simulink model "finalmodel1"  (R2024b)
(part 6 of 9)

Industries GmbH Sunmodule Plus SW 220 mono black | SolarWorld Industries GmbH Sunmodule Plus SW 220 poly | SolarWorld Industries GmbH Sunmodule Plus SW 225 mono | SolarWorld Industries GmbH Sunmodule Plus SW 225 mono black | SolarWorld Industries GmbH Sunmodule Plus SW 225 poly | SolarWorld Industries GmbH Sunmodule Plus SW 230 mono | SolarWorld Industries GmbH Sunmodule Plus SW 230 mono black | SolarWorld Industries GmbH Sunmodule Plus SW 230 poly | SolarWorld Industries GmbH Sunmodule Plus SW 235 mono | SolarWorld Industries GmbH Sunmodule Plus SW 235 mono black | SolarWorld Industries GmbH Sunmodule Plus SW 235 poly | SolarWorld Industries GmbH Sunmodule Plus SW 240 mono | SolarWorld Industries GmbH Sunmodule Plus SW 240 mono black | SolarWorld Industries GmbH Sunmodule Plus SW 240 poly | SolarWorld Industries GmbH Sunmodule Plus SW 245 mono | SolarWorld Industries GmbH Sunmodule Plus SW 245 mono black | SolarWorld Industries GmbH Sunmodule Plus SW 245 poly | SolarWorld Industries GmbH Sunmodule Plus SW 250 mono | SolarWorld Industries GmbH Sunmodule Plus SW 250 mono black | SolarWorld Industries GmbH Sunmodule Plus SW 250 poly | SolarWorld Industries GmbH Sunmodule Plus SW 255 mono | SolarWorld Industries GmbH Sunmodule Plus SW 255 mono black | SolarWorld Industries GmbH Sunmodule Plus SW 255 poly | SolarWorld Industries GmbH Sunmodule Protect SW 255 mono | SolarWorld Industries GmbH Sunmodule Protect SW 255 mono black | SolarWorld Industries GmbH Sunmodule Bisun SW 260 duo | SolarWorld Industries GmbH Sunmodule Plus SW 260 mono | SolarWorld Industries GmbH Sunmodule Plus SW 260 mono black | SolarWorld Industries GmbH Sunmodule Plus SW 260 poly | SolarWorld Industries GmbH Sunmodule Protect SW 260 mono | SolarWorld Industries GmbH Sunmodule Protect SW 260 mono black | SolarWorld Industries GmbH Sunmodule Bisun SW 265 duo | SolarWorld Industries GmbH Sunmodule Bisun SW 265 duo black | SolarWorld Industries GmbH Sunmodule Plus SW 265 mono | SolarWorld Industries GmbH Sunmodule Plus SW 265 mono black | SolarWorld Industries GmbH Sunmodule Plus SW 265 poly | SolarWorld Industries GmbH Sunmodule Protect SW 265 mono | SolarWorld Industries GmbH sunmodule Protect SW 265 mono black | SolarWorld Industries GmbH Sunmodule Plus SW 270 mono | SolarWorld Industries GmbH Sunmodule Protect SW 270 mono black | SolarWorld Industries GmbH Sunmodule Plus SW 275 mono | SolarWorld Industries GmbH Sunmodule Protect SW 275 mono | SolarWorld Industries GmbH Sunmodule Protect SW 275 mono black | SolarWorld Industries GmbH Sunmodule Protect SW 285 mono | SolarWorld Industries GmbH Sunmodule SW 305 XL mono | SolarWorld Industries GmbH Sunmodule SW 310 XL mono | SolarWorld Industries GmbH Sunmodule SW 315 XL mono | Solarzentrum Allgau Wiosun A-170P | Solarzentrum Allgau Wiosun PVT 170 | Solarzentrum Allgau Wiosun A-175P | Solarzentrum Allgau Wiosun PVT 175 | Solarzentrum Allgau Wiosun A-180P | Solarzentrum Allgau Wiosun PVT 180 | Solarzentrum Allgau Wiosun A-185P | Solarzentrum Allgau Wiosun PVT 185 | Solarzentrum Allgau Wiosun A-190P | Solarzentrum Allgau Wiosun PVT 190 | Soleeva Energy S1AC-7M330 | Soleeva Energy S1AC-7M335 | Soleeva Energy S1AC-7M340 | Soleeva Energy S1AC-7M345 | Solon Solon Blue 220/01 215 | Solon Solon Blue 220 | Solon Solon Blue 220/01 220 | Solon Solon Black 225 | Solon Solon Black 230/01 225 | Solon Solon Black 230/15 225 | Solon Solon Blue 220/01 225 | Solon Solon Blue 225 | Solon Solon Corvus 225 | Solon Solon Black 230 | Solon Solon Black 230/01 230 | Solon Solon Black 230/15 230 | Solon Solon Blue 220/01 230 | Solon Solon Blue 230 | Solon Solon Corvus 230 | Solon Solon Black 230/01 235 | Solon Solon Black 230/15 235 | Solon Solon Black 235 | Solon Solon Blue 220/01 235 | Solon Solon Blue 235 | Solon Solon Corvus 235 | Solon Solon Black 230/01 240 | Solon Solon Black 230/15 240 | Solon Solon Black 240 | Solon Solon Blue 220/01 240 | Solon Solon Blue 240 | Solon Solon Corvus 240 | Solon Solon Black 245 | Solon Solon Blue 270/09 250 | Solon Solon Blue 270/09 255 | Solon Solon Blue 270/09 260 | Solon Solon Black 280/09 265 | Solon Solon Blue 270/09 265 | Solon Solon Blue XT 265 | Solon Solon Black 280/09 270 | Solon Solon Blue 270/09 270 | Solon Solon Blue XT 270 | Solon Solon Black 280/09 275 | Solon Solon Black XT 275 | Solon Solon Blue 270/09 275 | Solon Solon Blue XT 275 | Solon Solon Black 280/09 280 | Solon Solon Black XT 280 | Solon Solon Blue 270/09 280 | Solon Solon Blue XT 280 | Solon SOLquick Black XT 280 | Solon SOLquick Blue XT 280 | Solon SOLquick Blue XT-H 280 | Solon Solon Black 280/09 285 | Solon Solon Black XT 285 | Solon Solon Blue 270/09 285 | Solon Solon Blue XT 285 | Solon SOLquick Black XT 285 | Solon SOLquick Blue XT 285 | Solon Solon Black 280/09 290 | Solon Solon Black XT 290 | Solon Solon Blue 270/09 290 | Solon SOLquick Black XT 290 | Solon Solon Black 280/09 295 | Solon Solon Black XT 295 | Solon SOLquick Black XT 295 | Solon Solon Black 280/09 300 | Solon SOLquick Black XT 300 | Soltecture Linion 85 F | Soltecture Linion 85 L | Soltecture Linion 85 R | Soltecture Linion 90 F | Soltecture Linion 90 L | Soltecture Linion 95 F | Soltecture Linion 95 L | Soltecture Linion 100 F | Soltecture Linion 100 L | SOLTON Power SPI-175M | SOLTON Power SPI-180M | SOLTON Power SPI-185M | SOLTON Power SPI-215P | SOLTON Power SPI-220P | SOLTON Power SPI-225M | SOLTON Power SPI-225P | SOLTON Power SPI-230M | SOLTON Power SPI-230P | SOLTON Power SPI-60-235M | SOLTON Power SPI-60-235P | SOLTON Power SPI-60-240M | SOLTON Power SPI-60-240P | SOLTON Power SPI-60-245M | SOLTON Power SPI-60-245P | SOLTON Power SPI-60-250M | SOLTON Power SPI-60-250P | SOLTON Power SPI-260M | SOLTON Power SPI-260P | SOLTON Power SPI-265M | SOLTON Power SPI-270M | SOLTON Power SPI-270P | SOLTON Power SPI-275M | SOLTON Power SPI-280M | SOLTON Power SPI-280P | SOLTON Power SPI-285M | SOLTON Power SPI-285P | SOLTON Power SPI-290M | SOLTON Power SPI-290P | SOLTON Power SPI-295M | SOLTON Power SPI-295P | SOLTON Power SPI-300M | SOLTON Power SPI-300P | Solvation Manufacturing P6Y-230 | Solvation Manufacturing P6Y-235 | Solvation Manufacturing P6Y-240 | Solvation Manufacturing SM240-5M | Solvation Manufacturing SM240M-B | Solvation Manufacturing P6Y-245 | Solvation Manufacturing SM245-5M | Solvation Manufacturing SM245M-B | Solvation Manufacturing SM245M-Bv | Solvation Manufacturing SM245S-B | Solvation Manufacturing M9X-250 | Solvation Manufacturing P6Y-250 | Solvation Manufacturing SM250-5M | Solvation Manufacturing SM250M-B | Solvation Manufacturing SM250M-Bv | Solvation Manufacturing SM250S-B | Solvation Manufacturing M9X-255 | Solvation Manufacturing SM255-5M | Solvation Manufacturing SM255M-B | Solvation Manufacturing SM255M-Bv | Solvation Manufacturing SM255S-B | Solvation Manufacturing M9X-260 | Solvation Manufacturing SM260-5M | Solvation Manufacturing SM260M-Bv | Solvation Manufacturing M9X-265 | Solvation Manufacturing SM265M-Bv | Solvation Manufacturing P7Y-270 | Solvation Manufacturing SM270M-A | Solvation Manufacturing P7Y-275 | Solvation Manufacturing SM275M-A | Solvation Manufacturing P7Y-280 | Solvation Manufacturing SM280M-A | Solvation Manufacturing P7Y-285 | Solvation Manufacturing SM285M-A | Solvation Manufacturing SM285M-Av | Solvation Manufacturing P7Y-290 | Solvation Manufacturing SM290M-A | Solvation Manufacturing SM290M-Av | Solvation Manufacturing SM295M-A | Solvation Manufacturing SM295M-Av | Solvation Manufacturing SM300M-A | Solvation Manufacturing SM300M-Av | Solvation Manufacturing SM305M-A | Solvation Manufacturing SM305M-Av | Solvation Manufacturing SM310M-Av | Solvation Manufacturing SM315M-Av | Sonali Energees SS 270 | Sonali Energees SS 280 | Sonali Energees SS 290 | Sonali Energees SS 300 | Sonali Energees SS 310 | Sonali Energees SS 315 | Sonali Energees SS 320 | Sonali Energees USA SS 1200 P | Sonali Energees USA SS 1250 P | Sonali Energees USA SS 1300 P | Sonali Energees USA SS 1400 P | Sonali Energees USA SS1750-170W | Sonali Energees USA SS 1750 P | Sonali Energees USA SS1750-175W | Sonali Energees USA SS 1800 P | Sonali Energees USA SS1750-180W | Sonali Energees USA SS 1900 P | Sonali Energees USA SS 2000 P | Sonali Energees USA SS 2100 P | Sonali Energees USA SS2100-210W | Sonali Energees USA SS2100-215W | Sonali Energees USA SS 2200 P | Sonali Energees USA SS2100-220W | Sonali Energees USA SS 2300 P | Sonali Energees USA SS2300-230W | Sonali Energees USA SS2300-235W | Sonali Energees USA SS 2400 P | Sonali Energees USA SS2300-240W | Sonali Energees USA SS2500-250W | Sonali Energees USA SS2800-275W | Sonali Energees USA SS2800-280W | Sonali Energees USA SS2800-285W | Sonnetek SNK-165PSD | Sonnetek SNK-170PSD | Sonnetek SNK-175PSD | Sonnetek SNK-180PSD | Sonnetek SNK-250PSP | Sonnetek SNK-260PSP | Sonnetek SNK-270PSP | Sopray Energy SR-150 | Sopray Energy SR-160 | Sopray Energy SR-165 | Sopray Energy SR-170 | Sopray Energy SR-175 | Sopray Energy SR-180 | Sopray Energy SR156P-200 | Sopray Energy SR156P-210 | Sopray Energy SR156P-220 | Sopray Energy SR156P-230 | Sova Power SOLARSOVA 200P | Sova Power SOLARSOVA 205P | Sova Power SOLARSOVA 210P | Sova Power SOLARSOVA 215P | Sova Power SOLARSOVA 220P | Sova Power SOLARSOVA 235P | Sova Power SOLARSOVA 240P | Sova Power SOLARSOVA 245P | Sova Power SOLARSOVA 250P | Sova Power SOLARSOVA 255P | Sova Power SOLARSOVA 260P | Sovello SV-T-190-yyy | Sovello SV-X-190-yyy | Sovello SV-T-195-yyy | Sovello SV-X-195-yyy | Sovello SV-T-200-yyy | Sovello SV-X-200-yyy | Sovello SV-X-205-yyy | Sovello SV-X-210-yyy | SRS Energy SPT16 | Star Harvest Solar SHS260-5M | Stion SN-110 | Stion STN-110 | Stion SN-115 | Stion STN-115 | Stion SN-120 | Stion STL-120A | Stion STN-120 | Stion STO-120A | Stion SN-125 | Stion STL-125 | Stion STL-125A | Stion STN-125 | Stion STO-125 | Stion STO-125A | Stion SN-130 | Stion STL-130 | Stion STL-130A | Stion STN-130 | Stion STO-130 | Stion STO-130A | Stion SN-135 | Stion STL-135 | Stion STL-135A | Stion STN-135 | Stion STO-135 | Stion STO-135A | Stion SN-140 | Stion STL-140 | Stion STL-140A | Stion STN-140 | Stion STO-140 | Stion STO-140A | Stion SN-145 | Stion STL-145 | Stion STL-145A | Stion STN-145 | Stion STO-145 | Stion STO-145A | Stion SN-150 | Stion STL-150 | Stion STL-150A | Stion STN-150 | Stion STO-150 | Stion STO-150A | Stion STL-155A | Stion STO-155A | Stion STL-160A | Stion STO-160A | STX Solar STX-240MT2 | STX Solar STX-245MT2 | STX Solar STX-250MT2 | STX Solar STX-255MT2 | STX Solar STX-260MT2 | STX Solar STX-290MT2 | STX Solar STX-295MT2 | STX Solar STX-300MT2 | STX Solar STX-305MT2 | Sun Earth Solar Power TDB125x125-36-P 80W | Sun Earth Solar Power TDB125x125-36-P 85W | Sun Earth Solar Power TPB125x125-36-P 85W | Sun Earth Solar Power TDB125x125-36-P 90W | Sun Earth Solar Power TPB125x125-36-P 90W | Sun Earth Solar Power TDB125x125-36-P 95W | Sun Earth Solar Power TPB125x125-36-P 95W | Sun Earth Solar Power TDB156x156-36-P 125W | Sun Earth Solar Power TPB156x156-36-P 125W | Sun Earth Solar Power TDB156x156-36-P 130W | Sun Earth Solar Power TPB156x156-36-P 130W | Sun Earth Solar Power TDB156x156-36-P 135W | Sun Earth Solar Power TPB156x156-36-P 135W | Sun Earth Solar Power TDB156x156-36-P 140W | Sun Earth Solar Power TPB156x156-36-P 140W | Sun Earth Solar Power TDB156x156-36-P 145W | Sun Earth Solar Power TPB156x156-36-P 145W | Sun Earth Solar Power TDB125x125-72-P 150W | Sun Earth Solar Power TPB125x125-72-P 150W | Sun Earth Solar Power TDB125x125-72-P 155W | Sun Earth Solar Power TPB125x125-72-P 155W | Sun Earth Solar Power TDB125x125-72-P 160W | Sun Earth Solar Power TPB125x125-72-P 160W | Sun Earth Solar Power TDB125x125-72-P 165W | Sun Earth Solar Power TPB125x125-72-P 165W | Sun Earth Solar Power TDB125x125-72-P 170W | Sun Earth Solar Power TPB125x125-72-P 170W | Sun Earth Solar Power TDB125x125-72-P 175W | Sun Earth Solar Power TPB125x125-72-P 175W | Sun Earth Solar Power TDB125x125-72-P 180W | Sun Earth Solar Power TPB125x125-72-P 180W | Sun Earth Solar Power TPB156x156-54-P 180W | Sun Earth Solar Power TDB125x125-72-P 185W | Sun Earth Solar Power TPB125x125-72-P 185W | Sun Earth Solar Power TPB156x156-54-P 185W | Sun Earth Solar Power TDB125x125-72-P 190W | Sun Earth Solar Power TPB125x125-72-P 190W | Sun Earth Solar Power TPB156x156-54-P 190W | Sun Earth Solar Power TPB156x156-54-P 195W | Sun Earth Solar Power TPB125x125-96-P 200W | Sun Earth Solar Power TPB156x156-54-P 200W | Sun Earth Solar Power TPB156x156-60-P 200W | Sun Earth Solar Power TPB156x156-54-P 205W | Sun Earth Solar Power TPB156x156-60-P 205W | Sun Earth Solar Power TPB125x125-96-P 210W | Sun Earth Solar Power TPB156x156-54-P 210W | Sun Earth Solar Power TPB156x156-60-P 210W | Sun Earth Solar Power TDB156x156-60-P 215W | Sun Earth Solar Power TPB156x156-54-P 215W | Sun Earth Solar Power TPB156x156-60-P 215W | Sun Earth Solar Power TDB156x156-60-P 220W | Sun Earth Solar Power TPB125x125-96-P 220W | Sun Earth Solar Power TPB156x156-54-P 220W | Sun Earth Solar Power TPB156x156-60-P 220W | Sun Earth Solar Power TDB156x156-60-P 225W | Sun Earth Solar Power TPB156x156-60-P 225W | Sun Earth Solar Power TDB156x156-60-P 230W | Sun Earth Solar Power TPB125x125-96-P 230W | Sun Earth Solar Power TPB156x156-60-P 230W | Sun Earth Solar Power TPB156x156-72-P 230W | Sun Earth Solar Power TDB156x156-60-P 235W | Sun Earth Solar Power TPB156x156-60-P 235W | Sun Earth Solar Power TDB156x156-60-P 240W | Sun Earth Solar Power TPB125x125-96-P 240W | Sun Earth Solar Power TPB156x156-60-P 240W | Sun Earth Solar Power TPB156x156-72-P 240W | Sun Earth Solar Power TDB156x156-60-P 245W | Sun Earth Solar Power TPB156x156-60-P 245W | Sun Earth Solar Power TPB156x156-72-P 250W | Sun Earth Solar Power TPB156x156-72-P 255W | Sun Earth Solar Power TPB156x156-72-P 260W | Sun Earth Solar Power TPB156x156-72-P 270W | Sun Earth Solar Power TDB156x156-72-P 280W | Sun Earth Solar Power TPB156x156-72-P 280W | Sun Earth Solar Power TDB156x156-72-P 285W | Sun Earth Solar Power TPB156x156-72-P 285W | Sun Earth Solar Power TDB156x156-72-P 290W | Sun Earth Solar Power TPB156x156-72-P 290W | Sun Earth Solar Power TDB156x156-72-P 295W | Sun Earth Solar Power TPB156x156-72-P 295W | Sun Energy Engineering SE14-50 | Sun Energy Engineering SE14-52 | SUN M ENERGY SDN BHD ES200PCFW | SUN M ENERGY SDN BHD SME-P648200 | SUN M ENERGY SDN BHD SME-P648200B | SUN M ENERGY SDN BHD ES205PCFW | SUN M ENERGY SDN BHD SME-P648205 | SUN M ENERGY SDN BHD SME-P648205B | SUN M ENERGY SDN BHD ES210PCFW | SUN M ENERGY SDN BHD SME-P648210 | SUN M ENERGY SDN BHD SME-P648210B | SUN M ENERGY SDN BHD ES215PCFW | SUN M ENERGY SDN BHD SME-P648215 | SUN M ENERGY SDN BHD SME-P648215B | SUN M ENERGY SDN BHD ES250PAFW | SUN M ENERGY SDN BHD SME-P660250 | SUN M ENERGY SDN BHD SME-P660250B | SUN M ENERGY SDN BHD ES255PAFW | SUN M ENERGY SDN BHD SME-P660255 | SUN M ENERGY SDN BHD SME-P660255B | SUN M ENERGY SDN BHD ES260PAFW | SUN M ENERGY SDN BHD SME-P660260 | SUN M ENERGY SDN BHD SME-P660260B | SUN M ENERGY SDN BHD ES265PAFW | SUN M ENERGY SDN BHD SME-P660265 | SUN M ENERGY SDN BHD SME-P660265B | SUN M ENERGY SDN BHD ES300PBFW | SUN M ENERGY SDN BHD SME-P672300 | SUN M ENERGY SDN BHD SME-P672300B | SUN M ENERGY SDN BHD ES305PBFW | SUN M ENERGY SDN BHD SME-P672305 | SUN M ENERGY SDN BHD SME-P672305B | SUN M ENERGY SDN BHD ES310PBFW | SUN M ENERGY SDN BHD SME-P672310 | SUN M ENERGY SDN BHD SME-P672310B | SUN M ENERGY SDN BHD ES315PBFW | SUN M ENERGY SDN BHD SME-P672315 | SUN M ENERGY SDN BHD SME-P672315B | SUN M ENERGY SDN BHD ES320PBFW | SUN M ENERGY SDN BHD SME-P672320 | SUN M ENERGY SDN BHD SME-P672320B | Sun Well Solar WD-A-CC-087A | Sun Well Solar WD-A-CC-087B | Sun Well Solar WD-A-CC-087C | Sun World Solar Energy Technology (Luoyang) SWM230P156 | Sun World Solar Energy Technology (Luoyang) SWM235M156 | Sun World Solar Energy Technology (Luoyang) SWM235P156 | Sun World Solar Energy Technology (Luoyang) SWM240M156 | Sun World Solar Energy Technology (Luoyang) SWM240P156 | Sun World Solar Energy Technology (Luoyang) SWM245M156 | Sun World Solar Energy Technology (Luoyang) SWM245P156 | Sun World Solar Energy Technology (Luoyang) SWM250M156 | Sun World Solar Energy Technology (Luoyang) SWM250P156 | Sun World Solar Energy Technology (Luoyang) SWM255M156 | Sun World Solar Energy Technology (Luoyang) SWM280P156 | Sun World Solar Energy Technology (Luoyang) SWM285M156 | Sun World Solar Energy Technology (Luoyang) SWM285P156 | Sun World Solar Energy Technology (Luoyang) SWM290M156 | Sun World Solar Energy Technology (Luoyang) SWM290P156 | Sun World Solar Energy Technology (Luoyang) SWM295M156 | Sun World Solar Energy Technology (Luoyang) SWM295P156 | Sun World Solar Energy Technology (Luoyang) SWM300M156 | Sun World Solar Energy Technology (Luoyang) SWM300P156 | Sunarray SUNARRAY-M6B2409-130 | Sunarray SUNARRAY-M6B2409-135 | Sunarray SUNARRAY-S6B2409-135 | Sunarray SUNARRAY-M6B2409-140 | Sunarray SUNARRAY-S6B2409-140 | Sunarray SUNARRAY-S6B2409-145 | Sunarray SUNARRAY-M6B2608-175 | Sunarray SUNARRAY-M6B2608-180 | Sunarray SUNARRAY-S6B2608-180 | Sunarray SUNARRAY-M6B2608-185 | Sunarray SUNARRAY-S6B2608-185 | Sunarray SUNARRAY-M6B2609-190 | Sunarray SUNARRAY-S6B2608-190 | Sunarray SUNARRAY-M6B2609-195 | Sunarray SUNARRAY-S6B2609-195 | Sunarray SUNARRAY-M6B2609-200 | Sunarray SUNARRAY-S6B2609-200 | Sunarray SUNARRAY-M6B2609-205 | Sunarray SUNARRAY-S6B2609-205 | Sunarray SUNARRAY-M6B2609-210 | Sunarray SUNARRAY-S6B2609-210 | Sunarray SUNARRAY-M6B2609-215 | Sunarray SUNARRAY-S6B2609-215 | Sunarray SUNARRAY-M6B2609-220 | Sunarray SUNARRAY-S6B2609-220 | Sunarray SUNARRAY-M6B2609-225 | Sunarray SUNARRAY-S6B2609-225 | Sunarray SUNARRAY-M6B2609-230 | Sunarray SUNARRAY-S6B2609-230 | Sunarray SUNARRAY-M6B2610-235 | Sunarray SUNARRAY-S6B2609-235 | Sunarray SUNARRAY-M6B2610-240 | Sunarray SUNARRAY-S6B2609-240 | Sunarray SUNARRAY-M6B3612-270T | Sunarray SUNARRAY-M6B2612-275 | Sunarray SUNARRAY-M6B3612-275T | Sunarray SUNARRAY-M6B2612-280 | Sunarray SUNARRAY-M6B3612-280T | Sunarray SUNARRAY-M6B2612-285 | Sunarray SUNARRAY-M6B3612-285T | Sunarray SUNARRAY-S6B3612-285T | Sunarray SUNARRAY-M6B2612-290 | Sunarray SUNARRAY-M6B3612-290T | Sunarray SUNARRAY-S6B3612-290T | Sunarray SUNARRAY-M6B2612-295 | Sunarray SUNARRAY-S6B3612-295T | Sunarray SUNARRAY-S6B3612-300T | Sunarray SUNARRAY-S6B3612-305T | SunEdison SE-F245KzC-2y | SunEdison SE-F250KzC-2y | SunEdison MEMC-F255KzC-2y | SunEdison SE-F255CzC-3y | SunEdison SE-F255CzC-4y | SunEdison SE-F255CzD-3y | SunEdison SE-F255CzD-4y | SunEdison SE-F255FzC-3y | SunEdison SE-F255FzC-4y | SunEdison SE-F255FzD-3y | SunEdison SE-F255FzD-4y | SunEdison SE-F255GzC-3y | SunEdison SE-F255GzC-4y | SunEdison SE-F255GzD-3y | SunEdison SE-F255GzD-4y | SunEdison SE-F255KzC-2y | SunEdison SE-F255KzC-3y | SunEdison SE-F255KzC-4y | SunEdison SE-F255KzD-3y | SunEdison SE-F255KzD-4y | SunEdison MEMC-F260KzC-2y | SunEdison SE-F260CzC-3y | SunEdison SE-F260CzC-4y | SunEdison SE-F260CzD-3y | SunEdison SE-F260CzD-4y | SunEdison SE-F260FzC-3y | SunEdison SE-F260FzC-4y | SunEdison SE-F260FzD-3y | SunEdison SE-F260FzD-4y | SunEdison SE-F260GzC-3y | SunEdison SE-F260GzC-4y | SunEdison SE-F260GzD-3y | SunEdison SE-F260GzD-4y | SunEdison SE-F260KzC-2y | SunEdison SE-F260KzC-3y | SunEdison SE-F260KzC-4y | SunEdison SE-F260KzD-3y | SunEdison SE-F260KzD-4y | SunEdison MEMC-F265KzC-2y | SunEdison SE-F265CzC-3y | SunEdison SE-F265CzC-4y | SunEdison SE-F265CzD-3y | SunEdison SE-F265CzD-4y | SunEdison SE-F265FzC-3y | SunEdison SE-F265FzC-4y | SunEdison SE-F265FzD-3y | SunEdison SE-F265FzD-4y | SunEdison SE-F265GzC-3y | SunEdison SE-F265GzC-4y | SunEdison SE-F265GzD-3y | SunEdison SE-F265GzD-4y | SunEdison SE-F265KzC-2y | SunEdison SE-F265KzC-3y | SunEdison SE-F265KzC-4y | SunEdison SE-F265KzD-3y | SunEdison SE-F265KzD-4y | SunEdison SE-R265GzC-3y | SunEdison SE-R265GzC-4y | SunEdison MEMC-F270KzC-2y | SunEdison SE-F270CzC-3y | SunEdison SE-F270CzC-4y | SunEdison SE-F270CzD-3y | SunEdison SE-F270CzD-4y | SunEdison SE-F270FzC-3y | SunEdison SE-F270FzC-4y | SunEdison SE-F270FzD-3y | SunEdison SE-F270FzD-4y | SunEdison SE-F270GzC-4y | SunEdison SE-F270GzD-3y | SunEdison SE-F270GzD-4y | SunEdison SE-F270KzC-2y | SunEdison SE-F270KzC-3y | SunEdison SE-F270KzC-4y | SunEdison SE-F270KzD-3y | SunEdison SE-F270KzD-4y | SunEdison SE-H270EzC-3y | SunEdison SE-R270CzC-3y | SunEdison SE-R270GzC-3y | SunEdison SE-R270GzC-4y | SunEdison SE-R270KzC-3y | SunEdison SE-F275CzC-3y | SunEdison SE-F275CzC-4y | SunEdison SE-F275CzD-3y | SunEdison SE-F275CzD-4y | SunEdison SE-F275FzC-3y | SunEdison SE-F275FzC-4y | SunEdison SE-F275FzD-3y | SunEdison SE-F275FzD-4y | SunEdison SE-F275GzC-4y | SunEdison SE-F275GzD-3y | SunEdison SE-F275GzD-4y | SunEdison SE-F275KzC-4y | SunEdison SE-F275KzD-3y | SunEdison SE-F275KzD-4y | SunEdison SE-H275EzC-3y | SunEdison SE-R275CzC-3y | SunEdison SE-R275FzC-3y | SunEdison SE-R275FzC-4y | SunEdison SE-R275GzC-3y | SunEdison SE-R275GzC-4y | SunEdison SE-R275KzC-3y | SunEdison SE-F280CzC-3y | SunEdison SE-F280CzC-4y | SunEdison SE-F280CzD-3y | SunEdison SE-F280CzD-4y | SunEdison SE-F280FzC-4y | SunEdison SE-F280FzD-3y | SunEdison SE-F280FzD-4y | SunEdison SE-F280GzC-4y | SunEdison SE-F280GzD-3y | SunEdison SE-F280GzD-4y | SunEdison SE-F280KzC-4y | SunEdison SE-F280KzD-3y | SunEdison SE-F280KzD-4y | SunEdison SE-H280EzC-3y | SunEdison SE-R280CzC-3y | SunEdison SE-R280FzC-3y | SunEdison SE-R280FzC-4y | SunEdison SE-R280GzC-3y | SunEdison SE-R280GzC-4y | SunEdison SE-R280KzC-3y | SunEdison SE-H285EzC-3y | SunEdison SE-R285CzC-3y | SunEdison SE-R285FzC-3y | SunEdison SE-R285FzC-4y | SunEdison SE-R285GzC-3y | SunEdison SE-R285GzC-4y | SunEdison SE-H290EzC-3y | SunEdison SE-R290CzC-3y | SunEdison SE-R290FzC-3y | SunEdison SE-R290FzC-4y | SunEdison SE-R295FzC-3y | SunEdison SE-R295FzC-4y | SunEdison SE-F305BzC-4y | SunEdison SE-F305BzD-3y | SunEdison SE-F305BzD-4y | SunEdison SE-F305EzC-3y | SunEdison SE-F305EzC-4y | SunEdison SE-F305EzD-3y | SunEdison SE-F305EzD-4y | SunEdison SE-Z305-4 | SunEdison SE-F310BzC-3y | SunEdison SE-F310BzC-4y | SunEdison SE-F310BzD-3y | SunEdison SE-F310BzD-4y | SunEdison SE-F310EzC-3y | SunEdison SE-F310EzC-4y | SunEdison SE-F310EzD-3y | SunEdison SE-F310EzD-4y | SunEdison SE-Z310-4 | SunEdison SE-D315BzC-3y | SunEdison SE-F315BzC-3y | SunEdison SE-F315BzC-4y | SunEdison SE-F315BzD-3y | SunEdison SE-F315BzD-4y | SunEdison SE-F315EzC-3y | SunEdison SE-F315EzC-4y | SunEdison SE-F315EzD-3y | SunEdison SE-F315EzD-4y | SunEdison SE-Z315-4 | SunEdison SE-D320BzC-3y | SunEdison SE-F320BzC-3y | SunEdison SE-F320BzC-4y | SunEdison SE-F320BzD-3y | SunEdison SE-F320BzD-4y | SunEdison SE-F320EzC-3y | SunEdison SE-F320EzC-4y | SunEdison SE-F320EzD-3y | SunEdison SE-F320EzD-4y | SunEdison SE-Z320-4 | SunEdison SE-D325BzC-3y | SunEdison SE-F325BzC-3y | SunEdison SE-F325BzC-4y | SunEdison SE-F325BzD-3y | SunEdison SE-F325BzD-4y | SunEdison SE-F325EzC-3y | SunEdison SE-F325EzC-4y | SunEdison SE-F325EzD-3y | SunEdison SE-F325EzD-4y | SunEdison SE-R325BzC-3y | SunEdison SE-Z325-4 | SunEdison SE-D330BzC-3y | SunEdison SE-F330BzC-3y | SunEdison SE-F330BzC-4y | SunEdison SE-F330BzD-3y | SunEdison SE-F330BzD-4y | SunEdison SE-F330EzC-3y | SunEdison SE-F330EzC-4y | SunEdison SE-F330EzD-3y | SunEdison SE-F330EzD-4y | SunEdison SE-H330EzC-3y | SunEdison SE-R330BzC-3y | SunEdison SE-R330BzC-4y | SunEdison SE-R330EzC-3y | SunEdison SE-R330EzC-4y | SunEdison SE-Z330-4 | SunEdison SE-D335BzC-3y | SunEdison SE-F335BzC-3y | SunEdison SE-F335BzC-4y | SunEdison SE-F335BzD-3y | SunEdison SE-F335BzD-4y | SunEdison SE-F335EzC-3y | SunEdison SE-F335EzC-4y | SunEdison SE-F335EzD-3y | SunEdison SE-F335EzD-4y | SunEdison SE-H335-4 | SunEdison SE-H335EzC-3y | SunEdison SE-R335BzC-3y | SunEdison SE-R335BzC-4y | SunEdison SE-R335EzC-3y | SunEdison SE-R335EzC-4y | SunEdison SE-H340-4 | SunEdison SE-H340EzC-3y | SunEdison SE-R340BzC-3y | SunEdison SE-R340BzC-4y | SunEdison SE-R340EzC-3y | SunEdison SE-R340EzC-4y | SunEdison SE-H345-4 | SunEdison SE-H345EzC-3y | SunEdison SE-R345BzC-3y | SunEdison SE-R345BzC-4y | SunEdison SE-R345EzC-3y | SunEdison SE-R345EzC-4y | SunEdison SE-H350-4 | SunEdison SE-H350EzC-3y | SunEdison SE-R350BzC-3y | SunEdison SE-R350BzC-4y | SunEdison SE-R350EzC-3y | SunEdison SE-R350EzC-4y | SunEdison SE-H355-4 | SunEdison SE-H355EzC-3y | SunEdison SE-R355BzC-4y | SunEdison SE-R355EzC-3y | SunEdison SE-R355EzC-4y | SunEdison SE-H360-4 | SunEdison SE-R360BzC-4y | SunEdison SE-R360EzC-3y | SunEdison SE-R360EzC-4y | SunEdison SE-H365-4 | SunEdison SE-Z370-4 | SunEdison SE-Z375-4 | SunEdison SE-Z380-4 | SunEdison SE-Z385-4 | SunEdison SE-Z390-4 | SunEdison SE-Z395-4 | SUNGEN International SG-HN90-GG | SUNGEN International SG-HN95-GG | SUNGEN International SG-HN100-GG | SUNGEN International SG-HN105-GG | SUNGEN International SG-HN110-GG | SUNGEN International SGM-165D | SUNGEN International SGM-170D | SUNGEN International SGM-175D | SUNGEN International SGM-180D | SUNGEN International SGM-185D | SUNGEN International SGM-190D | SUNGEN International SGM-195D | SUNGEN International SGM-200D | SUNGEN International SGM-200P | SUNGEN International SGM-205D | SUNGEN International SGM-205P | SUNGEN International SGM-210D | SUNGEN International SGM-210P | SUNGEN International SGM-215D | SUNGEN International SGM-215P | SUNGEN International SGM-220D | SUNGEN International SGM-220P | SUNGEN International SGM-225D | SUNGEN International SGM-225P | SUNGEN International SGM-230D | SUNGEN International SGM-230P | SUNGEN International SGM-235D | SUNGEN International SGM-235P | SUNGEN International SGM-240D | SUNGEN International SGM-240P | SUNGEN International SGM-245D | SUNGEN International SGM-245P | SUNGEN International SGM-250D | SUNGEN International SGM-250P | SUNGEN International SGM-255D | SUNGEN International SGM-255P | SUNGEN International SGM-260D | SUNGEN International SGM-260P | SUNGEN International SGM-265P | SUNGEN International SGM-270P | SUNGEN International SGM-275P | SUNGEN International SGM-280P | SUNGEN International SGM-285P | Suniva ART230-60-3-100 | Suniva ART235-60-3-100 | Suniva ART235-60-3-101 | Suniva ART235-60-3-1B0 | Suniva MVP235-60-5-401 | Suniva MVT235-60-5-100 | Suniva MVX235-60-5-100 | Suniva MVX235-60-5-701 | Suniva OPT235-60-4-100 | Suniva OPT235-60-4-1B0 | Suniva ART240-60-3-100 | Suniva ART240-60-3-101 | Suniva ART240-60-3-1B0 | Suniva MVT240-60-5-100 | Suniva MVX240-60-5-100 | Suniva MVX240-60-5-701 | Suniva MVX240-60-5-7B1 | Suniva MVX240-60-5-801 | Suniva MVX240-60-5-8B1 | Suniva OPT240-60-4-100 | Suniva OPT240-60-4-1B0 | Suniva ART245-60-3-100 | Suniva ART245-60-3-101 | Suniva ART245-60-3-1B0 | Suniva MVT245-60-5-100 | Suniva MVX245-60-5-100 | Suniva MVX245-60-5-701 | Suniva MVX245-60-5-7B1 | Suniva MVX245-60-5-801 | Suniva MVX245-60-5-8B1 | Suniva OPT245-60-4-100 | Suniva OPT245-60-4-1B0 | Suniva ART250-60-3-100 | Suniva ART250-60-3-101 | Suniva ART250-60-3-1B0 | Suniva MVT250-60-5-100 | Suniva MVX250-60-5-100 | Suniva MVX250-60-5-701 | Suniva MVX250-60-5-7B1 | Suniva MVX250-60-5-801 | Suniva MVX250-60-5-8B1 | Suniva OPT250-60-4-100 | Suniva OPT250-60-4-1B0 | Suniva ART255-60-3-100 | Suniva ART255-60-3-1B0 | Suniva MVT255-60-5-100 | Suniva MVX255-60-5-100 | Suniva MVX255-60-5-701 | Suniva MVX255-60-5-7B1 | Suniva MVX255-60-5-801 | Suniva MVX255-60-5-8B1 | Suniva OPT255-60-4-100 | Suniva OPT255-60-4-1B0 | Suniva MVT260-60-5-100 | Suniva MVX260-60-5-100 | Suniva MVX260-60-5-701 | Suniva MVX260-60-5-7B1 | Suniva MVX260-60-5-800 | Suniva MVX260-60-5-801 | Suniva MVX260-60-5-8B1 | Suniva OPT260-60-4-100 | Suniva OPT260-60-4-1B0 | Suniva ART265-60-4-8B0 | Suniva MVT265-60-5-100 | Suniva MVX265-60-5-100 | Suniva MVX265-60-5-800 | Suniva OPT265-60-4-100 | Suniva OPT265-60-4-1B0 | Suniva ART270-60-4-8B0 | Suniva MVX270-60-5-800 | Suniva OPT270-60-4-100 | Suniva OPT270-60-4-1B0 | Suniva ART275-60-4-800 | Suniva ART275-60-4-8B0 | Suniva OPT275-60-4-100 | Suniva OPT275-60-4-1B0 | Suniva OPT275-60-4-800 | Suniva OPT275-60-4-8B0 | Suniva ART280-60-4-800 | Suniva ART280-60-4-8B0 | Suniva MVT280-72-5-100 | Suniva MVX280-72-5-100 | Suniva OPT280-60-4-100 | Suniva OPT280-60-4-1B0 | Suniva OPT280-60-4-800 | Suniva OPT280-60-4-8B0 | Suniva ART285-60-4-800 | Suniva ART285-60-4-8B0 | Suniva MVT285-72-5-100 | Suniva MVX285-72-5-100 | Suniva MVX285-72-5-701 | Suniva MVX285-72-5-801 | Suniva OPT285-60-4-100 | Suniva OPT285-60-4-1B0 | Suniva OPT285-60-4-800 | Suniva OPT285-60-4-8B0 | Suniva ART290-60-4-800 | Suniva ART290-60-4-8B0 | Suniva MVT290-72-5-100 | Suniva MVX290-72-5-100 | Suniva MVX290-72-5-701 | Suniva MVX290-72-5-801 | Suniva OPT290-60-4-100 | Suniva OPT290-60-4-1B0 | Suniva OPT290-60-4-800 | Suniva OPT290-60-4-8B0 | Suniva OPT290-72-4-100 | Suniva MVT295-72-5-100 | Suniva MVX295-72-5-100 | Suniva MVX295-72-5-701 | Suniva MVX295-72-5-801 | Suniva OPT295-60-4-100 | Suniva OPT295-60-4-1B0 | Suniva OPT295-72-4-100 | Suniva ART300-72-4-100 | Suniva MVT300-72-5-100 | Suniva MVX300-72-5-100 | Suniva MVX300-72-5-701 | Suniva MVX300-72-5-801 | Suniva OPT300-60-4-100 | Suniva OPT300-60-4-1B0 | Suniva OPT300-72-4-100 | Suniva ART305-72-4-100 | Suniva MVT305-72-5-100 | Suniva MVX305-72-5-100 | Suniva MVX305-72-5-701 | Suniva MVX305-72-5-801 | Suniva OPT305-72-4-100 | Suniva ART310-72-4-100 | Suniva MVT310-72-5-100 | Suniva MVX310-72-5-100 | Suniva MVX310-72-5-800 | Suniva MVX310-72-5-801 | Suniva OPT310-72-4-100 | Suniva ART315-72-4-100 | Suniva MVX315-72-5-800 | Suniva OPT315-72-4-100 | Suniva ART320-72-4-100 | Suniva MVX320-72-5-800 | Suniva OPT320-72-4-100 | Suniva ART325-72-4-100 | Suniva MVX325-72-5-800 | Suniva OPT325-72-4-100 | Suniva ART330-72-4-100 | Suniva MVX330-72-5-800 | Suniva OPT330-72-4-100 | Suniva ART335-72-4-100 | Suniva OPT335-72-4-100 | Suniva ART340-72-4-100 | Suniva OPT340-72-4-100 | Sunlan Solar SLM225P | Sunlan Solar SLM230P | Sunlan Solar SLM235P | Sunlan Solar SLM245P | Sunlan Solar SLM270P | Sunlan Solar SLM275P | Sunlan Solar SLM280P | Sunny International Power SPM-180PB203 | Sunny International Power SPM-180SB105 | Sunny International Power SPM-190PB203 | Sunny International Power SPM-190SB105 | Sunny International Power SPM-200PB203 | Sunny International Power SPM-200PB204 | Sunny International Power SPM-200SB105 | Sunny International Power SPM-210PB203 | Sunny International Power SPM-210PB204 | Sunny International Power SPM-220PB204 | Sunny International Power SPM-230PB204 | Sunny International Power SPM-230PB206 | Sunny International Power SPM-240PB204 | Sunny International Power SPM-240PB205 | Sunny International Power SPM-240PB206 | Sunny International Power SPM-250PB205 | Sunny International Power SPM-250PB206 | Sunny International Power SPM-260PB205 | Sunny International Power SPM-260PB206 | Sunny International Power SPM-270PB205 | Sunny International Power SPM-270PB206 | Sunny International Power SPM-280PB205 | Sunny International Power SPM-290PB205 | Sunperfect Solar CRM60S125M-24 | Sunperfect Solar CRM60S125S | Sunperfect Solar CRM85S125M-36 | Sunperfect Solar CRM85S125S | Sunperfect Solar CRM115S125M-48 | Sunperfect Solar CRM115S125S | Sunperfect Solar CRM145S125M-60 | Sunperfect Solar CRM145S125S | Sunperfect Solar CRM175S125M-72 | Sunperfect Solar CRM175S125S | Sunperfect Solar CRM180S125M-72 | Sunperfect Solar CRM185S125M-72 | Sunperfect Solar CRM185S156P-54 | Sunperfect Solar CRM190S125M-72 | Sunperfect Solar CRM190S156P-54 | Sunperfect Solar CRM195S125M-72 | Sunperfect Solar CRM195S125M-80 | Sunperfect Solar CRM195S125S | Sunperfect Solar CRM195S156P-54 | Sunperfect Solar CRM200S156P-54 | Sunperfect Solar CRM200S156P-60 | Sunperfect Solar CRM205S125M-80 | Sunperfect Solar CRM205S156P-54 | Sunperfect Solar CRM205S156P-60 | Sunperfect Solar CRM210S125M-80 | Sunperfect Solar CRM210S156P-54 | Sunperfect Solar CRM210S156P-60 | Sunperfect Solar CRM215S125M-80 | Sunperfect Solar CRM215S156P-54 | Sunperfect Solar CRM215S156P-60 | Sunperfect Solar CRM220S156P-54 | Sunperfect Solar CRM220S156P-60 | Sunperfect Solar CRM225S156P-54 | Sunperfect Solar CRM225S156P-60 | Sunperfect Solar CRM230S156P-54 | Sunperfect Solar CRM230S156P-60 | Sunperfect Solar CRM235S125M-96 | Sunperfect Solar CRM235S125S | Sunperfect Solar CRM235S156P-60 | Sunperfect Solar CRM240S125M-96 | Sunperfect Solar CRM240S156P-60 | Sunperfect Solar CRM240S156P-72 | Sunperfect Solar CRM245S125M-96 | Sunperfect Solar CRM245S156P-60 | Sunperfect Solar CRM245S156P-72 | Sunperfect Solar CRM250S125M-96 | Sunperfect Solar CRM250S156P-60 | Sunperfect Solar CRM250S156P-72 | Sunperfect Solar CRM255S125M-96 | Sunperfect Solar CRM255S156P-60 | Sunperfect Solar CRM255S156P-72 | Sunperfect Solar CRM260S125M-96 | Sunperfect Solar CRM260S156P-60 | Sunperfect Solar CRM260S156P-72 | Sunperfect Solar CRM265S125M-96 | Sunperfect Solar CRM265S156P-72 | Sunperfect Solar CRM270S156P-72 | Sunperfect Solar CRM275S156P-72 | Sunperfect Solar CRM280S156P-72 | Sunperfect Solar CRM285S156P-72 | Sunperfect Solar CRM290S156P-72 | Sunperfect Solar CRM295S156P-72 | Sunperfect Solar CRM300S156P-72 | SunPower PL-PLT-63L-BLK-U | SunPower SPR-76R-BLK-U | SunPower SPR-76RE-BLK-U | SunPower SPR-200-BLK-U | SunPower SPR-200-WHT-U | SunPower SPR-205-BLK-U | SunPower SPR-208-WHT-U | SunPower SPR-210-BLK-U | SunPower SPR-210-WHT-U | SunPower PL-SUNP-SPR-215 | SunPower SPR-215-WHT-U | SunPower SPR-217-WHT-U | SunPower SER-220P | SunPower SPR-220-BLK-U | SunPower SPR-220-WHT-U | SunPower SPR-225-BLK-U | SunPower SPR-225E-BLK-D | SunPower SPR-225E-BLK-U-ACPV | SunPower SPR-225E-WHT-D | SunPower SPR-225NE-BLK-D | SunPower SER-228P | SunPower SPR-230E-WHT-D | SunPower SPR-230NE-BLK-D | SunPower SPR-230NE-BLK-U-ACPV | SunPower SPR-230-WHT-U | SunPower SER-235P | SunPower SPR-235NE-WHT-D | SunPower SPR-E18-235 | SunPower SPR-E19-235 | SunPower T5-SER-235P | SunPower SPR-238E-WHT-D | SunPower SPR-240E-WHT-D | SunPower SPR-240E-WHT-U-ACPV | SunPower SPR-E19-240 | SunPower SPR-X19-240-BLK | SunPower SPR-X19-240-BLK-B-AC | SunPower SPR-245NE-WHT-D | SunPower SPR-245NE-WHT-U-240 ACPV | SunPower SPR-245NE-WHT-U-ACPV | SunPower SPR-E19-245 | SunPower SPR-E20-245 | SunPower SPR-E20-245-A-AC | SunPower SPR-E20-245-B-AC | SunPower SPR-X20-245 | SunPower SPR-250NX-BLK-D | SunPower SPR-X20-250-BLK | SunPower SPR-X20-250-BLK-A-AC | SunPower SPR-X20-250-BLK-B-AC | SunPower SPR-X20-250-BLK-LAM | SunPower SPR-X20-255 | SunPower SPR-X21-255 | SunPower PL-SUNP-SPR-290 | SunPower SPR-290-WHT-U | SunPower T5-SPR-290 | SunPower SPR-295E-WHT-D | SunPower SPR-295E-WHT-U | SunPower SPR-E18-295-COM | SunPower SPR-300E-WHT-D | SunPower SPR-300NE-WHT-D | SunPower SPR-E18-300-COM | SunPower PL-SUNP-SPR-305 | SunPower SPR-305E-WHT-D | SunPower SPR-305E-WHT-U | SunPower SPR-305NE-WHT-D | SunPower SPR-305-WHT-U | SunPower SPR-E18-305-COM | SunPower T5-SPR-305 | SunPower T5-SPR-305E | SunPower PL-SUNP-SPR-308E | SunPower SPR-308E-WHT-D | SunPower SPR-308NE-WHT-D | SunPower T5-SPR-308E | SunPower PL-SUNP-SPR-310 | SunPower SPR-310E-WHT-D | SunPower SPR-310E-WHT-U | SunPower SPR-310-WHT-U | SunPower SPR-E19-310-COM | SunPower T5-SPR-310 | SunPower PL-SUNP-SPR-315E | SunPower SPR-315E-WHT-D | SunPower SPR-315E-WHT-U | SunPower SPR-315NE-WHT-D | SunPower SPR-E19-315 | SunPower SPR-E19-315-COM | SunPower T5-SPR-315 | SunPower T5-SPR-315E | SunPower PL-SUNP-SPR-318E | SunPower SPR-318E-WHT-D | SunPower T5-SPR-318E | SunPower SPR-320E-WHT-D | SunPower SPR-320NE-WHT-D | SunPower SPR-E19-320 | SunPower SPR-E19-320-C-AC | SunPower SPR-E19-320-COM | SunPower SPR-E19-320-D-AC | SunPower T5-SPR-320E | SunPower SPR-P17-325-COM | SunPower SPR-327NE-WHT-D | SunPower SPR-E20-327 | SunPower SPR-E20-327-C-AC | SunPower SPR-E20-327-COM | SunPower SPR-E20-327-COM-LAM | SunPower SPR-E20-327-COM-T5 | SunPower SPR-E20-327-D-AC | SunPower SPR-X20-327 | SunPower SPR-X20-327-BLK | SunPower SPR-X20-327-BLK-C-AC | SunPower SPR-X20-327-BLK-D-AC | SunPower SPR-X20-327-C-AC | SunPower SPR-X20-327-COM | SunPower SPR-X20-327-D-AC | SunPower T5-SPR-327 | SunPower SPR-P17-330-COM | SunPower SPR-335NX-BLK-D | SunPower SPR-P17-335-COM | SunPower SPR-X21-335 | Sunpower SPR-X21-335-BLK | SunPower SPR-X21-335-BLK-C-AC | SunPower SPR-X21-335-BLK-D-AC | SunPower SPR-X21-335-C-AC | Sunpower SPR-X21-335-COM | SunPower SPR-X21-335-D-AC | SunPower SPR-X22-335-BLK | SunPower SPR-P17-340-COM | SunPower SPR-X22-340-BLK | SunPower SPR-343J-WHT-D | SunPower SPR-343NJ-WHT-D | SunPower SPR-343NX-BLK-D | SunPower SPR-343NX-WHT-D | SunPower SPR-P17-345-COM | SunPower SPR-X21-345 | SunPower SPR-X21-345-C-AC | SunPower SPR-X21-345-COM | SunPower SPR-X21-345-D-AC | SunPower SPR-X22-345-BLK | SunPower SPV-P17-345-COM | SunPower SPR-P17-350-COM | SunPower SPR-X21-350-BLK | SunPower SPR-P17-355-COM | SunPower SPR-X22-359 | SunPower SPR-X22-360 | SunPower SPR-X22-360-C-AC | SunPower SPR-X22-360-COM | SunPower SPR-X22-360-D-AC | SunPower SPR-X22-370 | SunPower SPR-X22-370-COM | SunPower SPR-X22-370-D-AC | SunPower SPR-390E-WHT-D | SunPower SPR-400E-WHT-D | SunPower SPR-410NE-WHT-D | SunPower SPR-E19-410-COM | SunPower SPR-415E-WHT-D | Sunpower SPR-E19-415-COM | SunPower SPR-E19-420-COM | Sunpower SPR-425E-WHT-D | SunPower SPR-435NE-WHT-D | SunPower SPR-E20-435-COM | SunPower SPR-440NE-WHT-D | SunPower SPR-E20-440-COM | SunPower SPR-445J-WHT-D | SunPower SPR-445NJ-WHT-D | SunPower SPR-445NX-WHT-D | SunPower SPR-X20-445-COM | Sunpower SPR-X20-450-COM | Sunpower SPR-X21-460-COM | Sunpower SPR-X22-460 | SunPower SPR-X22-460-COM | Sunpower SPR-X21-470-COM | SunPower SPR-X22-470-COM | SunPower SPR-X22-475-COM | Sunpower SPR-X22-480-COM | Sunpreme Inc. SNPM-GX-220 | Sunpreme Inc. SNPM-GX-225 | Sunpreme Inc. SNPM-GX-230 | Sunpreme Inc. SNPM-GX-235 | Sunpreme Inc. SNPM-GX-240 | Sunpreme Inc. SNPM-GX-72-245 | Sunpreme Inc. SNPM-GX-72-250 | Sunpreme Inc. SNPM-GX-72-255 | Sunpreme Inc. SNPM-GxB-270 | Sunpreme Inc. SNPM-GxB-280 | Sunpreme Inc. SNPM-GX-285 | Sunpreme Inc. SNPM-GX-290 | Sunpreme Inc. SNPM-GxB-290 | Sunpreme Inc. SNPM-GxB-290 SM | Sunpreme Inc. SNPM-GxB-SL-290 | Sunpreme Inc. SNPM-GX-295 | Sunpreme Inc. SNPM-GX-300 | Sunpreme Inc. SNPM-GxB-300y | Sunpreme Inc. SNPM-GxB-SL-300 | Sunpreme Inc. SNPM-GX-305 | Sunpreme Inc. SNPM-GX-310 | Sunpreme Inc. SNPM-GxB-310y | Sunpreme Inc. SNPM-GxB-310y SM | Sunpreme Inc. SNPM-GxB-SL-310 | Sunpreme Inc. SNPM-GX-315 | Sunpreme Inc. SNPM-GX-330 | Sunpreme Inc. SNPM-GxB-330 | Sunpreme Inc. SNPM-GX-340 | Sunpreme Inc. SNPM-GxB-340 | Sunpreme Inc. SNPM-GX-350 | Sunpreme Inc. SNPM-GxB-350 | Sunpreme Inc. SNPM-GxB-360 | Sunpreme Inc. SNPM-GxB-370-4BB | Sunpreme Inc. SNPM-GxB-380-4BB | Sunpreme Inc. SNPM-HxB-390 | Sunpreme Inc. SNPM-HxB-395 | Sunpreme Inc. SNPM-HxB-400 | Sunpreme Inc. SNPM-HxB-405 | Sunpreme Inc. SNPM-HxB-410 | Sunpreme Inc. SNPM-HxB-415 | Sunpreme Inc. SNPM-HxB-420 | Sunpreme Inc. SNPM-GxB-490 | Sunpreme Inc. SNPM-GxB-500 | Sunpreme Inc. SNPM-GxB-510 | Sunrise Solartech SR-M572185 | Sunrise Solartech SR-M648185 | Sunrise Solartech SR-M572190 | Sunrise Solartech SR-M648190 | Sunrise Solartech SR-M572195 | Sunrise Solartech SR-M648195 | Sunrise Solartech SR-M572200 | Sunrise Solartech SR-M648200 | Sunrise Solartech SR-M572205 | Sunrise Solartech SR-M648205 | Sunrise Solartech SR-M654210 | Sunrise Solartech SR-M654215 | Sunrise Solartech SR-M654220 | Sunrise Solartech SR-P660220 | Sunrise Solartech SR-M654225 | Sunrise Solartech SR-P660225 | Sunrise Solartech SR-M654230 | Sunrise Solartech SR-P660230 | Sunrise Solartech SR-M660235 | Sunrise Solartech SR-P660235 | Sunrise Solartech SR-M660240 | Sunrise Solartech SR-P660240 | Sunrise Solartech SR-M660245 | Sunrise Solartech SR-M660250 | Sunrise Solartech SR-M660255 | Sunrise Solartech SR-M660260 | Sunrise Solartech SR-P672275 | Sunrise Solartech SR-M672280 | Sunrise Solartech SR-P672280 | Sunrise Solartech SR-M672285 | Sunrise Solartech SR-P672285 | Sunrise Solartech SR-M672290 | Sunrise Solartech SR-P672290 | Sunrise Solartech SR-M672295 | Sunrise Solartech SR-P672295 | Sunrise Solartech SR-M672300 | Sunrise Solartech SR-M672305 | Sunrise Solartech SR-M672310 | Sunspark Technology SMX-245P | Sunspark Technology SMX-250P | Sunspark Technology SMX-255P | Sunspark Technology SMX-260P | Sunspark Technology SMX-265P | Sunspark Technology SST-275M | Sunspark Technology SST-280M | Sunspark Technology SST-285M | Sunspark Technology SST-290M | Sunspark Technology SST-295M | Sunspark Technology SST-300M | Suntech Power STP050D-5/ZCB | Suntech Power STP050D-5/ZCF | Suntech Power STP050D-5/ZCG | Suntech Power STP120D-12/VEC | Suntech Power STP130D-12/VEC | Suntech Power STP135D-12/VEC | Suntech Power STP160S-24/Ab-1 Black | Suntech Power STP165S-24/Ab-1 Black | Suntech Power STP170S-24/Ab-1 | Suntech Power STP170S-24/Ab-1 Black | Suntech Power STP170S-24/Ad+ | Suntech Power STP170S-24/Adb+ | Suntech Power MSZ175B-F | Suntech Power MSZ175J-F | Suntech Power STP175S-24/Ab-1 | Suntech Power STP175S-24/Ab-1 Black | Suntech Power STP175S-24/Ad+ | Suntech Power STP175S-24/Adb+ | Suntech Power MSZ180B-F | Suntech Power MSZ180J-F | Suntech Power STP180S-24/Ab-1 | Suntech Power STP180S-24/Ab-1 Black | Suntech Power STP180S-24/Ad+ | Suntech Power STP180S-24/Adb+ | Suntech Power STP185S-24/Ab-1 | Suntech Power STP185S-24/Ad+ | Suntech Power STP185S-24/Adb | Suntech Power STP185S-24/Adb+ | Suntech Power PLUTO190-Ada | Suntech Power PLUTO190-Adb | Suntech Power PLUTO190-Ade | Suntech Power PLUTO190-Adf | Suntech Power STP190-18/UB-1 | Suntech Power STP190S-24/Ad | Suntech Power STP190S-24/Ad+ | Suntech Power STP190S-24/Adb | Suntech Power STP190S-24/Adb+ | Suntech Power PLUTO195-Ada | Suntech Power PLUTO195-Adb | Suntech Power PLUTO195-Ade | Suntech Power PLUTO195-Adf | Suntech Power STP195S-24/Ad | Suntech Power STP195S-24/Ad+ | Suntech Power STP195S-24/Adb | Suntech Power STP195S-24/Adb+ | Suntech Power PLUTO200-Ada | Suntech Power PLUTO200-Adb | Suntech Power PLUTO200-Ade | Suntech Power PLUTO200-Adf | Suntech Power STP200-18/UB-1 | Suntech Power STP200-18/Ud | Suntech Power PLUTO205-Ada | Suntech Power PLUTO205-Adb | Suntech Power PLUTO205-Ade | Suntech Power PLUTO205-Adf | Suntech Power STP205-18/Ud | Suntech Power PLUTO210-Ada | Suntech Power PLUTO210-Adb | Suntech Power PLUTO210-Ade | Suntech Power PLUTO210-Adf | Suntech Power PLUTO210-Udm | Suntech Power STP210-18/UB-1 | Suntech Power STP210-18/Ud | Suntech Power STP210-20/Wd | Suntech Power STP210-20/Wde | Suntech Power PLUTO215-Udm | Suntech Power STP215-18/Ud | Suntech Power STP215-20/Wd | Suntech Power STP215-20/Wde | Suntech Power PLUTO220-Udm | Suntech Power STP220-18/Ud | Suntech Power STP220-20/Wd | Suntech Power STP220-20/Wde | Suntech Power STP220-20/Wdl | Suntech Power PLUTO225-Udm | Suntech Power STP225-18/Ud | Suntech Power STP225-20/Wd | Suntech Power STP225-20/Wde | Suntech Power STP225-20/Wdl | Suntech Power PLUTO230-Udm | Suntech Power PLUTO230-Wdb | Suntech Power PLUTO230-Wde | Suntech Power PLUTO230-Wdm | Suntech Power STP230-20/Wd | Suntech Power STP230-20/Wde | Suntech Power STP230-20/Wdl | Suntech Power STP230S-20/Wd | Suntech Power STP230S-20/Wdb | Suntech Power STP230S-20/Wde | Suntech Power PLUTO235-Wdb | Suntech Power PLUTO235-Wde | Suntech Power PLUTO235-Wdm | Suntech Power STP235-20/Wd | Suntech Power STP235-20/Wde | Suntech Power STP235-20/Wdl | Suntech Power STP235S-20/Wd | Suntech Power STP235S-20/Wdb | Suntech Power STP235S-20/Wde | Suntech Power PLUTO240-Wdb | Suntech Power PLUTO240-Wde | Suntech Power PLUTO240-Wdm | Suntech Power STP240-20/Wd | Suntech Power STP240-20/Wdb | Suntech Power STP240-20/Wde | Suntech Power STP240-20/Wdl | Suntech Power STP240S-20/Wd | Suntech Power STP240S-20/Wdb | Suntech Power STP240S-20/Wde | Suntech Power PLUTO245-Wdb | Suntech Power PLUTO245-Wde | Suntech Power PLUTO245-Wdm | Suntech Power STP245-20/Wd | Suntech Power STP245-20/Wdb | Suntech Power STP245-20/Wde | Suntech Power STP245S-20/Wd | Suntech Power STP245S-20/Wdb | Suntech Power STP245S-20/Wde | Suntech Power PLUTO250-Wdb | Suntech Power PLUTO250-Wde | Suntech Power PLUTO250-Wdm | Suntech Power STP250-20/Wd | Suntech Power STP250-20/Wdb | Suntech Power STP250-20/Wde | Suntech Power STP250-20/Wem | Suntech Power STP250D-24/VEC | Suntech Power STP250S-20/Wd | Suntech Power STP250S-20/Wdb | Suntech Power STP250S-20/Wde | Suntech Power STP255-20/Wd | Suntech Power STP255-20/Wdb | Suntech Power STP255-20/Wde | Suntech Power STP255-20/Wem | Suntech Power STP255S-20/Wdb | Suntech Power STP255S-20/Wde | Suntech Power STP260-20/Wd | Suntech Power STP260-20/Wdb | Suntech Power STP260-20/Wde | Suntech Power STP260-20/Wem | Suntech Power STP260-24/Vb-1 | Suntech Power STP260-24/Vd | Suntech Power STP260-24/Ve | Suntech Power STP260D-24/VEC | Suntech Power STP260S-20/Wdb | Suntech Power STP260S-20/Wde | Suntech Power STP260-VRM-1 | Suntech Power STP265-20/Wd | Suntech Power STP265-20/Wde | Suntech Power STP265-20/Wem | Suntech Power STP265S-20/Web | Suntech Power STP270-20/Wem | Suntech Power STP270-24/Vb-1 | Suntech Power STP270-24/Vd | Suntech Power STP270-24/Vdx | Suntech Power STP270-24/Ve | Suntech Power STP270D-24/VEC | Suntech Power STP270S-20/Web | Suntech Power STP270-VRM-1 | Suntech Power STP275-24/Vd | Suntech Power STP275-24/Vdx | Suntech Power STP275-24/Ve | Suntech Power STP275S-20/Web | Suntech Power STP275S-20/Wem | Suntech Power STP275S-20/Wew | Suntech Power STP275-VRM-1 | Suntech Power STP275-VRM-1.5 | Suntech Power PLUTO280-Vdm | Suntech Power PLUTO280-Vdx | Suntech Power STP280-24/Vb-1 | Suntech Power STP280-24/Vd | Suntech Power STP280-24/Vdx | Suntech Power STP280-24/Ve | Suntech Power STP280S-20/Web | Suntech Power STP280S-20/Wem | Suntech Power STP280S-20/Wew | Suntech Power STP280-VRM-1 | Suntech Power STP280-VRM-1.5 | Suntech Power PLUTO285-Vdm | Suntech Power PLUTO285-Vdx | Suntech Power STP285-24/Vd | Suntech Power STP285-24/Vdx | Suntech Power STP285-24/Ve | Suntech Power STP285-24/Ver | Suntech Power STP285S-20/Web | Suntech Power STP285S-20/Wem | Suntech Power STP285S-20/Wew | Suntech Power STP285-VRM-1 | Suntech Power STP285-VRM-1.5 | Suntech Power PLUTO290-Vdm | Suntech Power PLUTO290-Vdx | Suntech Power STP290-24/Vd | Suntech Power STP290-24/Vdx | Suntech Power STP290-24/Ve | Suntech Power STP290-24/Ver | Suntech Power STP290S-20/Web | Suntech Power STP290S-20/Wem | Suntech Power STP290S-20/Wew | Suntech Power STP290-VRM-1 | Suntech Power STP290-VRM-1.5 | Suntech Power PLUTO295-Vdm | Suntech Power PLUTO295-Vdx | Suntech Power STP295-24/Vd | Suntech Power STP295-24/Vdx | Suntech Power STP295-24/Ve | Suntech Power STP295-24/Ver | Suntech Power STP295-VRM-1 | Suntech Power STP295-VRM-1.5 | Suntech Power PLUTO300-Vdm | Suntech Power PLUTO300-Vdx | Suntech Power STP300-24/Vd | Suntech Power STP300-24/Vdx | Suntech Power STP300-24/Ve | Suntech Power STP300-24/Ver | Suntech Power STP300-VRM-1 | Suntech Power STP300-VRM-1.5 | Suntech Power PLUTO305-Vdm | Suntech Power PLUTO305-Vdx | Suntech Power STP305-24/Vd | Suntech Power STP305-24/Vdx | Suntech Power STP305-24/Ve | Suntech Power STP305-24/Vem | Suntech Power STP305-24/Ver | Suntech Power STP305-VRM-1 | Suntech Power STP305-VRM-1.5 | Suntech Power PLUTO310-Vdm | Suntech Power PLUTO310-Vdx | Suntech Power STP310-24/Vd | Suntech Power STP310-24/Vdx | Suntech Power STP310-24/Ve | Suntech Power STP310-24/Vem | Suntech Power STP310-24/Ver | Suntech Power STP310-VRM-1 | Suntech Power STP310-VRM-1.5 | Suntech Power STP315-24/Vd | Suntech Power STP315-24/Vdx | Suntech Power STP315-24/Ve | Suntech Power STP315-24/Vem | Suntech Power STP315-24/Ver | Suntech Power STP320-24/Vd | Suntech Power STP320-24/Vdx | Suntech Power STP320-24/Ve | Suntech Power STP320-24/Vem | Suntech Power STP325-24/Vem | Suntech Power STP330-24/Vem | SunTegra STS-110M-B4U | Suntop Solar Energy TOP-S-125M6A | Suntop Solar Energy TOP-S-130M6A | Suntop Solar Energy TOP-S-135M6A | Suntop Solar Energy TOP-S-135S6A | Suntop Solar Energy TOP-S-140M6A | Suntop Solar Energy TOP-S-140S6A | Suntop Solar Energy TOP-S-145S6A | Suntop Solar Energy TOP-S-170M6A | Suntop Solar Energy TOP-S-175M6A | Suntop Solar Energy TOP-S-180M6A | Suntop Solar Energy TOP-S-185M6A | Suntop Solar Energy TOP-S-185S6A | Suntop Solar Energy TOP-S-190M6A | Suntop Solar Energy TOP-S-190S6A | Suntop Solar Energy TOP-S-195M6A | Suntop Solar Energy TOP-S-195S6A | Suntop Solar Energy TOP-S-200M6A | Suntop Solar Energy TOP-S-205M6A | Suntop Solar Energy TOP-S-210M6A | Suntop Solar Energy TOP-H-215M6A | Suntop Solar Energy TOP-S-215M6A | Suntop Solar Energy TOP-H-220M6A | Suntop Solar Energy TOP-H-220S6A | Suntop Solar Energy TOP-S-220M6A | Suntop Solar Energy TOP-S-220S6A | Suntop Solar Energy TOP-H-225M6A | Suntop Solar Energy TOP-H-225S6A | Suntop Solar Energy TOP-S-225M6A | Suntop Solar Energy TOP-S-225S6A | Suntop Solar Energy TOP-H-230M6A | Suntop Solar Energy TOP-H-230S6A | Suntop Solar Energy TOP-S-230M6A | Suntop Solar Energy TOP-S-230S6A | Suntop Solar Energy TOP-H-235M6A | Suntop Solar Energy TOP-H-235S6A | Suntop Solar Energy TOP-S-235M6A | Suntop Solar Energy TOP-S-235S6A | Suntop Solar Energy TOP-H-240S6A | Suntop Solar Energy TOP-S-240S6A | SunWize Technologies SW170 | SunWize Technologies SW175 | SunWize Technologies SW180 | Supreme Solar SS-165M | Supreme Solar SS-170M | Supreme Solar SS-175M | Supreme Solar SS-180M | Supreme Solar SS-200P | Supreme Solar SS-210P | Supreme Solar SS-220P | Supreme Solar SS-230P | Supreme Solar SS-250P | Supreme Solar SS-260P | Supreme Solar SS-270P | Supreme Solar SS-280P | Suzhou Shenglong PV-Tech SLSM-175D | Suzhou Shenglong PV-Tech SLSM-180D | Suzhou Shenglong PV-Tech SLSM-185D | Suzhou Shenglong PV-Tech SLSM-220P | Suzhou Shenglong PV-Tech SLSM-225P | Suzhou Shenglong PV-Tech SLSM-230P | SweModule 220 x | SweModule 225 x | SweModule 230 x | SweModule 235 x | SweModule 240 x | SweModule 245 x | SweModule 250 x | SweModule 255 x | SweModule 260 x | SweModule 265 x | Symphony Energy SE-M215Gy | Symphony Energy SE-M216Gy | Symphony Energy SE-M217Gy | Symphony Energy SE-M218Gy | Symphony Energy SE-M219Gy | Symphony Energy SE-M220Gy | Symphony Energy SE-M221Gy | Symphony Energy SE-M222Gy | Symphony Energy SE-M223Gy | Symphony Energy SE-M224Gy | Symphony Energy OS-M225NA | Symphony Energy SE-M225Gy | Symphony Energy SE-M225NA | Symphony Energy OS-M226NA | Symphony Energy SE-M226Gy | Symphony Energy SE-M226NA | Symphony Energy OS-M227NA | Symphony Energy SE-M227Gy | Symphony Energy SE-M227NA | Symphony Energy OS-M228NA | Symphony Energy OS-S228TA | Symphony Energy SE-M228Gy | Symphony Energy SE-M228NA | Symphony Energy SE-S228TA | Symphony Energy OS-M229NA | Symphony Energy OS-S229TA | Symphony Energy SE-M229Gy | Symphony Energy SE-M229NA | Symphony Energy SE-S229TA | Symphony Energy OS-M230NA | Symphony Energy OS-M230NA3 | Symphony Energy OS-S230TA | Symphony Energy SE-M230Gy | Symphony Energy SE-M230NA | Symphony Energy SE-M230NA3 | Symphony Energy SE-S230TA | Symphony Energy OS-M231NA | Symphony Energy OS-M231NA3 | Symphony Energy OS-S231TA | Symphony Energy SE-M231Gy | Symphony Energy SE-M231NA | Symphony Energy SE-M231NA3 | Symphony Energy SE-S231TA | Symphony Energy OS-M232NA | Symphony Energy OS-M232NA3 | Symphony Energy OS-S232TA | Symphony Energy SE-M232Gy | Symphony Energy SE-M232NA | Symphony Energy SE-M232NA3 | Symphony Energy SE-S232TA | Symphony Energy OS-M233NA | Symphony Energy OS-M233NA3 | Symphony Energy OS-S233TA | Symphony Energy SE-M233Gy | Symphony Energy SE-M233NA | Symphony Energy SE-M233NA3 | Symphony Energy SE-S233TA | Symphony Energy OS-M234NA | Symphony Energy OS-M234NA3 | Symphony Energy OS-S234TA | Symphony Energy SE-M234Gy | Symphony Energy SE-M234NA | Symphony Energy SE-M234NA3 | Symphony Energy SE-S234TA | Symphony Energy OS-M235NA | Symphony Energy OS-M235NA3 | Symphony Energy OS-S235NA3 | Symphony Energy OS-S235TA | Symphony Energy SE-M235Gy | Symphony Energy SE-M235NA | Symphony Energy SE-M235NA3 | Symphony Energy SE-S235NA3 | Symphony Energy SE-S235TA | Symphony Energy OS-M236NA | Symphony Energy OS-M236NA3 | Symphony Energy OS-P236NA3 | Symphony Energy OS-S236NA3 | Symphony Energy OS-S236TA | Symphony Energy SE-M236NA | Symphony Energy SE-M236NA3 | Symphony Energy SE-P236NA3 | Symphony Energy SE-S236NA3 | Symphony Energy SE-S236TA | Symphony Energy OS-M237NA | Symphony Energy OS-M237NA3 | Symphony Energy OS-P237NA3 | Symphony Energy OS-S237NA3 | Symphony Energy OS-S237TA | Symphony Energy SE-M237NA | Symphony Energy SE-M237NA3 | Symphony Energy SE-P237NA3 | Symphony Energy SE-S237NA3 | Symphony Energy SE-S237TA | Symphony Energy OS-M238NA | Symphony Energy OS-M238NA3 | Symphony Energy OS-P238NA3 | Symphony Energy OS-S238NA3 | Symphony Energy OS-S238TA | Symphony Energy SE-M238NA | Symphony Energy SE-M238NA3 | Symphony Energy SE-P238NA3 | Symphony Energy SE-S238NA3 | Symphony Energy SE-S238TA | Symphony Energy OS-M239NA | Symphony Energy OS-M239NA3 | Symphony Energy OS-P239NA3 | Symphony Energy OS-S239NA3 | Symphony Energy OS-S239TA | Symphony Energy SE-M239NA | Symphony Energy SE-M239NA3 | Symphony Energy SE-P239NA3 | Symphony Energy SE-S239NA3 | Symphony Energy SE-S239TA | Symphony Energy OS-M240NA | Symphony Energy OS-M240NA3 | Symphony Energy OS-P240NA3 | Symphony Energy OS-S240NA3 | Symphony Energy OS-S240TA | Symphony Energy SE-M240NA | Symphony Energy SE-M240NA3 | Symphony Energy SE-P240NA3 | Symphony Energy SE-S240NA3 | Symphony Energy SE-S240TA | Symphony Energy OS-M241NA | Symphony Energy OS-M241NA3 | Symphony Energy OS-P241NA3 | Symphony Energy OS-S241NA3 | Symphony Energy OS-S241TA | Symphony Energy SE-M241NA | Symphony Energy SE-M241NA3 | Symphony Energy SE-P241NA3 | Symphony Energy SE-S241NA3 | Symphony Energy SE-S241TA | Symphony Energy OS-M242NA | Symphony Energy OS-M242NA3 | Symphony Energy OS-P242NA3 | Symphony Energy OS-S242NA3 | Symphony Energy OS-S242TA | Symphony Energy SE-M242NA | Symphony Energy SE-M242NA3 | Symphony Energy SE-P242NA3 | Symphony Energy SE-S242NA3 | Symphony Energy SE-S242TA | Symphony Energy OS-M243NA | Symphony Energy OS-M243NA3 | Symphony Energy OS-P243NA3 | Symphony Energy OS-S243NA3 | Symphony Energy OS-S243TA | Symphony Energy SE-M243NA | Symphony Energy SE-M243NA3 | Symphony Energy SE-P243NA3 | Symphony Energy SE-S243NA3 | Symphony Energy SE-S243TA | Symphony Energy OS-M244NA | Symphony Energy OS-M244NA3 | Symphony Energy OS-P244NA3 | Symphony Energy OS-S244NA3 | Symphony Energy OS-S244TA | Symphony Energy SE-M244NA | Symphony Energy SE-M244NA3 | Symphony Energy SE-P244NA3 | Symphony Energy SE-S244NA3 | Symphony Energy SE-S244TA | Symphony Energy OS-M245NA | Symphony Energy OS-M245NA3 | Symphony Energy OS-P245NA3 | Symphony Energy OS-S245NA3 | Symphony Energy OS-S245TA | Symphony Energy SE-M245NA | Symphony Energy SE-M245NA3 | Symphony Energy SE-P245NA3 | Symphony Energy SE-S245NA3 | Symphony Energy SE-S245TA | Symphony Energy OS-M246NA3 | Symphony Energy OS-P246NA3 | Symphony Energy OS-S246NA3 | Symphony Energy OS-S246TA | Symphony Energy SE-M246NA3 | Symphony Energy SE-P246NA3 | Symphony Energy SE-S246NA3 | Symphony Energy SE-S246TA | Symphony Energy OS-M247NA3 | Symphony Energy OS-P247NA3 | Symphony Energy OS-S247NA3 | Symphony Energy OS-S247TA | Symphony Energy SE-M247NA3 | Symphony Energy SE-P247NA3 | Symphony Energy SE-S247NA3 | Symphony Energy SE-S247TA | Symphony Energy OS-M248NA3 | Symphony Energy OS-P248NA3 | Symphony Energy OS-S248NA3 | Symphony Energy OS-S248TA | Symphony Energy SE-M248NA3 | Symphony Energy SE-P248NA3 | Symphony Energy SE-S248NA3 | Symphony Energy SE-S248TA | Symphony Energy OS-M249NA3 | Symphony Energy OS-P249NA3 | Symphony Energy OS-S249NA3 | Symphony Energy OS-S249TA | Symphony Energy SE-M249NA3 | Symphony Energy SE-P249NA3 | Symphony Energy SE-S249NA3 | Symphony Energy SE-S249TA | Symphony Energy OS-M250NA3 | Symphony Energy OS-P250NA3 | Symphony Energy OS-S250NA3 | Symphony Energy OS-S250TA | Symphony Energy SE-M250NA3 | Symphony Energy SE-P250NA3 | Symphony Energy SE-S250NA3 | Symphony Energy SE-S250TA | Symphony Energy OS-P251NA3 | Symphony Energy OS-S251NA3 | Symphony Energy SE-P251NA3 | Symphony Energy SE-S251NA3 | Symphony Energy OS-P252NA3 | Symphony Energy OS-S252NA3 | Symphony Energy SE-P252NA3 | Symphony Energy SE-S252NA3 | Symphony Energy OS-P253NA3 | Symphony Energy OS-S253NA3 | Symphony Energy SE-P253NA3 | Symphony Energy SE-S253NA3 | Symphony Energy OS-P254NA3 | Symphony Energy OS-S254NA3 | Symphony Energy SE-P254NA3 | Symphony Energy SE-S254NA3 | Symphony Energy OS-P255NA3 | Symphony Energy OS-S255NA3 | Symphony Energy SE-P255NA3 | Symphony Energy SE-S255NA3 | Symphony Energy OS-P256NA3 | Symphony Energy SE-P256NA3 | Symphony Energy OS-P257NA3 | Symphony Energy SE-P257NA3 | Symphony Energy OS-P258NA3 | Symphony Energy SE-P258NA3 | Symphony Energy OS-P259NA3 | Symphony Energy SE-P259NA3 | Symphony Energy OS-P260NA3 | Symphony Energy SE-P260NA3 | T & Solar TSS3-228 | T & Solar TSS3-230 | T & Solar TSS3-233 | T & Solar TSS3-235 | T & Solar TSS3-238 | T & Solar TSS3-240 | T & Solar TSS3-243 | T & Solar TSS3-245 | T & Solar TSS3-248 | T & Solar TSS3-250 | Tainergy Tech TKSE-13001 | Tainergy Tech TKSE-13501 | Tainergy Tech TKSE-14001 | Tainergy Tech TKSD-15001 | Tainergy Tech TKSD-15501 | Tainergy Tech TKSD-16001 | Tainergy Tech TKSD-16501 | Tainergy Tech TKSC-17001 | Tainergy Tech TKSC-17501 | Tainergy Tech TKSC-18001 | Tainergy Tech TKSC-18501 | Tainergy Tech TKSC-19001 | Tainergy Tech TKSB-20001 | Tainergy Tech TKSB-20501 | Tainergy Tech TKSB-21001 | Tainergy Tech TKSB-21501 | Tainergy Tech TKSA-22001 | Tainergy Tech TKSB-22001 | Tainergy Tech TKSA-22501 | Tainergy Tech TKSA-23001 | Tainergy Tech TKSA-23501 | Tainergy Tech TKSA-24001 | Tainergy Tech TKSA-24501 | Tainergy Tech TKSA-25001 | Tainergy Tech TKSG-25001 | Tainergy Tech TKSA-25501 | Tainergy Tech TKSG-25501 | Tainergy Tech TKSA-26001 | Tainergy Tech TKSG-26001 | Tainergy Tech TKSG-26501 | Tainergy Tech TKSG-27001 | Tainergy Tech TKSG-27501 | Tainergy Tech TKSG-28001 | Tainergy Tech TKSG-28501 | Tainergy Tech TKSG-29001 | Tainergy Tech TKSG-29501 | Tainergy Tech TKSG-30001 | Tainergy Tech TKSG-30501 | Tainergy Tech TKSG-31001 | Tainergy Tech TKSG-31501 | Taiwan Semiconductor Manufacturing TS-230P4-AD | Taiwan Semiconductor Manufacturing TS-235P4-AD | Taiwan Semiconductor Manufacturing TS-240P4-AD | Taiwan Semiconductor Manufacturing TS-245P4-AD | Taiwan Semiconductor Manufacturing TS-250P4-AD | Talesun Solar TP572M-175 | Talesun Solar TP572M-180 | Talesun Solar TP572M-185 | Talesun Solar TP572M-190 | Talesun Solar TP572M-195 | Talesun Solar TP572M-200 | Talesun Solar TP660M-220 | Talesun Solar TP660P-220 | Talesun Solar TP660M-225 | Talesun Solar TP660P-225 | Talesun Solar TP660M-230 | Talesun Solar TP660P-230 | Talesun Solar TP660M-235 | Talesun Solar TP660P-235 | Talesun Solar TP660M-240 | Talesun Solar TP660M-240B | Talesun Solar TP660P-240 | Talesun Solar TP660P-240B | Talesun Solar TP660M-245 | Talesun Solar TP660M-245B | Talesun Solar TP660P-245 | Talesun Solar TP660P-245B | Talesun Solar TAC208/240 | Talesun Solar TP660AM225 | Talesun Solar TP660AM240 | Talesun Solar TP660M-250 | Talesun Solar TP660M-250B | Talesun Solar TP660P-250 | Talesun Solar TP660P-250B | Talesun Solar TP660M-255 | Talesun Solar TP660M-255B | Talesun Solar TP660P-255 | Talesun Solar TP660P-255B | Talesun Solar TP660M-260 | Talesun Solar TP660M-260B | Talesun Solar TP660P-260 | Talesun Solar TP660M-265 | Talesun Solar TP660P(H)-265 | Talesun Solar TP660P-265 | Talesun Solar TP660M-270 | Talesun Solar TP660P(H)-270 | Talesun Solar TP660P-270 | Talesun Solar TP660M(H)-275 | Talesun Solar TP660M-275 | Talesun Solar TP660P(H)-275 | Talesun Solar TP660P-275 | Talesun Solar TP660M(H)-280 | Talesun Solar TP660M-280 | Talesun Solar TP660P(H)-280 | Talesun Solar TP660P-280 | Talesun Solar TP672P-280 | Talesun Solar TP660M(H)-285 | Talesun Solar TP660M-285 | Talesun Solar TP660P(H)-285 | Talesun Solar TP660P-285 | Talesun Solar TP672M-285 | Talesun Solar TP672M-285B | Talesun Solar TP672P-285 | Talesun Solar TP672P-285B | Talesun Solar TP660M(H)-290 | Talesun Solar TP660M-290 | Talesun Solar TP672M-290 | Talesun Solar TP672M-290B | Talesun Solar TP672P-290 | Talesun Solar TP672P-290B | Talesun Solar TP660M(H)-295 | Talesun Solar TP660M-295 | Talesun Solar TP672M-295 | Talesun Solar TP672M-295B | Talesun Solar TP672P-295 | Talesun Solar TP672P-295B | Talesun Solar TP660M(H)-300 | Talesun Solar TP660M-300 | Talesun Solar TP672M-300 | Talesun Solar TP672M-300B | Talesun Solar TP672P-300 | Talesun Solar TP672P-300B | Talesun Solar TP672M-305 | Talesun Solar TP672M-305B | Talesun Solar TP672P-305 | Talesun Solar TP672M-310 | Talesun Solar TP672M-310B | Talesun Solar TP672P-310 | Talesun Solar TP672M-315 | Talesun Solar TP672P(H)-315 | Talesun Solar TP672P-315 | Talesun Solar TP672M-320 | Talesun Solar TP672P(H)-320 | Talesun Solar TP672P-320 | Talesun Solar TP672M(H)-325 | Talesun Solar TP672M-325 | Talesun Solar TP672P(H)-325 | Talesun Solar TP672P-325 | Talesun Solar TP672M(H)-330 | Talesun Solar TP672M-330 | Talesun Solar TP672P(H)-330 | Talesun Solar TP672P-330 | Talesun Solar TP672M(H)-335 | Talesun Solar TP672M-335 | Talesun Solar TP672P(H)-335 | Talesun Solar TP672P-335 | Talesun Solar TP672M(H)-340 | Talesun Solar TP672M-340 | Talesun Solar TP672P(H)-340 | Talesun Solar TP672P-340 | Talesun Solar TP672M(H)-345 | Talesun Solar TP672M-345 | Talesun Solar TP672P(H)-345 | Talesun Solar TP672P-345 | Talesun Solar TP672M(H)-350 | Talesun Solar TP672M-350 | Talesun Solar TP672M(H)-355 | Talesun Solar TP672M-355 | Talesun Solar TP672M(H)-360 | Talesun Solar TP672M-360 | Tata Power Solar Systems TP140SBZ | Tata Power Solar Systems TP145SBZ | Tata Power Solar Systems TP150SBZ | Tata Power Solar Systems TP235MBZ | Tata Power Solar Systems TP240MBZ | Tata Power Solar Systems TP245MBZ | Tata Power Solar Systems TP250MBZ | Tata Power Solar Systems TP255MBZ | Tata Power Solar Systems TP265LBZ | Tata Power Solar Systems TP270LBZ | Tata Power Solar Systems TP275LBZ | Tata Power Solar Systems TP280LBZ | Tata Power Solar Systems TP285LBZ | Tata Power Solar Systems TP290LBZ | Tata Power Solar Systems TP295LBZ | Tata Power Solar Systems TP300LBZ | Tata Power Solar Systems TP305LBZ | Tata Power Solar Systems TP310LBZ | TBEA Xinjiang SunOasis TBEA4180T | TBEA Xinjiang SunOasis TBEA4185T | TBEA Xinjiang SunOasis TBEA4190T | TBEA Xinjiang SunOasis TBEA3220T | TBEA Xinjiang SunOasis TBEA3225T | TBEA Xinjiang SunOasis TBEA3230T | TBEA Xinjiang SunOasis TBEA3235T | TBEA Xinjiang SunOasis TBEA3240T | TDG Holding T170M725 | TDG Holding T175M725 | TDG Holding T180M725 | TDG Holding T185M725 | TDG Holding T190M725 | TDG Holding T195M725 | TDG Holding T200M725 | TDG Holding T210P606 | TDG Holding T215P606 | TDG Holding T220M606 | TDG Holding T220M965 | TDG Holding T220P606 | TDG Holding T225M606 | TDG Holding T225M965 | TDG Holding T225P606 | TDG Holding T230M606 | TDG Holding T230M965 | TDG Holding T230P606 | TDG Holding T235M606 | TDG Holding T235M965 | TDG Holding T235P606 | TDG Holding T240M606 | TDG Holding T240M965 | TDG Holding T240P606 | TDG Holding T245M606 | TDG Holding T245M965 | TDG Holding T245P606 | TDG Holding T250M606 | TDG Holding T250M965 | TDG Holding T250P606 | TDG Holding T250P726 | TDG Holding T255M606 | TDG Holding T255M726 | TDG Holding T255M965 | TDG Holding T255P726 | TDG Holding T260M726 | TDG Holding T260M965 | TDG Holding T260P726 | TDG Holding T265M726 | TDG Holding T265P726 | TDG Holding T270M726 | TDG Holding T270P726 | TDG Holding T275M726 | TDG Holding T275P726 | TDG Holding T280M726 | TDG Holding T280P726 | TDG Holding T285M726 | TDG Holding T285P726 | TDG Holding T290M726 | TDG Holding T290P726 | TDG Holding T295M726 | TDG Holding T295P726 | TDG Holding T300M726 | TDG Holding T305M726 | Tesla Inc. SR24S3-2 | Tesla Inc. SR24T3-2 | Tesla Inc. SR25S3 | Tesla Inc. SR25T3 | Thaisun Green Energy TSG-180M | Thaisun Green Energy TSG-185M | Thaisun Green Energy TSG-190M | Thaisun Green Energy TSG54-200P | Thaisun Green Energy TSG54-210M | Thaisun Green Energy TSG54-210P | Thaisun Green Energy TSG54-220M | Thaisun Green Energy TSG54-220P | Thaisun Green Energy TSG60-220P | Thaisun Green Energy TSG54-230M | Thaisun Green Energy TSG60-230M | Thaisun Green Energy TSG60-230P | Thaisun Green Energy TSG60-240M | Thaisun Green Energy TSG60-240P | Thaisun Green Energy TSG60-245P | Thaisun Green Energy TSG60-250M | Thaisun Green Energy TSG60-250P | Thaisun Green Energy TSG60-255M | Thaisun Green Energy TSG60-255P | Thaisun Green Energy TSG60-260M | Thaisun Green Energy TSG60-260P | Thaisun Green Energy TSG60-265M | Thaisun Green Energy TSG60-265P | Thaisun Green Energy TSG60-270M | Thaisun Green Energy TSG72-270P | Thaisun Green Energy TSG60-275M | Thaisun Green Energy TSG72-280M | Thaisun Green Energy TSG72-280P | Thaisun Green Energy TSG72-290M | Thaisun Green Energy TSG72-290P | Thaisun Green Energy TSG72-295P | Thaisun Green Energy TSG72-300M | Thaisun Green Energy TSG72-300P | Thaisun Green Energy TSG72-305M | Thaisun Green Energy TSG72-305P | Thaisun Green Energy TSG72-310M | Thaisun Green Energy TSG72-310P | Thaisun Green Energy TSG72-315M | Thaisun Green Energy TSG72-315P | Thaisun Green Energy TSG72-320M | Thaisun Green Energy TSG72-320P | Thaisun Green Energy TSG72-325M | Thaisun Green Energy TSG72-330M | Thaisun Green Energy TSG72-335M | Tianwei EcoSolargy TWES-(155)72M | Tianwei EcoSolargy TWES-(160)72M | Tianwei EcoSolargy TWES-(165)72M | Tianwei EcoSolargy TWES-(170)72M | Tianwei EcoSolargy TWES-(175)72M | Tianwei EcoSolargy TWES-(180)72M | Tianwei EcoSolargy TWES-(200)60P | Tianwei EcoSolargy TWES-(205)60P | Tianwei EcoSolargy TWES-(210)60P | Tianwei EcoSolargy TWES-(215)60P | Tianwei EcoSolargy TWES-(220)60P | Tianwei EcoSolargy TWES-(225)60P | Tianwei EcoSolargy TWES-(230)60P | Tianwei EcoSolargy TWES-(235)60P | Tianwei New Energy (Chengdu) PV Module TW155(35)D | Tianwei New Energy (Chengdu) PV Module TW160(35)D | Tianwei New Energy (Chengdu) PV Module TW165(35)D | Tianwei New Energy (Chengdu) PV Module TW170(35)D | Tianwei New Energy (Chengdu) PV Module TW175(35)D | Tianwei New Energy (Chengdu) PV Module TW180(28)P | Tianwei New Energy (Chengdu) PV Module TW180(35)D | Tianwei New Energy (Chengdu) PV Module TW185(28)P | Tianwei New Energy (Chengdu) PV Module TW185(35)D | Tianwei New Energy (Chengdu) PV Module TW190(28)P | Tianwei New Energy (Chengdu) PV Module TW195(28)P | Tianwei New Energy (Chengdu) PV Module TW200(28)P | Tianwei New Energy (Chengdu) PV Module TW205(28)P | Tianwei New Energy (Chengdu) PV Module TW210(28)P | Tianwei New Energy (Chengdu) PV Module TW215(28)P | Tianwei New Energy (Chengdu) PV Module TW220(28)P | Tianwei New Energy (Chengdu) PV Module TW225(28)P | Tianwei New Energy (Chengdu) PV Module TW230(28)P | Tianwei New Energy (Chengdu) PV Module TW235(28)P | Tianwei New Energy (Yangzhou) TW240P660 | Tianwei New Energy (Yangzhou) TW240P660(1000) | Tianwei New Energy (Yangzhou) TW245P660 | Tianwei New Energy (Yangzhou) TW245P660(1000) | Tianwei New Energy (Yangzhou) TW250M660 | Tianwei New Energy (Yangzhou) TW250M660(1000) | Tianwei New Energy (Yangzhou) TW250P660 | Tianwei New Energy (Yangzhou) TW250P660(1000) | Tianwei New Energy (Yangzhou) TW255M660 | Tianwei New Energy (Yangzhou) TW255M660(1000) | Tianwei New Energy (Yangzhou) TW255P660 | Tianwei New Energy (Yangzhou) TW255P660(1000) | Tianwei New Energy (Yangzhou) TW260M660 | Tianwei New Energy (Yangzhou) TW260M660(1000) | Tianwei New Energy (Yangzhou) TW260P660 | Tianwei New Energy (Yangzhou) TW260P660(1000) | Tianwei New Energy (Yangzhou) TW265M660 | Tianwei New Energy (Yangzhou) TW265M660(1000) | Tianwei New Energy (Yangzhou) TW270M660 | Tianwei New Energy (Yangzhou) TW270M660(1000) | Tianwei New Energy (Yangzhou) TW285P672 | Tianwei New Energy (Yangzhou) TW285P672(1000) | Tianwei New Energy (Yangzhou) TW290M672 | Tianwei New Energy (Yangzhou) TW290M672(1000) | Tianwei New Energy (Yangzhou) TW290P672 | Tianwei New Energy (Yangzhou) TW290P672(1000) | Tianwei New Energy (Yangzhou) TW295M672 | Tianwei New Energy (Yangzhou) TW295M672(1000) | Tianwei New Energy (Yangzhou) TW295P672 | Tianwei New Energy (Yangzhou) TW295P672(1000) | Tianwei New Energy (Yangzhou) TW300M672 | Tianwei New Energy (Yangzhou) TW300M672(1000) | Tianwei New Energy (Yangzhou) TW300P672 | Tianwei New Energy (Yangzhou) TW300P672(1000) | Tianwei New Energy (Yangzhou) TW305M672 | Tianwei New Energy (Yangzhou) TW305M672(1000) | Tianwei New Energy (Yangzhou) TW305P672 | Tianwei New Energy (Yangzhou) TW305P672(1000) | Tianwei New Energy (Yangzhou) TW310M672 | Tianwei New Energy (Yangzhou) TW310M672(1000) | Tianwei New Energy (Yangzhou) TW310P672 | Tianwei New Energy (Yangzhou) TW310P672(1000) | Tianwei New Energy (Yangzhou) TW315M672 | Tianwei New Energy (Yangzhou) TW315M672(1000) | Tianwei New Energy (Yangzhou) TW320M672 | Tianwei New Energy (Yangzhou) TW320M672(1000) | Tianwei New Energy Holdings TW210P60-FA2 | Tianwei New Energy Holdings TW215P60-FA2 | Tianwei New Energy Holdings TW220P60-FA2 | Tianwei New Energy Holdings TW225P60-FA2 | Tianwei New Energy Holdings TW230P60-FA2 | Tianwei New Energy Holdings TW235P60-FA2 | Tianwei New Energy Holdings TW240P60-FA2 | Titan Energy Systems Titan S6-60 | Titan Energy Systems Titan S6-60-2-235 | Titan Energy Systems Titan S6-60-2-240 | Titan Energy Systems Titan S6-60-2-245 | Tongwei Solar (Hefei) TW240P-60 | Tongwei Solar (Hefei) TW245P-60 | Tongwei Solar (Hefei) TW250P-60 | Tongwei Solar (Hefei) TW255P-60 | Tongwei Solar (Hefei) TW260P-60 | Tongwei Solar (Hefei) TW285P-72 | Tongwei Solar (Hefei) TW290P-72 | Tongwei Solar (Hefei) TW295P-72 | Tongwei Solar (Hefei) TW300P-72 | Tongwei Solar (Hefei) TW305P-72 | Tongwei Solar (Hefei) TW310P-72 | Top Solar TSC-200W-E | Topsun TS-M228NA1 | Topsun TS-M229NA1 | Topsun TS-M230NA1 | Topsun TS-M231NA1 | Topsun TS-M232NA1 | Topsun TS-M233NA1 | Topsun TS-M234NA1 | Topsun TS-M235NA1 | Topsun TS-M236NA1 | Topsun TS-M237NA1 | Topsun TS-M238NA1 | Topsun TS-S238SA1K | Topsun TS-S238TA1 | Topsun TS-M239NA1 | Topsun TS-S239SA1K | Topsun TS-S239TA1 | Topsun TS-M240NA1 | Topsun TS-S240SA1K | Topsun TS-S240TA1 | Topsun TS-M241NA1 | Topsun TS-S241SA1K | Topsun TS-S241TA1 | Topsun TS-M242NA1 | Topsun TS-S242SA1K | Topsun TS-S242TA1 | Topsun TS-M243NA1 | Topsun TS-S243SA1K | Topsun TS-S243TA1 | Topsun TS-M244NA1 | Topsun TS-S244SA1K | Topsun TS-S244TA1 | Topsun TS-M245NA1 | Topsun TS-S245SA1K | Topsun TS-S245TA1 | Topsun TS-M246NA1 | Topsun TS-S246SA1K | Topsun TS-S246TA1 | Topsun TS-M247NA1 | Topsun TS-S247SA1K | Topsun TS-S247TA1 | Topsun TS-M248NA1 | Topsun TS-S248SA1K | Topsun TS-S248TA1 | Topsun TS-M249NA1 | Topsun TS-S249SA1K | Topsun TS-S249TA1 | Topsun TS-M250NA1 | Topsun TS-S250SA1 | Topsun TS-S250SA1K | Topsun TS-S250TA1 | Topsun TS-M251NA1 | Topsun TS-S251SA1K | Topsun TS-S251TA1 | Topsun TS-M252NA1 | Topsun TS-S252SA1K | Topsun TS-S252TA1 | Topsun TS-S253SA1K | Topsun TS-S253TA1 | Topsun TS-S254SA1K | Topsun TS-S254TA1 | Topsun TS-S255SA1 | Topsun TS-S255SA1K | Topsun TS-S255TA1 | Topsun TS-S256SA1K | Topsun TS-S256TA1 | Topsun TS-S257SA1K | Topsun TS-S257TA1 | Topsun TS-S258SA1K | Topsun TS-S258TA1 | Topsun TS-S259SA1K | Topsun TS-S259TA1 | Topsun TS-S260SA1 | Topsun TS-S260SA1K | Topsun TS-S260TA1 | Topsun TS-S261SA1K | Topsun TS-S261TA1 | Topsun TS-S262SA1K | Topsun TS-S262TA1 | Topsun TS-S286SA1K | Topsun TS-S287SA1K | Topsun TS-S288SA1K | Topsun TS-S289SA1K | Topsun TS-S290SA1K | Topsun TS-S291SA1K | Topsun TS-S292SA1K | Topsun TS-S293SA1K | Topsun TS-S294SA1K | Topsun TS-S295SA1K | Topsun TS-S296SA1K | Topsun TS-S297SA1K | Topsun TS-S298SA1K | Topsun TS-S299SA1K | Topsun TS-S300SA1 | Topsun TS-S300SA1K | Topsun TS-S301SA1K | Topsun TS-S302SA1K | Topsun TS-S303SA1K | Topsun TS-S304SA1K | Topsun TS-S305SA1 | Topsun TS-S305SA1K | Topsun TS-S306SA1K | Topsun TS-S307SA1K | Topsun TS-S308SA1K | Topsun TS-S309SA1K | Topsun TS-S310SA1 | Topsun TS-S310SA1K | Topsun TS-S311SA1K | Topsun TS-S312SA1K | Topsun TS-S313SA1K | Topsun TS-S314SA1K | Topsun TS-S356TA1 | Topsun TS-S357TA1 | Topsun TS-S358TA1 | Topsun TS-S359TA1 | Topsun TS-S360TA1 | Topsun TS-M361NA1 | Topsun TS-S361TA1 | Topsun TS-M362NA1 | Topsun TS-S362TA1 | Topsun TS-M363NA1 | Topsun TS-S363TA1 | Topsun TS-M364NA1 | Topsun TS-S364TA1 | Topsun TS-M365NA1 | Topsun TS-S365TA1 | Topsun TS-M366NA1 | Topsun TS-S366TA1 | Topsun TS-M367NA1 | Topsun TS-S367TA1 | Topsun TS-M368NA1 | Topsun TS-S368TA1 | Topsun TS-M369NA1 | Topsun TS-S369TA1 | Topsun TS-M370NA1 | Topsun TS-S370 | Topsun TS-S370TA1 | Topsun TS-M371NA1 | Topsun TS-S371 | Topsun TS-S371TA1 | Topsun TS-M372NA1 | Topsun TS-S372 | Topsun TS-S372TA1 | Topsun TS-M373NA1 | Topsun TS-S373 | Topsun TS-S373TA1 | Topsun TS-M374NA1 | Topsun TS-S374 | Topsun TS-S374TA1 | Topsun TS-M375NA1 | Topsun TS-S375 | Topsun TS-S375TA1 | Topsun TS-M376NA1 | Topsun TS-S376 | Topsun TS-S376TA1 | Topsun TS-M377NA1 | Topsun TS-S377 | Topsun TS-S377TA1 | Topsun TS-M378NA1 | Topsun TS-S378 | Topsun TS-S378TA1 | Topsun TS-M379NA1 | Topsun TS-S379 | Topsun TS-S379TA1 | Topsun TS-M380NA1 | Topsun TS-S380 | Topsun TS-S380SA1 | Topsun TS-S380TA1 | Topsun TS-S380VA1 | Topsun TS-M381JA1 | Topsun TS-M381NA1 | Topsun TS-S381 | Topsun TS-S381SA1 | Topsun TS-S381SA1K | Topsun TS-S381TA1 | Topsun TS-S381VA1 | Topsun TS-M382JA1 | Topsun TS-M382NA1 | Topsun TS-S382 | Topsun TS-S382SA1 | Topsun TS-S382SA1K | Topsun TS-S382TA1 | Topsun TS-S382VA1 | Topsun TS-M383JA1 | Topsun TS-M383NA1 | Topsun TS-S383 | Topsun TS-S383SA1 | Topsun TS-S383SA1K | Topsun TS-S383TA1 | Topsun TS-S383VA1 | Topsun TS-M384JA1 | Topsun TS-M384NA1 | Topsun TS-S384 | Topsun TS-S384SA1 | Topsun TS-S384SA1K | Topsun TS-S384TA1 | Topsun TS-S384VA1 | Topsun TS-M385JA1 | Topsun TS-M385NA1 | Topsun TS-S385 | Topsun TS-S385SA1 | Topsun TS-S385SA1K | Topsun TS-S385TA1 | Topsun TS-S385VA1 | Topsun TS-M386JA1 | Topsun TS-M386NA1 | Topsun TS-S386 | Topsun TS-S386SA1 | Topsun TS-S386SA1K | Topsun TS-S386TA1 | Topsun TS-S386VA1 | Topsun TS-M387JA1 | Topsun TS-M387NA1 | Topsun TS-S387 | Topsun TS-S387SA1 | Topsun TS-S387SA1K | Topsun TS-S387TA1 | Topsun TS-S387VA1 | Topsun TS-M388JA1 | Topsun TS-M388NA1 | Topsun TS-S388 | Topsun TS-S388SA1 | Topsun TS-S388SA1K | Topsun TS-S388TA1 | Topsun TS-S388VA1 | Topsun TS-M389JA1 | Topsun TS-M389NA1 | Topsun TS-S389 | Topsun TS-S389SA1 | Topsun TS-S389SA1K | Topsun TS-S389TA1 | Topsun TS-S389VA1 | Topsun TS-M390JA1 | Topsun TS-M390NA1 | Topsun TS-S390 | Topsun TS-S390SA1 | Topsun TS-S390SA1K | Topsun TS-S390TA1 | Topsun TS-S390VA1 | Topsun TS-M391JA1 | Topsun TS-M391NA1 | Topsun TS-S391 | Topsun TS-S391SA1 | Topsun TS-S391SA1K | Topsun TS-S391TA1 | Topsun TS-S391VA1 | Topsun TS-M392JA1 | Topsun TS-M392NA1 | Topsun TS-S392 | Topsun TS-S392SA1 | Topsun TS-S392SA1K | Topsun TS-S392TA1 | Topsun TS-S392VA1 | Topsun TS-M393JA1 | Topsun TS-M393NA1 | Topsun TS-S393 | Topsun TS-S393SA1 | Topsun TS-S393SA1K | Topsun TS-S393TA1 | Topsun TS-S393VA1 | Topsun TS-M394JA1 | Topsun TS-M394NA1 | Topsun TS-S394 | Topsun TS-S394SA1 | Topsun TS-S394SA1K | Topsun TS-S394TA1 | Topsun TS-S394VA1 | Topsun TS-M395JA1 | Topsun TS-M395NA1 | Topsun TS-S395 | Topsun TS-S395SA1 | Topsun TS-S395SA1K | Topsun TS-S395TA1 | Topsun TS-S395VA1 | Topsun TS-M396JA1 | Topsun TS-M396NA1 | Topsun TS-S396 | Topsun TS-S396SA1 | Topsun TS-S396SA1K | Topsun TS-S396TA1 | Topsun TS-S396VA1 | Topsun TS-M397JA1 | Topsun TS-M397NA1 | Topsun TS-S397 | Topsun TS-S397SA1 | Topsun TS-S397SA1K | Topsun TS-S397TA1 | Topsun TS-S397VA1 | Topsun TS-M398JA1 | Topsun TS-M398NA1 | Topsun TS-S398 | Topsun TS-S398SA1 | Topsun TS-S398SA1K | Topsun TS-S398TA1 | Topsun TS-S398VA1 | Topsun TS-M399JA1 | Topsun TS-M399NA1 | Topsun TS-S399 | Topsun TS-S399SA1 | Topsun TS-S399SA1K | Topsun TS-S399TA1 | Topsun TS-S399VA1 | Topsun TS-M400JA1 | Topsun TS-S400 | Topsun TS-S400SA1 | Topsun TS-S400SA1K | Topsun TS-S400TA1 | Topsun TS-S400VA1 | Topsun TS-M401JA1 | Topsun TS-S401 | Topsun TS-S401SA1 | Topsun TS-S401SA1K | Topsun TS-S401TA1 | Topsun TS-S401VA1 | Topsun TS-M402JA1 | Topsun TS-S402 | Topsun TS-S402SA1 | Topsun TS-S402SA1K | Topsun TS-S402TA1 | Topsun TS-S402VA1 | Topsun TS-M403JA1 | Topsun TS-S403 | Topsun TS-S403SA1 | Topsun TS-S403SA1K | Topsun TS-S403TA1 | Topsun TS-S403VA1 | Topsun TS-M404JA1 | Topsun TS-S404 | Topsun TS-S404SA1 | Topsun TS-S404SA1K | Topsun TS-S404TA1 | Topsun TS-S404VA1 | Topsun TS-M405JA1 | Topsun TS-S405 | Topsun TS-S405SA1 | Topsun TS-S405SA1K | Topsun TS-S405TA1 | Topsun TS-S405VA1 | Topsun TS-M406JA1 | Topsun TS-S406 | Topsun TS-S406SA1 | Topsun TS-S406SA1K | Topsun TS-S406TA1 | Topsun TS-S406VA1 | Topsun TS-M407JA1 | Topsun TS-S407 | Topsun TS-S407SA1 | Topsun TS-S407SA1K | Topsun TS-S407TA1 | Topsun TS-S407VA1 | Topsun TS-M408JA1 | Topsun TS-S408 | Topsun TS-S408SA1 | Topsun TS-S408SA1K | Topsun TS-S408TA1 | Topsun TS-S408VA1 | Topsun TS-M409JA1 | Topsun TS-S409 | Topsun TS-S409SA1 | Topsun TS-S409SA1K | Topsun TS-S409TA1 | Topsun TS-S409VA1 | Topsun TS-M410JA1 | Topsun TS-S410 | Topsun TS-S410SA1 | Topsun TS-S410SA1K | Topsun TS-S410TA1 | Topsun TS-S410VA1 | Topsun TS-M411JA1 | Topsun TS-S411SA1 | Topsun TS-S411SA1K | Topsun TS-S411TA1 | Topsun TS-S411VA1 | Topsun TS-M412JA1 | Topsun TS-S412SA1 | Topsun TS-S412SA1K | Topsun TS-S412TA1 | Topsun TS-S412VA1 | Topsun TS-M413JA1 | Topsun TS-S413SA1 | Topsun TS-S413SA1K | Topsun TS-S413TA1 | Topsun TS-S413VA1 | Topsun TS-M414JA1 | Topsun TS-S414SA1 | Topsun TS-S414SA1K | Topsun TS-S414TA1 | Topsun TS-S414VA1 | Topsun TS-M415JA1 | Topsun TS-S415SA1 | Topsun TS-S415SA1K | Topsun TS-S415TA1 | Topsun TS-S415VA1 | Topsun TS-M416JA1 | Topsun TS-S416SA1 | Topsun TS-S416SA1K | Topsun TS-S416TA1 | Topsun TS-S416VA1 | Topsun TS-M417JA1 | Topsun TS-S417SA1 | Topsun TS-S417SA1K | Topsun TS-S417TA1 | Topsun TS-S417VA1 | Topsun TS-M418JA1 | Topsun TS-S418SA1 | Topsun TS-S418SA1K | Topsun TS-S418TA1 | Topsun TS-S418VA1 | Topsun TS-M419JA1 | Topsun TS-S419SA1 | Topsun TS-S419SA1K | Topsun TS-S419TA1 | Topsun TS-M420JA1 | Topsun TS-S420SA1 | Topsun TS-S420TA1 | Trina Solar TSM-160PEG40.07 | Trina Solar TSM-165DA01 | Trina Solar TSM-165PEG40.07 | Trina Solar TSM-170D | Trina Solar TSM-170DA01 | Trina Solar TSM-170DA03 | Trina Solar TSM-170PA03 | Trina Solar TSM-170PEG40.07 | Trina Solar TSM-175D | Trina Solar TSM-175DA01 | Trina Solar TSM-175DA03 | Trina Solar TSM-175PA03 | Trina Solar TSM-175PEG40.07 | Trina Solar TSM-180D | Trina Solar TSM-180DA01 | Trina Solar TSM-180DA03 | Trina Solar TSM-180PA03 | Trina Solar TSM-185DA01 | Trina Solar TSM-185DA01A | Trina Solar TSM-185DA01A.05 | Trina Solar TSM-185DA01A.08 | Trina Solar TSM-185DA03 | Trina Solar TSM-185PA03 | Trina Solar TSM-190DA01A | Trina Solar TSM-190DA01A.05 | Trina Solar TSM-190DA01A.08 | Trina Solar TSM-190DA03 | Trina Solar TSM-190PA03 | Trina Solar TSM-195DA01A | Trina Solar TSM-195DA01A.05 | Trina Solar TSM-195DA01A.08 | Trina Solar TSM-200DA01A | Trina Solar TSM-200DA01A.05 | Trina Solar TSM-200DA01A.08 | Trina Solar TSM-205DA01A | Trina Solar TSM-205DA01A.05 | Trina Solar TSM-205DA01A.08 | Trina Solar TSM-220DA05 | Trina Solar TSM-220PA05 | Trina Solar TSM-220PA05.05 | Trina Solar TSM-220PA05.08 | Trina Solar TSM-220PA05.10 | Trina Solar TSM-220PA05.15 | Trina Solar TSM-220PA05.18 | Trina Solar TSM-220PA05.20 | Trina Solar TSM-220PA05.28 | Trina Solar TSM-220PA05.30 | Trina Solar TSM-220PA05.38 | Trina Solar TSM-220PA05.xy2 | Trina Solar TSM-220PD05 | Trina Solar TSM-220PD05.08 | Trina Solar TSM-220PD05.10 | Trina Solar TSM-220PD05.18 | Trina Solar TSM-220PD05.xy2 | Trina Solar TSM-225PA05 | Trina Solar TSM-225PA05.05 | Trina Solar TSM-225PA05.08 | Trina Solar TSM-225PA05.10 | Trina Solar TSM-225PA05.15 | Trina Solar TSM-225PA05.18 | Trina Solar TSM-225PA05.20 | Trina Solar TSM-225PA05.28 | Trina Solar TSM-225PA05.30 | Trina Solar TSM-225PA05.38 | Trina Solar TSM-225PA05.xy2 | Trina Solar TSM-225PD05 | Trina Solar TSM-225PD05.08 | Trina Solar TSM-225PD05.10 | Trina Solar TSM-225PD05.18 | Trina Solar TSM-225PD05.xy2 | Trina Solar TSM-230DA05 | Trina Solar TSM-230PA05 | Trina Solar TSM-230PA05.05 | Trina Solar TSM-230PA05.08 | Trina Solar TSM-230PA05.10 | Trina Solar TSM-230PA05.15 | Trina Solar TSM-230PA05.18 | Trina Solar TSM-230PA05.20 | Trina Solar TSM-230PA05.28 | Trina Solar TSM-230PA05.30 | Trina Solar TSM-230PA05.38 | Trina Solar TSM-230PA05.xy2 | Trina Solar TSM-230PD05 | Trina Solar TSM-230PD05.08 | Trina Solar TSM-230PD05.10 | Trina Solar TSM-230PD05.18 | Trina Solar TSM-230PD05.xy2 | Trina Solar TSM-235PA05 | Trina Solar TSM-235PA05.05 | Trina Solar TSM-235PA05.08 | Trina Solar TSM-235PA05.10 | Trina Solar TSM-235PA05.15 | Trina Solar TSM-235PA05.18 | Trina Solar TSM-235PA05.20 | Trina Solar TSM-235PA05.28 | Trina Solar TSM-235PA05.30 | Trina Solar TSM-235PA05.38 | Trina Solar TSM-235PA05.xy2 | Trina Solar TSM-235PD05 | Trina Solar TSM-235PD05.08 | Trina Solar TSM-235PD05.10 | Trina Solar TSM-235PD05.18 | Trina Solar TSM-235PD05.xy2 | Trina Solar TSM-240DA05 | Trina Solar TSM-240PA05 | Trina Solar TSM-240PA05.05 | Trina Solar TSM-240PA05.08 | Trina Solar TSM-240PA05.10 | Trina Solar TSM-240PA05.15 | Trina Solar TSM-240PA05.18 | Trina Solar TSM-240PA05.20 | Trina Solar TSM-240PA05.28 | Trina Solar TSM-240PA05.30 | Trina Solar TSM-240PA05.38 | Trina Solar TSM-240PA05.xy2 | Trina Solar TSM-240PD05 | Trina Solar TSM-240PD05.08 | Trina Solar TSM-240PD05.10 | Trina Solar TSM-240PD05.18 | Trina Solar TSM-240PD05.xy2 | Trina Solar TSM-240PxG5 | Trina Solar TSM-240PxG5.50 | Trina Solar TSM-245PA05 | Trina Solar TSM-245PA05.05 | Trina Solar TSM-245PA05.08 | Trina Solar TSM-245PA05.10 | Trina Solar TSM-245PA05.15 | Trina Solar TSM-245PA05.18 | Trina Solar TSM-245PA05.20 | Trina Solar TSM-245PA05.28 | Trina Solar TSM-245PA05.30 | Trina Solar TSM-245PA05.38 | Trina Solar TSM-245PA05.xy2 | Trina Solar TSM-245PD05 | Trina Solar TSM-245PD05.001 | Trina Solar TSM-245PD05.002 | Trina Solar TSM-245PD05.00C | Trina Solar TSM-245PD05.00M | Trina Solar TSM-245PD05.00S | Trina Solar TSM-245PD05.051 | Trina Solar TSM-245PD05.052 | Trina Solar TSM-245PD05.05M | Trina Solar TSM-245PD05.05S | Trina Solar TSM-245PD05.08 | Trina Solar TSM-245PD05.081 | Trina Solar TSM-245PD05.082 | Trina Solar TSM-245PD05.08C | Trina Solar TSM-245PD05.08D | Trina Solar TSM-245PD05.08M | Trina Solar TSM-245PD05.08S | Trina Solar TSM-245PD05.10 | Trina Solar TSM-245PD05.18 | Trina Solar TSM-245PD05.xy2 | Trina Solar TSM-245PxG5 | Trina Solar TSM-245PxG5.50 | Trina Solar TSM-250PA05 | Trina Solar TSM-250PA05.05 | Trina Solar TSM-250PA05.08 | Trina Solar TSM-250PA05.10 | Trina Solar TSM-250PA05.15 | Trina Solar TSM-250PA05.18 | Trina Solar TSM-250PA05.20 | Trina Solar TSM-250PA05.28 | Trina Solar TSM-250PA05.30 | Trina Solar TSM-250PA05.38 | Trina Solar TSM-250PA05.xy2 | Trina Solar TSM-250PA05A | Trina Solar TSM-250PA05A.08 | Trina Solar TSM-250PA05A.10 | Trina Solar TSM-250PA05A.18 | Trina Solar TSM-250PD05 | Trina Solar TSM-250PD05.001 | Trina Solar TSM-250PD05.002 | Trina Solar TSM-250PD05.00C | Trina Solar TSM-250PD05.00M | Trina Solar TSM-250PD05.00S | Trina Solar TSM-250PD05.00U | Trina Solar TSM-250PD05.05 | Trina Solar TSM-250PD05.051 | Trina Solar TSM-250PD05.052 | Trina Solar TSM-250PD05.05M | Trina Solar TSM-250PD05.05S | Trina Solar TSM-250PD05.05U | Trina Solar TSM-250PD05.08 | Trina Solar TSM-250PD05.081 | Trina Solar TSM-250PD05.082 | Trina Solar TSM-250PD05.08C | Trina Solar TSM-250PD05.08D | Trina Solar TSM-250PD05.08M | Trina Solar TSM-250PD05.08S | Trina Solar TSM-250PD05.08U | Trina Solar TSM-250PD05.10 | Trina Solar TSM-250PD05.18 | Trina Solar TSM-250PD05.xy2 | Trina Solar TSM-250PDG5 | Trina Solar TSM-250PE05A | Trina Solar TSM-250PE05A.08 | Trina Solar TSM-250PEG5 | Trina Solar TSM-250PEG5.07 | Trina Solar TSM-250PxG5 | Trina Solar TSM-250PxG5.50 | Trina Solar TSM-255PA05 | Trina Solar TSM-255PA05.05 | Trina Solar TSM-255PA05.08 | Trina Solar TSM-255PA05.10 | Trina Solar TSM-255PA05.18 | Trina Solar TSM-255PA05.20 | Trina Solar TSM-255PA05.28 | Trina Solar TSM-255PA05.30 | Trina Solar TSM-255PA05.38 | Trina Solar TSM-255PA05.xy2 | Trina Solar TSM-255PA05A | Trina Solar TSM-255PA05A.08 | Trina Solar TSM-255PA05A.10 | Trina Solar TSM-255PA05A.18 | Trina Solar TSM-255PD05 | Trina Solar TSM-255PD05.001 | Trina Solar TSM-255PD05.002 | Trina Solar TSM-255PD05.00C | Trina Solar TSM-255PD05.00M | Trina Solar TSM-255PD05.00S | Trina Solar TSM-255PD05.05 | Trina Solar TSM-255PD05.051 | Trina Solar TSM-255PD05.052 | Trina Solar TSM-255PD05.05M | Trina Solar TSM-255PD05.05S | Trina Solar TSM-255PD05.08 | Trina Solar TSM-255PD05.081 | Trina Solar TSM-255PD05.082 | Trina Solar TSM-255PD05.08C | Trina Solar TSM-255PD05.08D | Trina Solar TSM-255PD05.08M | Trina Solar TSM-255PD05.08S | Trina Solar TSM-255PD05.10 | Trina Solar TSM-255PD05.18 | Trina Solar TSM-255PD05.xy2 | Trina Solar TSM-255PDG5 | Trina Solar TSM-255PE05A | Trina Solar TSM-255PE05A.08 | Trina Solar TSM-255PEG5 | Trina Solar TSM-255PEG5.07 | Trina Solar TSM-255PxG5 | Trina Solar TSM-255PxG5.50 | Trina Solar TSM-260PA05 | Trina Solar TSM-260PA05.05 | Trina Solar TSM-260PA05.08 | Trina Solar TSM-260PA05.10 | Trina Solar TSM-260PA05.18 | Trina Solar TSM-260PA05.20 | Trina Solar TSM-260PA05.28 | Trina Solar TSM-260PA05.30 | Trina Solar TSM-260PA05.38 | Trina Solar TSM-260PA05.xy2 | Trina Solar TSM-260PA05A | Trina Solar TSM-260PA05A.08 | Trina Solar TSM-260PA05A.10 | Trina Solar TSM-260PA05A.18 | Trina Solar TSM-260PD05 | Trina Solar TSM-260PD05.001 | Trina Solar TSM-260PD05.002 | Trina Solar TSM-260PD05.00C | Trina Solar TSM-260PD05.00M | Trina Solar TSM-260PD05.00S | Trina Solar TSM-260PD05.05 | Trina Solar TSM-260PD05.051 | Trina Solar TSM-260PD05.052 | Trina Solar TSM-260PD05.05M | Trina Solar TSM-260PD05.05S | Trina Solar TSM-260PD05.08 | Trina Solar TSM-260PD05.081 | Trina Solar TSM-260PD05.082 | Trina Solar TSM-260PD05.08C | Trina Solar TSM-260PD05.08D | Trina Solar TSM-260PD05.08M | Trina Solar TSM-260PD05.08S | Trina Solar TSM-260PD05.10 | Trina Solar TSM-260PD05.18 | Trina Solar TSM-260PD05.18D | Trina Solar TSM-260PD05.xy2 | Trina Solar TSM-260PDG5 | Trina Solar TSM-260PE05A | Trina Solar TSM-260PE05A.08 | Trina Solar TSM-260PEG5 | Trina Solar TSM-260PEG5.07 | Trina Solar TSM-260PEG5.40 | Trina Solar TSM-260PEG5.47 | Trina Solar TSM-260PxG5 | Trina Solar TSM-260PxG5.50 | Trina Solar TSM-265PA05.05 | Trina Solar TSM-265PA05A | Trina Solar TSM-265PA05A.08 | Trina Solar TSM-265PA05A.10 | Trina Solar TSM-265PA05A.18 | Trina Solar TSM-265PD05 | Trina Solar TSM-265PD05.001 | Trina Solar TSM-265PD05.002 | Trina Solar TSM-265PD05.00C | Trina Solar TSM-265PD05.00M | Trina Solar TSM-265PD05.00S | Trina Solar TSM-265PD05.05 | Trina Solar TSM-265PD05.051 | Trina Solar TSM-265PD05.052 | Trina Solar TSM-265PD05.05M | Trina Solar TSM-265PD05.05S | Trina Solar TSM-265PD05.08 | Trina Solar TSM-265PD05.081 | Trina Solar TSM-265PD05.082 | Trina Solar TSM-265PD05.08C | Trina Solar TSM-265PD05.08D | Trina Solar TSM-265PD05.08M | Trina Solar TSM-265PD05.08S | Trina Solar TSM-265PD05.10 | Trina Solar TSM-265PD05.102 | Trina Solar TSM-265PD05.18 | Trina Solar TSM-265PD05.182 | Trina Solar TSM-265PD05.18D | Trina Solar TSM-265PDG5 | Trina Solar TSM-265PE05A | Trina Solar TSM-265PE05A.08 | Trina Solar TSM-265PEG5 | Trina Solar TSM-265PEG5.07 | Trina Solar TSM-265PEG5.40 | Trina Solar TSM-265PEG5.47 | Trina Solar TSM-270DD05A | Trina Solar TSM-270DD05A(II) | Trina Solar TSM-270DD05A.05 | Trina Solar TSM-270DD05A.05(II) | Trina Solar TSM-270DD05A.08 | Trina Solar TSM-270DD05A.08(II) | Trina Solar TSM-270PA05A | Trina Solar TSM-270PA05A.08 | Trina Solar TSM-270PA05A.10 | Trina Solar TSM-270PA05A.18 | Trina Solar TSM-270PA14 | Trina Solar TSM-270PA14.05 | Trina Solar TSM-270PA14.08 | Trina Solar TSM-270PA14.0x2 | Trina Solar TSM-270PA14.10 | Trina Solar TSM-270PA14.18 | Trina Solar TSM-270PA14.20 | Trina Solar TSM-270PA14.28 | Trina Solar TSM-270PD05 | Trina Solar TSM-270PD05.001 | Trina Solar TSM-270PD05.002 | Trina Solar TSM-270PD05.00C | Trina Solar TSM-270PD05.00D | Trina Solar TSM-270PD05.00M | Trina Solar TSM-270PD05.00S | Trina Solar TSM-270PD05.00U | Trina Solar TSM-270PD05.05 | Trina Solar TSM-270PD05.051 | Trina Solar TSM-270PD05.052 | Trina Solar TSM-270PD05.05C | Trina Solar TSM-270PD05.05D | Trina Solar TSM-270PD05.05M | Trina Solar TSM-270PD05.05S | Trina Solar TSM-270PD05.05U | Trina Solar TSM-270PD05.08 | Trina Solar TSM-270PD05.081 | Trina Solar TSM-270PD05.082 | Trina Solar TSM-270PD05.08C | Trina Solar TSM-270PD05.08D | Trina Solar TSM-270PD05.08M | Trina Solar TSM-270PD05.08S | Trina Solar TSM-270PD05.08U | Trina Solar TSM-270PD05.10 | Trina Solar TSM-270PD05.10C | Trina Solar TSM-270PD05.10D | Trina Solar TSM-270PD05.15 | Trina Solar TSM-270PD05.15C | Trina Solar TSM-270PD05.15D | Trina Solar TSM-270PD05.18 | Trina Solar TSM-270PD05.18C | Trina Solar TSM-270PD05.18D | Trina Solar TSM-270PD14.08 | Trina Solar TSM-270PD14.0x2 | Trina Solar TSM-270PD14.10 | Trina Solar TSM-270PD14.18 | Trina Solar TSM-270PE05A | Trina Solar TSM-270PE05A.08 | Trina Solar TSM-270PEG5 | Trina Solar TSM-270PEG5.07 | Trina Solar TSM-270PEG5.40 | Trina Solar TSM-270PEG5.47 | Trina Solar TSM-275DD05A(II) | Trina Solar TSM-275DD05A.001(II) | Trina Solar TSM-275DD05A.002(II) | Trina Solar TSM-275DD05A.00M(II) | Trina Solar TSM-275DD05A.00S(II) | Trina Solar TSM-275DD05A.00U(II) | Trina Solar TSM-275DD05A.05(II) | Trina Solar TSM-275DD05A.051(II) | Trina Solar TSM-275DD05A.052(II) | Trina Solar TSM-275DD05A.05M(II) | Trina Solar TSM-275DD05A.05S(II) | Trina Solar TSM-275DD05A.05U(II) | Trina Solar TSM-275DD05A.08(II) | Trina Solar TSM-275DD05A.081(II) | Trina Solar TSM-275DD05A.082(II) | Trina Solar TSM-275DD05A.08M(II) | Trina Solar TSM-275DD05A.08S(II) | Trina Solar TSM-275DD05A.08U(II) | Trina Solar TSM-275DD05A.10(II) | Trina Solar TSM-275DD05A.15(II) | Trina Solar TSM-275DD05A.18(II) | Trina Solar TSM-275DE05A(II) | Trina Solar TSM-275DE05A.08(II) | Trina Solar TSM-275DEG5(II) | Trina Solar TSM-275DEG5.07(II) | Trina Solar TSM-275DEG5.40(II) | Trina Solar TSM-275DEG5.47(II) | Trina Solar TSM-275PA14 | Trina Solar TSM-275PA14.05 | Trina Solar TSM-275PA14.08 | Trina Solar TSM-275PA14.0x2 | Trina Solar TSM-275PA14.10 | Trina Solar TSM-275PA14.18 | Trina Solar TSM-275PA14.20 | Trina Solar TSM-275PA14.28 | Trina Solar TSM-275PD05 | Trina Solar TSM-275PD05.001 | Trina Solar TSM-275PD05.002 | Trina Solar TSM-275PD05.00C | Trina Solar TSM-275PD05.00D | Trina Solar TSM-275PD05.00M | Trina Solar TSM-275PD05.00S | Trina Solar TSM-275PD05.00U | Trina Solar TSM-275PD05.05 | Trina Solar TSM-275PD05.051 | Trina Solar TSM-275PD05.052 | Trina Solar TSM-275PD05.05C | Trina Solar TSM-275PD05.05D | Trina Solar TSM-275PD05.05M | Trina Solar TSM-275PD05.05S | Trina Solar TSM-275PD05.05U | Trina Solar TSM-275PD05.08 | Trina Solar TSM-275PD05.081 | Trina Solar TSM-275PD05.082 | Trina Solar TSM-275PD05.08C | Trina Solar TSM-275PD05.08D | Trina Solar TSM-275PD05.08M | Trina Solar TSM-275PD05.08S | Trina Solar TSM-275PD05.08U | Trina Solar TSM-275PD05.10 | Trina Solar TSM-275PD05.10C | Trina Solar TSM-275PD05.10D | Trina Solar TSM-275PD05.15 | Trina Solar TSM-275PD05.15C | Trina Solar TSM-275PD05.15D | Trina Solar TSM-275PD05.18 | Trina Solar TSM-275PD05.18C | Trina Solar TSM-275PD05.18D | Trina Solar TSM-275PD14 | Trina Solar TSM-275PD14.08 | Trina Solar TSM-275PD14.0x2 | Trina Solar TSM-275PD14.10 | Trina Solar TSM-275PD14.18 | Trina Solar TSM-275PE05A | Trina Solar TSM-275PE05A.08 | Trina Solar TSM-275PEG5 | Trina Solar TSM-275PEG5.07 | Trina Solar TSM-275PEG5.40 | Trina Solar TSM-275PEG5.47 | Trina Solar TSM-280DD05A(II) | Trina Solar TSM-280DD05A.001(II) | Trina Solar TSM-280DD05A.002(II) | Trina Solar TSM-280DD05A.00M(II) | Trina Solar TSM-280DD05A.00S(II) | Trina Solar TSM-280DD05A.00U(II) | Trina Solar TSM-280DD05A.05(II) | Trina Solar TSM-280DD05A.051(II) | Trina Solar TSM-280DD05A.052(II) | Trina Solar TSM-280DD05A.05M(II) | Trina Solar TSM-280DD05A.05S(II) | Trina Solar TSM-280DD05A.05U(II) | Trina Solar TSM-280DD05A.08(II) | Trina Solar TSM-280DD05A.081(II) | Trina Solar TSM-280DD05A.082(II) | Trina Solar TSM-280DD05A.08M(II) | Trina Solar TSM-280DD05A.08S(II) | Trina Solar TSM-280DD05A.08U(II) | Trina Solar TSM-280DD05A.10(II) | Trina Solar TSM-280DD05A.15(II) | Trina Solar TSM-280DD05A.18(II) | Trina Solar TSM-280DE05A(II) | Trina Solar TSM-280DE05A.08(II) | Trina Solar TSM-280DEG5(II) | Trina Solar TSM-280DEG5.07(II) | Trina Solar TSM-280DEG5.40(II) | Trina Solar TSM-280DEG5.47(II) | Trina Solar TSM-280PA14 | Trina Solar TSM-280PA14.05 | Trina Solar TSM-280PA14.08 | Trina Solar TSM-280PA14.0x2 | Trina Solar TSM-280PA14.10 | Trina Solar TSM-280PA14.18 | Trina Solar TSM-280PA14.20 | Trina Solar TSM-280PA14.28 | Trina Solar TSM-280PD05.05 | Trina Solar TSM-280PD05.08 | Trina Solar TSM-280PD14 | Trina Solar TSM-280PD14.08 | Trina Solar TSM-280PD14.0x2 | Trina Solar TSM-280PD14.10 | Trina Solar TSM-280PD14.18 | Trina Solar TSM-285DD05A(II) | Trina Solar TSM-285DD05A.001(II) | Trina Solar TSM-285DD05A.002(II) | Trina Solar TSM-285DD05A.00M(II) | Trina Solar TSM-285DD05A.00S(II) | Trina Solar TSM-285DD05A.00U(II) | Trina Solar TSM-285DD05A.05(II) | Trina Solar TSM-285DD05A.051(II) | Trina Solar TSM-285DD05A.052(II) | Trina Solar TSM-285DD05A.05M(II) | Trina Solar TSM-285DD05A.05S(II) | Trina Solar TSM-285DD05A.05U(II) | Trina Solar TSM-285DD05A.08(II) | Trina Solar TSM-285DD05A.081(II) | Trina Solar TSM-285DD05A.082(II) | Trina Solar TSM-285DD05A.08M(II) | Trina Solar TSM-285DD05A.08S(II) | Trina Solar TSM-285DD05A.08U(II) | Trina Solar TSM-285DD05A.10(II) | Trina Solar TSM-285DD05A.15(II) | Trina Solar TSM-285DD05A.18(II) | Trina Solar TSM-285DE05A(II) | Trina Solar TSM-285DE05A.08(II) | Trina Solar TSM-285DEG5(II) | Trina Solar TSM-285DEG5.07(II) | Trina Solar TSM-285DEG5.40(II) | Trina Solar TSM-285DEG5.47(II) | Trina Solar TSM-285PA14 | Trina Solar TSM-285PA14.05 | Trina Solar TSM-285PA14.08 | Trina Solar TSM-285PA14.0x2 | Trina Solar TSM-285PA14.10 | Trina Solar TSM-285PA14.18 | Trina Solar TSM-285PA14.20 | Trina Solar TSM-285PA14.28 | Trina Solar TSM-285PA14A | Trina Solar TSM-285PA14A.08 | Trina Solar TSM-285PD14 | Trina Solar TSM-285PD14.08 | Trina Solar TSM-285PD14.0x2 | Trina Solar TSM-285PD14.10 | Trina Solar TSM-285PD14.18 | Trina Solar TSM-285PxG14 | Trina Solar TSM-290DD05A(II) | Trina Solar TSM-290DD05A.001(II) | Trina Solar TSM-290DD05A.002(II) | Trina Solar TSM-290DD05A.00M(II) | Trina Solar TSM-290DD05A.00S(II) | Trina Solar TSM-290DD05A.00U(II) | Trina Solar TSM-290DD05A.05(II) | Trina Solar TSM-290DD05A.051(II) | Trina Solar TSM-290DD05A.052(II) | Trina Solar TSM-290DD05A.05M(II) | Trina Solar TSM-290DD05A.05S(II) | Trina Solar TSM-290DD05A.05U(II) | Trina Solar TSM-290DD05A.08(II) | Trina Solar TSM-290DD05A.081(II) | Trina Solar TSM-290DD05A.082(II) | Trina Solar TSM-290DD05A.08M(II) | Trina Solar TSM-290DD05A.08S(II) | Trina Solar TSM-290DD05A.08U(II) | Trina Solar TSM-290DD05A.10(II) | Trina Solar TSM-290DD05A.15(II) | Trina Solar TSM-290DD05A.18(II) | Trina Solar TSM-290DE05A(II) | Trina Solar TSM-290DE05A.08(II) | Trina Solar TSM-290DEG5(II) | Trina Solar TSM-290DEG5.07(II) | Trina Solar TSM-290DEG5.40(II) | Trina Solar TSM-290DEG5.47(II) | Trina Solar TSM-290DEG5C.07(II) | Trina Solar TSM-290PA14 | Trina Solar TSM-290PA14.08 | Trina Solar TSM-290PA14.0x2 | Trina Solar TSM-290PA14.10 | Trina Solar TSM-290PA14.18 | Trina Solar TSM-290PA14.20 | Trina Solar TSM-290PA14.28 | Trina Solar TSM-290PA14A | Trina Solar TSM-290PA14A.08 | Trina Solar TSM-290PD14 | Trina Solar TSM-290PD14.08 | Trina Solar TSM-290PD14.0x2 | Trina Solar TSM-290PD14.10 | Trina Solar TSM-290PD14.18 | Trina Solar TSM-290PxG14 | Trina Solar TSM-295DD05A(II) | Trina Solar TSM-295DD05A.001(II) | Trina Solar TSM-295DD05A.002(II) | Trina Solar TSM-295DD05A.00M(II) | Trina Solar TSM-295DD05A.00S(II) | Trina Solar TSM-295DD05A.00U(II) | Trina Solar TSM-295DD05A.05(II) | Trina Solar TSM-295DD05A.051(II) | Trina Solar TSM-295DD05A.05M(II) | Trina Solar TSM-295DD05A.05S(II) | Trina Solar TSM-295DD05A.05U(II) | Trina Solar TSM-295DD05A.08(II) | Trina Solar TSM-295DD05A.08M(II) | Trina Solar TSM-295DD05A.08S(II) | Trina Solar TSM-295DD05A.08U(II) | Trina Solar TSM-295DD05A.10(II) | Trina Solar TSM-295DD05A.15(II) | Trina Solar TSM-295DD05A.18(II) | Trina Solar TSM-295DE05A(II) | Trina Solar TSM-295DE05A.08(II) | Trina Solar TSM-295DEG5(II) | Trina Solar TSM-295DEG5.07(II) | Trina Solar TSM-295DEG5.40(II) | Trina Solar TSM-295DEG5.47(II) | Trina Solar TSM-295DEG5C.07(II) | Trina Solar TSM-295PA14 | Trina Solar TSM-295PA14.08 | Trina Solar TSM-295PA14.0x2 | Trina Solar TSM-295PA14.10 | Trina Solar TSM-295PA14.18 | Trina Solar TSM-295PA14.20 | Trina Solar TSM-295PA14.28 | Trina Solar TSM-295PA14A | Trina Solar TSM-295PA14A.08 | Trina Solar TSM-295PD14 | Trina Solar TSM-295PD14.08 | Trina Solar TSM-295PD14.0x2 | Trina Solar TSM-295PD14.10 | Trina Solar TSM-295PD14.18 | Trina Solar TSM-295PxG14 | Trina Solar TSM-300DD05A(II) | Trina Solar TSM-300DD05A.001(II) | Trina Solar TSM-300DD05A.002(II) | Trina Solar TSM-300DD05A.00M(II) | Trina Solar TSM-300DD05A.00S(II) | Trina Solar TSM-300DD05A.00U(II) | Trina Solar TSM-300DD05A.05(II) | Trina Solar TSM-300DD05A.051(II) | Trina Solar TSM-300DD05A.052(II) | Trina Solar TSM-300DD05A.05M(II) | Trina Solar TSM-300DD05A.05S(II) | Trina Solar TSM-300DD05A.05U(II) | Trina Solar TSM-300DD05A.08(II) | Trina Solar TSM-300DD05A.081(II) | Trina Solar TSM-300DD05A.082(II) | Trina Solar TSM-300DD05A.08M(II) | Trina Solar TSM-300DD05A.08S(II) | Trina Solar TSM-300DD05A.08U(II) | Trina Solar TSM-300DD05A.10(II) | Trina Solar TSM-300DD05A.15(II) | Trina Solar TSM-300DD05A.18(II) | Trina Solar TSM-300DE05A(II) | Trina Solar TSM-300DE05A.08(II) | Trina Solar TSM-300DEG5(II) | Trina Solar TSM-300DEG5.07(II) | Trina Solar TSM-300DEG5.40(II) | Trina Solar TSM-300DEG5.47(II) | Trina Solar TSM-300DEG5C.07(II) | Trina Solar TSM-300PA14 | Trina Solar TSM-300PA14.08 | Trina Solar TSM-300PA14.0x2 | Trina Solar TSM-300PA14.10 | Trina Solar TSM-300PA14.18 | Trina Solar TSM-300PA14.20 | Trina Solar TSM-300PA14.28 | Trina Solar TSM-300PA14A | Trina Solar TSM-300PA14A.08 | Trina Solar TSM-300PD14 | Trina Solar TSM-300PD14.08 | Trina Solar TSM-300PD14.0x2 | Trina Solar TSM-300PD14.10 | Trina Solar TSM-300PD14.18 | Trina Solar TSM-300PDG14 | Trina Solar TSM-300PE14A | Trina Solar TSM-300PE14A.08 | Trina Solar TSM-300PEG14 | Trina Solar TSM-300PxG14 | Trina Solar TSM-305DD05A.05(II) | Trina Solar TSM-305DD05A.05S(II) | Trina Solar TSM-305DD05A.15(II) | Trina Solar TSM-305DD05A.18(II) | Trina Solar TSM-305DEG5(II) | Trina Solar TSM-305DEG5.07(II) | Trina Solar TSM-305DEG5.40(II) | Trina Solar TSM-305DEG5.47(II) | Trina Solar TSM-305DEG5C.07(II) | Trina Solar TSM-305PA14 | Trina Solar TSM-305PA14.08 | Trina Solar TSM-305PA14.0x2 | Trina Solar TSM-305PA14.10 | Trina Solar TSM-305PA14.18 | Trina Solar TSM-305PA14.20 | Trina Solar TSM-305PA14.28 | Trina Solar TSM-305PA14A | Trina Solar TSM-305PA14A.08 | Trina Solar TSM-305PD14 | Trina Solar TSM-305PD14.08 | Trina Solar TSM-305PD14.0x2 | Trina Solar TSM-305PD14.10 | Trina Solar TSM-305PD14.18 | Trina Solar TSM-305PDG14 | Trina Solar TSM-305PE14A | Trina Solar TSM-305PE14A.08 | Trina Solar TSM-305PEG14 | Trina Solar TSM-305PxG14 | Trina Solar TSM-310DEG5C.07(II) | Trina Solar TSM-310PA14 | Trina Solar TSM-310PA14.08 | Trina Solar TSM-310PA14.0x2 | Trina Solar TSM-310PA14.10 | Trina Solar TSM-310PA14.18 | Trina Solar TSM-310PA14.20 | Trina Solar TSM-310PA14.28 | Trina Solar TSM-310PA14A | Trina Solar TSM-310PA14A.08 | Trina Solar TSM-310PD14 | Trina Solar TSM-310PD14.08 | Trina Solar TSM-310PD14.0x2 | Trina Solar TSM-310PD14.10 | Trina Solar TSM-310PD14.18 | Trina Solar TSM-310PDG14 | Trina Solar TSM-310PE14A | Trina Solar TSM-310PE14A.08 | Trina Solar TSM-310PEG14 | Trina Solar TSM-310PxG14 | Trina Solar TSM-315DD14A(II) | Trina Solar TSM-315DD14A.05(II) | Trina Solar TSM-315DD14A.08(II) | Trina Solar TSM-315PA14A | Trina Solar TSM-315PA14A.08 | Trina Solar TSM-315PD14 | Trina Solar TSM-315PD14.002 | Trina Solar TSM-315PD14.08 | Trina Solar TSM-315PD14.082 | Trina Solar TSM-315PD14.10 | Trina Solar TSM-315PD14.102 | Trina Solar TSM-315PD14.18 | Trina Solar TSM-315PD14.182 | Trina Solar TSM-315PDG14 | Trina Solar TSM-315PE14A | Trina Solar TSM-315PE14A.08 | Trina Solar TSM-315PEG14 | Trina Solar TSM-320DD14A | Trina Solar TSM-320DD14A(II) | Trina Solar TSM-320DD14A.05 | Trina Solar TSM-320DD14A.05(II) | Trina Solar TSM-320DD14A.08 | Trina Solar TSM-320DD14A.08(II) | Trina Solar TSM-320PD14 | Trina Solar TSM-320PD14.001 | Trina Solar TSM-320PD14.002 | Trina Solar TSM-320PD14.00C | Trina Solar TSM-320PD14.00M | Trina Solar TSM-320PD14.00S | Trina Solar TSM-320PD14.00U | Trina Solar TSM-320PD14.05 | Trina Solar TSM-320PD14.051 | Trina Solar TSM-320PD14.052 | Trina Solar TSM-320PD14.05C | Trina Solar TSM-320PD14.05M | Trina Solar TSM-320PD14.05S | Trina Solar TSM-320PD14.05U | Trina Solar TSM-320PD14.08 | Trina Solar TSM-320PD14.081 | Trina Solar TSM-320PD14.08C | Trina Solar TSM-320PD14.08M | Trina Solar TSM-320PD14.08S | Trina Solar TSM-320PD14.08U | Trina Solar TSM-320PD14.10 | Trina Solar TSM-320PD14.10C | Trina Solar TSM-320PD14.15 | Trina Solar TSM-320PD14.15C | Trina Solar TSM-320PD14.18 | Trina Solar TSM-320PD14.18C | Trina Solar TSM-320PD14.50 | Trina Solar TSM-320PDG14 | Trina Solar TSM-320PE14A | Trina Solar TSM-320PE14A.05 | Trina Solar TSM-320PE14A.08 | Trina Solar TSM-320PE14A.10 | Trina Solar TSM-320PE14A.18 | Trina Solar TSM-320PE14A.50 | Trina Solar TSM-320PEG14 | Trina Solar TSM-320PEG14.07 | Trina Solar TSM-320PEG14.40 | Trina Solar TSM-320PEG14.47 | Trina Solar TSM-325DD14A | Trina Solar TSM-325DD14A(II) | Trina Solar TSM-325DD14A.05 | Trina Solar TSM-325DD14A.05(II) | Trina Solar TSM-325DD14A.08 | Trina Solar TSM-325DD14A.08(II) | Trina Solar TSM-325PD14 | Trina Solar TSM-325PD14.001 | Trina Solar TSM-325PD14.002 | Trina Solar TSM-325PD14.00C | Trina Solar TSM-325PD14.00M | Trina Solar TSM-325PD14.00S | Trina Solar TSM-325PD14.00U | Trina Solar TSM-325PD14.05 | Trina Solar TSM-325PD14.051 | Trina Solar TSM-325PD14.052 | Trina Solar TSM-325PD14.05C | Trina Solar TSM-325PD14.05M | Trina Solar TSM-325PD14.05S | Trina Solar TSM-325PD14.05U | Trina Solar TSM-325PD14.08 | Trina Solar TSM-325PD14.081 | Trina Solar TSM-325PD14.08C | Trina Solar TSM-325PD14.08M | Trina Solar TSM-325PD14.08S | Trina Solar TSM-325PD14.08U | Trina Solar TSM-325PD14.10 | Trina Solar TSM-325PD14.10C | Trina Solar TSM-325PD14.15 | Trina Solar TSM-325PD14.15C | Trina Solar TSM-325PD14.18 | Trina Solar TSM-325PD14.18C | Trina Solar TSM-325PD14.50 | Trina Solar TSM-325PE14A | Trina Solar TSM-325PE14A.05 | Trina Solar TSM-325PE14A.08 | Trina Solar TSM-325PE14A.10 | Trina Solar TSM-325PE14A.15 | Trina Solar TSM-325PE14A.18 | Trina Solar TSM-325PE14A.50 | Trina Solar TSM-325PEG14 | Trina Solar TSM-325PEG14.07 | Trina Solar TSM-325PEG14.40 | Trina Solar TSM-325PEG14.47 | Trina Solar TSM-330DD14A | Trina Solar TSM-330DD14A(II) | Trina Solar TSM-330DD14A.05 | Trina Solar TSM-330DD14A.05(II) | Trina Solar TSM-330DD14A.08 | Trina Solar TSM-330DD14A.08(II) | Trina Solar TSM-330DD14A.10(II) | Trina Solar TSM-330DD14A.15(II) | Trina Solar TSM-330DD14A.18(II) | Trina Solar TSM-330DE14A(II) | Trina Solar TSM-330DE14A.08(II) | Trina Solar TSM-330PD14 | Trina Solar TSM-330PD14.001 | Trina Solar TSM-330PD14.002 | Trina Solar TSM-330PD14.00M | Trina Solar TSM-330PD14.00S | Trina Solar TSM-330PD14.00U | Trina Solar TSM-330PD14.05 | Trina Solar TSM-330PD14.051 | Trina Solar TSM-330PD14.052 | Trina Solar TSM-330PD14.05M | Trina Solar TSM-330PD14.05S | Trina Solar TSM-330PD14.05U | Trina Solar TSM-330PD14.08 | Trina Solar TSM-330PD14.081 | Trina Solar TSM-330PD14.08M | Trina Solar TSM-330PD14.08S | Trina Solar TSM-330PD14.08U | Trina Solar TSM-330PD14.10 | Trina Solar TSM-330PD14.15 | Trina Solar TSM-330PD14.18 | Trina Solar TSM-330PD14.50 | Trina Solar TSM-330PE14A | Trina Solar TSM-330PE14A.05 | Trina Solar TSM-330PE14A.08 | Trina Solar TSM-330PE14A.10 | Trina Solar TSM-330PE14A.15 | Trina Solar TSM-330PE14A.18 | Trina Solar TSM-330PE14A.50 | Trina Solar TSM-330PEG14 | Trina Solar TSM-330PEG14.07 | Trina Solar TSM-330PEG14.40 | Trina Solar TSM-330PEG14.47 | Trina Solar TSM-335DD14A(II) | Trina Solar TSM-335DD14A.05(II) | Trina Solar TSM-335DD14A.08(II) | Trina Solar TSM-335DD14A.10(II) | Trina Solar TSM-335DD14A.15(II) | Trina Solar TSM-335DD14A.18(II) | Trina Solar TSM-335DE14A(II) | Trina Solar TSM-335DE14A.08(II) | Trina Solar TSM-335PD14 | Trina Solar TSM-335PD14.10 | Trina Solar TSM-335PE14A | Trina Solar TSM-335PEG14 | Trina Solar TSM-335PEG14.40 | Trina Solar TSM-340DD14A(II) | Trina Solar TSM-340DD14A.05(II) | Trina Solar TSM-340DD14A.08(II) | Trina Solar TSM-340DD14A.10(II) | Trina Solar TSM-340DD14A.15(II) | Trina Solar TSM-340DD14A.18(II) | Trina Solar TSM-340DE14A(II) | Trina Solar TSM-340DE14A.08(II) | Trina Solar TSM-340DEG14(II) | Trina Solar TSM-340DEG14.07(II) | Trina Solar TSM-340DEG14.40(II) | Trina Solar TSM-340DEG14.47(II) | Trina Solar TSM-340PE14A | Trina Solar TSM-345DD14A(II) | Trina Solar TSM-345DD14A.05(II) | Trina Solar TSM-345DD14A.08(II) | Trina Solar TSM-345DD14A.10(II) | Trina Solar TSM-345DD14A.15(II) | Trina Solar TSM-345DD14A.18(II) | Trina Solar TSM-345DE14A(II) | Trina Solar TSM-345DE14A.08(II) | Trina Solar TSM-345DEG14(II) | Trina Solar TSM-345DEG14.07(II) | Trina Solar TSM-345DEG14.40(II) | Trina Solar TSM-345DEG14.47(II) | Trina Solar TSM-345DEG14C.07(II) | Trina Solar TSM-350DD14A(II) | Trina Solar TSM-350DD14A.05(II) | Trina Solar TSM-350DD14A.08(II) | Trina Solar TSM-350DD14A.10(II) | Trina Solar TSM-350DD14A.15(II) | Trina Solar TSM-350DD14A.18(II) | Trina Solar TSM-350DE14A(II) | Trina Solar TSM-350DE14A.08(II) | Trina Solar TSM-350DEG14(II) | Trina Solar TSM-350DEG14.07(II) | Trina Solar TSM-350DEG14.40(II) | Trina Solar TSM-350DEG14.47(II) | Trina Solar TSM-350DEG14C.07(II) | Trina Solar TSM-355DD14A(II) | Trina Solar TSM-355DD14A.05(II) | Trina Solar TSM-355DD14A.08(II) | Trina Solar TSM-355DD14A.10(II) | Trina Solar TSM-355DD14A.15(II) | Trina Solar TSM-355DD14A.18(II) | Trina Solar TSM-355DE14A(II) | Trina Solar TSM-355DE14A.08(II) | Trina Solar TSM-355DEG14(II) | Trina Solar TSM-355DEG14.07(II) | Trina Solar TSM-355DEG14.40(II) | Trina Solar TSM-355DEG14.47(II) | Trina Solar TSM-355DEG14C.07(II) | Trina Solar TSM-360DD14A(II) | Trina Solar TSM-360DD14A.05(II) | Trina Solar TSM-360DD14A.08(II) | Trina Solar TSM-360DD14A.10(II) | Trina Solar TSM-360DD14A.15(II) | Trina Solar TSM-360DD14A.18(II) | Trina Solar TSM-360DE14A(II) | Trina Solar TSM-360DE14A.08(II) | Trina Solar TSM-360DEG14(II) | Trina Solar TSM-360DEG14.40(II) | Trina Solar TSM-360DEG14C.07(II) | Trina Solar TSM-365DD14A(II) | Trina Solar TSM-365DD14A.10(II) | Trina Solar TSM-365DE14A(II) | Trina Solar TSM-365DEG14(II) | Trina Solar TSM-365DEG14.40(II) | Trina Solar TSM-365DEG14C.07(II) | TSEC TS36-6P2-130 | TSEC TS36-6P3-130A | TSEC TS36-6M2-135 | TSEC TS36-6M3-135A | TSEC TS36-6P2-135 | TSEC TS36-6P3-135A | TSEC TS36-6M2-140 | TSEC TS36-6M3-140A | TSEC TS36-6P2-140 | TSEC TS36-6P3-140A | TSEC TS36-6M2-145 | TSEC TS36-6M3-145A | TSEC TS48-6P2-175 | TSEC TS48-6P3-175A | TSEC TS48-6M2-180 | TSEC TS48-6M3-180A | TSEC TS48-6P2-180 | TSEC TS48-6P3-180A | TSEC TS48-6M2-185 | TSEC TS48-6M3-185A | TSEC TS48-6P2-185 | TSEC TS48-6P3-185A | TSEC TS48-6M2-190 | TSEC TS48-6M3-190A | TSEC TS54-6P2-190 | TSEC TS54-6M2-195 | TSEC TS54-6M3-195D | TSEC TS54-6P2-195 | TSEC TS54-6P3-195A | TSEC TS54-6M2-200 | TSEC TS54-6M3-200D | TSEC TS54-6P2-200 | TSEC TS54-6P3-200A | TSEC TS54-6M2-205 | TSEC TS54-6M3-205D | TSEC TS54-6P2-205 | TSEC TS54-6P3-205A | TSEC TS54-6M2-210 | TSEC TS54-6M3-210D | TSEC TS54-6P2-210 | TSEC TS54-6P3-210A | TSEC TS54-6M2-215 | TSEC TS54-6M3-215D | TSEC TS54-6P2-215 | TSEC TS54-6P3-215A | TSEC TS54-6M2-220 | TSEC TS54-6M3-220A | TSEC TS54-6P3-220A | TSEC TS60-6P2-220 | TSEC TS54-6M3-225A | TSEC TS54-6P3-225A | TSEC TS60-6M2-225 | TSEC TS60-6P2-225 | TSEC TS54-6M3-230A | TSEC TS60-6M2-230 | TSEC TS60-6P2-230 | TSEC TS60-6M2-235 | TSEC TS60-6P2-235 | TSEC TS60-6M2-240 | TSEC TS60-6P2-240 | TSEC TS60-6P3-240 | TSEC TS60-6P3-240S | TSEC TS60-6P3-245 | TSEC TS60-6P3-245A | TSEC TS60-6P3-245S | TSEC TS60-6M3-250 | TSEC TS60-6M3-250S | TSEC TS60-6P3-250 | TSEC TS60-6P3-250A | TSEC TS60-6P3-250S | TSEC TS60-6M3-255 | TSEC TS60-6M3-255S | TSEC TS60-6P3-255 | TSEC TS60-6P3-255A | TSEC TS60-6P3-255S | TSEC TS60-6M3-260 | TSEC TS60-6M3-260S | TSEC TS60-6P3-260 | TSEC TS60-6P3-260S | TSEC TS60-6M3-265 | TSEC TS60-6M3-265S | TSEC TS60-6P3-265 | TSEC TS60-6P3-265S | TSEC TS60-6M3-270 | TSEC TS60-6M3-270S | TSEC TS60-6P3-270 | TSEC TS60-6P3-270S | TSEC TS72-6P3-270 | TSEC TS72-6P3-270B | TSEC TS60-6M3-275 | TSEC TS60-6M3-275S | TSEC TS60-6P3-275 | TSEC TS60-6P3-275S | TSEC TS72-6P2-275 | TSEC TS72-6P3-275 | TSEC TS72-6P3-275A | TSEC TS72-6P3-275B | TSEC TS60-6M3-280 | TSEC TS60-6M3-280S | TSEC TS60-6P3-280 | TSEC TS60-6P3-280S | TSEC TS72-6P2-280 | TSEC TS72-6P3-280 | TSEC TS72-6P3-280A | TSEC TS72-6P3-280B | TSEC TS60-6M3-285 | TSEC TS60-6M3-285S | TSEC TS60-6P3-285 | TSEC TS60-6P3-285S | TSEC TS72-6M3-285 | TSEC TS72-6M3-285B | TSEC TS72-6P2-285 | TSEC TS72-6P3-285 | TSEC TS72-6P3-285A | TSEC TS72-6P3-285B | TSEC TS72-6P3-285S | TSEC TS60-6M3-290 | TSEC TS60-6M3-290S | TSEC TS72-6M3-290 | TSEC TS72-6M3-290B | TSEC TS72-6P2-290 | TSEC TS72-6P3-290 | TSEC TS72-6P3-290A | TSEC TS72-6P3-290B | TSEC TS72-6P3-290S | TSEC TS60-6M3-295 | TSEC TS60-6M3-295S | TSEC TS72-6M3-295 | TSEC TS72-6M3-295B | TSEC TS72-6P2-295 | TSEC TS72-6P3-295 | TSEC TS72-6P3-295A | TSEC TS72-6P3-295S | TSEC TS72-6M3-300 | TSEC TS72-6M3-300B | TSEC TS72-6M3-300S | TSEC TS72-6P3-300 | TSEC TS72-6P3-300S | TSEC TS72-6M3-305 | TSEC TS72-6M3-305B | TSEC TS72-6M3-305S | TSEC TS72-6P3-305 | TSEC TS72-6P3-305S | TSEC TS72-6M3-310 | TSEC TS72-6M3-310S | TSEC TS72-6P3-310 | TSEC TS72-6P3-310S | TSEC TS72-6M3-315 | TSEC TS72-6M3-315S | TSEC TS72-6P3-315 | TSEC TS72-6P3-315S | TSEC TS72-6M3-320 | TSEC TS72-6M3-320S | TSEC TS72-6P3-320 | TSEC TS72-6P3-320S | TSEC TS72-6M3-325 | TSEC TS72-6M3-325S | TSEC TS72-6P3-325 | TSEC TS72-6P3-325S | TSEC TS72-6M3-330 | TSEC TS72-6M3-330S | TSEC TS72-6P3-330 | TSEC TS72-6P3-330S | TSEC TS72-6M3-335 | TSEC TS72-6M3-335S | TSEC TS72-6P3-335 | TSEC TS72-6P3-335S | TSEC TS72-6M3-340 | TSEC TS72-6M3-340S | TSEC TS72-6P3-340 | TSEC TS72-6P3-340S | TSEC TS72-6M3-345 | TSEC TS72-6M3-345S | TSEC TS72-6M3-350 | TSEC TS72-6M3-350S | TSEC TS72-6M3-355 | TSEC TS72-6M3-355S | TSEC Corporation TS60-6M3-300 | TSEC Corporation TS60-6M3-305 | TSEC Corporation TS60-6M3-310 | TSEC Corporation TS60-6M3-315 | TSMC Solar TS-110C | TSMC Solar TS-115C | TSMC Solar TS-120C | TSMC Solar TS-125C | TSMC Solar TS-130C | TSMC Solar TS-135C | TSMC Solar TS-135C1 | TSMC Solar TS-135C1HV | TSMC Solar TS-135C2 | TSMC Solar TS-135C2HV | TSMC Solar TS-140C1 | TSMC Solar TS-140C1HV | TSMC Solar TS-140C2 | TSMC Solar TS-140C2HV | TSMC Solar TS-145C1 | TSMC Solar TS-145C1HV | TSMC Solar TS-145C2 | TSMC Solar TS-145C2HV | TSMC Solar TS-150C1 | TSMC Solar TS-150C1HV | TSMC Solar TS-150C2 | TSMC Solar TS-150C2HV | TSMC Solar TS-155C1 | TSMC Solar TS-155C1HV | TSMC Solar TS-155C2 | TSMC Solar TS-155C2HV | TSMC Solar TS-160C1 | TSMC Solar TS-160C1HV | TSMC Solar TS-160C2 | TSMC Solar TS-160C2HV | TSMC Solar TS-165C2 | TSMC Solar TS-165C2HV | TSMC Solar TS-170C2 | TSMC Solar TS-170C2HV | T-Solar Global TS92 | T-Solar Global TS97 | T-Solar Global TS102 | T-Solar Global TS370 | T-Solar Global TS390 | T-Solar Global TS410 | Tynsolar TYNS62409130 | Tynsolar TYNS62606130 | Tynsolar TYNS62409135 | Tynsolar TYNS62606135 | Tynsolar TYNS62409140 | Tynsolar TYNS62606140 | Tynsolar TYNS62409145 | Tynsolar TYNS62606145 | Tynsolar TYNS62607145 | Tynsolar TYNS62409150 | Tynsolar TYNS62606150 | Tynsolar TYNS62607150 | Tynsolar TYNS62409155 | Tynsolar TYNS62606155 | Tynsolar TYNS62607155 | Tynsolar TYNS62607160 | Tynsolar TYNS62608160 | Tynsolar TYN-168P6 | Tynsolar TYNS62607165 | Tynsolar TYNS62608165 | Tynsolar TYN-170S5 | Tynsolar TYNS62607170 | Tynsolar TYNS62608170 | Tynsolar TYN-180P6 | Tynsolar TYN-180S5 | Tynsolar TYNS62607175 | Tynsolar TYNS62608175 | Tynsolar TYNS62607180 | Tynsolar TYNS62608180 | Tynsolar TYNS62608185 | Tynsolar TYN-190P6 | Tynsolar TYNS62608190 | Tynsolar TYN-195P6 | Tynsolar TYNS62608195 | Tynsolar TYNS62609195 | Tynsolar TYN-200P6 | Tynsolar TYNS62608200 | Tynsolar TYNS62609200 | Tynsolar TYN-205P6 | Tynsolar TYNS62608205 | Tynsolar TYNS62609205 | Tynsolar TYN-210P6 | Tynsolar TYNP62610210 | Tynsolar TYNS62608210 | Tynsolar TYNS62609210 | Tynsolar TYN-215P6 | Tynsolar TYNP62610215 | Tynsolar TYNS62609215 | Tynsolar TYN-220P6 | Tynsolar TYNP62610220 | Tynsolar TYNS62609220 | Tynsolar TYN-225P6 | Tynsolar TYNP62610225 | Tynsolar TYNS62609225 | Tynsolar TYNS62610225 | Tynsolar TYN-230P6 | Tynsolar TYNP62610230 | Tynsolar TYNS62609230 | Tynsolar TYNS62610230 | Tynsolar TYN-235P6 | Tynsolar TYNP62610235 | Tynsolar TYNS62609235 | Tynsolar TYNS62610235 | Tynsolar TYN-240P6 | Tynsolar TYNP62610240 | Tynsolar TYNP62611240 | Tynsolar TYNP62611250 | Tynsolar TYNS62610240 | Tynsolar TYN-245P6 | Tynsolar TYNP62610245 | Tynsolar TYNP62611245 | Tynsolar TYNS62610245 | Tynsolar TYN-250P6 | Tynsolar TYNP62610250 | Tynsolar TYNS62610250 | Tynsolar TYNS62611250 | Tynsolar TYN-255P6 | Tynsolar TYNP62610255 | Tynsolar TYNP62611255 | Tynsolar TYNP62612255 | Tynsolar TYNS62610255 | Tynsolar TYNS62611255 | Tynsolar TYN-260P6 | Tynsolar TYNP62611260 | Tynsolar TYNP62612260 | Tynsolar TYNS62610260 | Tynsolar TYNS62611260 | Tynsolar TYN-265P6 | Tynsolar TYNP62611265 | Tynsolar TYNP62612265 | Tynsolar TYNS62611265 | Tynsolar TYNS62612265 | Tynsolar TYN-270P6 | Tynsolar TYNP62611270 | Tynsolar TYNP62612270 | Tynsolar TYNS62611270 | Tynsolar TYNS62612270 | Tynsolar TYN-275P6 | Tynsolar TYNP62611275 | Tynsolar TYNP62612275 | Tynsolar TYNS62611275 | Tynsolar TYNS62612275 | Tynsolar TYN-280P6 | Tynsolar TYNP62611280 | Tynsolar TYNP62612280 | Tynsolar TYNS62611280 | Tynsolar TYNS62612280 | Tynsolar TYN-285P6 | Tynsolar TYNP62612285 | Tynsolar TYNS62611285 | Tynsolar TYNS62612285 | Tynsolar TYNP62612290 | Tynsolar TYNS62612290 | Tynsolar TYNP62612295 | Tynsolar TYNS62612295 | Tynsolar TYNP62612300 | Tynsolar TYNS62612300 | Tynsolar TYNP62612305 | Tynsolar TYNS62612305 | Tynsolar TYNP62612310 | Tynsolar TYNS62612310 | Tynsolar TYNP62612315 | Tynsolar TYNS62612315 | U.S. Solar USS-QCMI2-36-130 | U.S. Solar USS-QCMI2-36-135 | U.S. Solar USS-QCMI2-36-140 | U.S. Solar USS-QCMI2-36-145 | U.S. Solar USS-QCMI2-36-150 | U.S. Solar USS-QCMI2-48-175 | U.S. Solar USS-QCMI2-48-180 | U.S. Solar USS-QCMI2-48-185 | U.S. Solar USS-QCMI2-48-190 | U.S. Solar USS-QCMI2-48-195 | U.S. Solar USS-QCMI2-48-200 | U.S. Solar USS-QCMI2-54-200 | U.S. Solar USS-QCMI2-54-205 | U.S. Solar USS-QCMI2-54-210 | U.S. Solar USS-QCMI2-54-215 | U.S. Solar USS-QCMI2-54-220 | U.S. Solar USS-QCMI2-60-220 | U.S. Solar USS-QCMI2-54-225 | U.S. Solar USS-QCMI2-60-225 | U.S. Solar USS-QCMI3-60-225 | U.S. Solar USS-QCMI2-54-230 | U.S. Solar USS-QCMI2-60-230 | U.S. Solar USS-QCMI3-60-230 | U.S. Solar USS-QCMO3-60-230 | U.S. Solar USS-QCMI2-60-235 | U.S. Solar USS-QCMI3-60-235 | U.S. Solar USS-QCMO3-60-235 | U.S. Solar USS-QCMI2-60-240 | U.S. Solar USS-QCMI3-60-240 | U.S. Solar USS-QCMO3-60-240 | U.S. Solar USS-QCMI2-60-245 | U.S. Solar USS-QCMI3-60-245 | U.S. Solar USS-QCMO3-60-245 | U.S. Solar USS-QCMI2-60-250 | U.S. Solar USS-QCMI3-60-250 | U.S. Solar USS-QCMO3-60-250 | U.S. Solar USS-QCMI2-60-255 | U.S. Solar USS-QCMI3-60-255 | U.S. Solar USS-QCMO3-60-255 | U.S. Solar USS-QCMI3-60-260 | U.S. Solar USS-QCMO3-60-260 | U.S. Solar USS-QCMI2-72-265 | U.S. Solar USS-QCMI3-60-265 | U.S. Solar USS-QCMO3-60-265 | U.S. Solar USS-QCMI2-72-270 | U.S. Solar USS-QCMI3-60-270 | U.S. Solar USS-QCMO3-60-270 | U.S. Solar USS-QCMI2-72-275 | U.S. Solar USS-QCMO3-60-275 | U.S. Solar USS-QCMI2-72-280 | U.S. Solar USS-QCMI3-72-280 | U.S. Solar USS-QCMI2-72-285 | U.S. Solar USS-QCMI3-72-285 | U.S. Solar USS-QCMO3-72-285 | U.S. Solar USS-QCMI2-72-290 | U.S. Solar USS-QCMI3-72-290 | U.S. Solar USS-QCMO3-72-290 | U.S. Solar USS-QCMI2-72-295 | U.S. Solar USS-QCMI3-72-295 | U.S. Solar USS-QCMO3-72-295 | U.S. Solar USS-QCMI2-72-300 | U.S. Solar USS-QCMI3-72-300 | U.S. Solar USS-QCMO3-72-300 | U.S. Solar USS-QCMI2-72-305 | U.S. Solar USS-QCMI3-72-305 | U.S. Solar USS-QCMO3-72-305 | U.S. Solar USS-QCMI3-72-310 | U.S. Solar USS-QCMO3-72-310 | U.S. Solar USS-QCMI3-72-315 | U.S. Solar USS-QCMO3-72-315 | U.S. Solar USS-QCMI3-72-320 | U.S. Solar USS-QCMO3-72-320 | U.S. Solar USS-QCMI3-72-325 | U.S. Solar USS-QCMO3-72-325 | U.S. Solar USS-QCMI3-72-330 | U.S. Solar USS-QCMO3-72-330 | U.S. Solar USS-QCMO3-72-335 | U.S. Yabang Solar Energy CSM-220P | U.S. Yabang Solar Energy CSM-230P | U.S. Yabang Solar Energy CSM-235P | U.S. Yabang Solar Energy CSM-240PA | U.S. Yabang Solar Energy CSM-260P | U.S. Yabang Solar Energy CSM-270P | U.S. Yabang Solar Energy CSM-280P | U.S. Yabang Solar Energy CSM-290D/C | U.S. Yabang Solar Energy CSM-290P | U.S. Yabang Solar Energy CSM 295D/C | U.S. Yabang Solar Energy CSM-295P | U.S. Yabang Solar Energy CSM-300D/C | UE Solar ZHM175 | UE Solar ZHM180 | UE Solar ZHM185 | UE Solar ZHM220P | UE Solar ZHM225P | UE Solar ZHM230P | UE Solar ZHM-60-230P | UE Solar ZHM235P | UE Solar ZHM-60-235P | UE Solar ZHM240P | UE Solar ZHM-60-240P | UE Solar ZHM245P | UE Solar ZHM-60-245P | UE Solar ZHM250P | UE Solar ZHM-60-250P | UE Solar ZHM255P | UE Solar ZHM-60-255P | UE Solar ZHM260P | UE Solar ZHM-60-260P | UE Solar ZHM265P | UE Solar ZHM270P | UE Solar ZHM275P | UE Solar ZHM280P | Unicor Federal Prison Industries PVM220PS-A2P1200 | Unicor Federal Prison Industries PVM220PS-G156200 | Unicor Federal Prison Industries PVM220PS-IM156200 | Unicor Federal Prison Industries PVM220PS-M156200 | Unicor Federal Prison Industries PVM220PS-Q6LTT200 | Unicor Federal Prison Industries PVM220PS-A2P1205 | Unicor Federal Prison Industries PVM220PS-G156205 | Unicor Federal Prison Industries PVM220PS-IM156205 | Unicor Federal Prison Industries PVM220PS-M156205 | Unicor Federal Prison Industries PVM220PS-Q6LTT205 | Unicor Federal Prison Industries PVM220PS-A2P1210 | Unicor Federal Prison Industries PVM220PS-G156210 | Unicor Federal Prison Industries PVM220PS-IM156210 | Unicor Federal Prison Industries PVM220PS-M156210 | Unicor Federal Prison Industries PVM220PS-Q6LTT210 | Unicor Federal Prison Industries PVM220PS-A2P1215 | Unicor Federal Prison Industries PVM220PS-G156215 | Unicor Federal Prison Industries PVM220PS-IM156215 | Unicor Federal Prison Industries PVM220PS-M156215 | Unicor Federal Prison Industries PVM220PS-Q6LTT215 | Unicor Federal Prison Industries PVM220PS-A2P1220 | Unicor Federal Prison Industries PVM220PS-G156220 | Unicor Federal Prison Industries PVM220PS-IM156220 | Unicor Federal Prison Industries PVM220PS-M156220 | Unicor Federal Prison Industries PVM220PS-Q6LTT220 | Unicor Federal Prison Industries PVM220PS-IM156225 | Unicor Federal Prison Industries PVM220PS-M156225 | Unicor Federal Prison Industries PVM220PS-IM156230 | Unicor Federal Prison Industries PVM220PS-M156230 | Unicor Federal Prison Industries PVM220PS-IM156235 | Unicor Federal Prison Industries PVM220PS-M156235 | Unicor Federal Prison Industries PVM220PS-IM156240 | Universal Energy Nanjing Solar Technology UE M180HR | Universal Energy Nanjing Solar Technology UE M185HR | Universal Energy Nanjing Solar Technology UE M190HR | Universal Energy Nanjing Solar Technology UE P220 | Universal Energy Nanjing Solar Technology UE P225 | Universal Energy Nanjing Solar Technology UE P230 | Universal Energy Nanjing Solar Technology UE P235 | Universal Energy Nanjing Solar Technology UE P240 | Universal Hardware UHC-230M6-6100 | Universal Hardware UHC-230P6-6100 | Universal Hardware UHC-240M6-6100 | Universal Hardware UHC-240P6-6100 | Universal Hardware UHC-250M6-6100 | Universal Hardware UHC-250P6-6100 | Upsolar UP-M155M | Upsolar UP-M160M | Upsolar UP-M165M | Upsolar UP-M170M | Upsolar UP-M175M | Upsolar UP-M175M-B | Upsolar UP-Z175M | Upsolar UP-Z175M-B | Upsolar UP-M180M | Upsolar UP-M180P | Upsolar UP-Z180M | Upsolar UP-Z180M-B | Upsolar UP-M185M | Upsolar UP-M185M-B | Upsolar UP-M185P | Upsolar UP-Z185M | Upsolar UP-Z185M-B | Upsolar UP-M190M | Upsolar UP-M190M-B | Upsolar UP-M190MT | Upsolar UP-M190MT-B | Upsolar UP-M190P | Upsolar UP-S190MT | Upsolar UP-S190MT-B | Upsolar UP-Z190M | Upsolar UP-Z190M-B | Upsolar UP-M195M | Upsolar UP-M195M-B | Upsolar UP-M195P | Upsolar UP-Z195M | Upsolar UP-Z195M-B | Upsolar UP-M200P | Upsolar UP-M205P | Upsolar UP-M205P-B | Upsolar UP-M210P | Upsolar UP-M210P-B | Upsolar UP-M210PT | Upsolar UP-M210PT-B | Upsolar UP-M215P | Upsolar UP-M215P-B | Upsolar UP-M220P | Upsolar UP-M220P-B | Upsolar UP-Z220P | Upsolar UP-Z220P-B | Upsolar UP-M225P | Upsolar UP-Z225P | Upsolar UP-Z225P-B | Upsolar UP-M230M | Upsolar UP-M230M-B | Upsolar UP-M230MS | Upsolar UP-M230MS-B | Upsolar UP-M230MT | Upsolar UP-M230MT-B | Upsolar UP-M230P | Upsolar UP-M230P-B | Upsolar UP-M230PS | Upsolar UP-M230PS-B | Upsolar UP-M230PT | Upsolar UP-M230PT-B | Upsolar UP-Z230M | Upsolar UP-Z230M-B | Upsolar UP-Z230MS | Upsolar UP-Z230MS-B | Upsolar UP-Z230MT | Upsolar UP-Z230MT-B | Upsolar UP-Z230P | Upsolar UP-Z230P-B | Upsolar UP-Z230PS | Upsolar UP-Z230PS-B | Upsolar UP-Z230PT | Upsolar UP-Z230PT-B | Upsolar UP-M235M | Upsolar UP-M235M-B | Upsolar UP-M235MS | Upsolar UP-M235MS-B | Upsolar UP-M235MT | Upsolar UP-M235MT-B | Upsolar UP-M235P | Upsolar UP-M235P-B | Upsolar UP-M235PS | Upsolar UP-M235PS-B | Upsolar UP-M235PT | Upsolar UP-M235PT-B | Upsolar UP-Z235M | Upsolar UP-Z235M-B | Upsolar UP-Z235MS | Upsolar UP-Z235MS-B | Upsolar UP-Z235MT | Upsolar UP-Z235MT-B | Upsolar UP-Z235P | Upsolar UP-Z235P-B | Upsolar UP-Z235PS | Upsolar UP-Z235PS-B | Upsolar UP-Z235PT | Upsolar UP-Z235PT-B | Upsolar UP-M240M | Upsolar UP-M240M-B | Upsolar UP-M240MS | Upsolar UP-M240MS-B | Upsolar UP-M240MT | Upsolar UP-M240MT-B | Upsolar UP-M240P | Upsolar UP-M240P-B | Upsolar UP-M240PS | Upsolar UP-M240PS-B | Upsolar UP-M240PT | Upsolar UP-M240PT-B | Upsolar UP-Z240M | Upsolar UP-Z240M-B | Upsolar UP-Z240MS | Upsolar UP-Z240MS-B | Upsolar UP-Z240MT | Upsolar UP-Z240MT-B | Upsolar UP-Z240P | Upsolar UP-Z240PS | Upsolar UP-Z240PS-B | Upsolar UP-Z240PT | Upsolar UP-Z240PT-B | Upsolar UP-M245M | Upsolar UP-M245M-B | Upsolar UP-M245MS | Upsolar UP-M245MS-B | Upsolar UP-M245MT | Upsolar UP-M245MT-B | Upsolar UP-M245P | Upsolar UP-M245P-B | Upsolar UP-M245PS | Upsolar UP-M245PS-B | Upsolar UP-M245PT | Upsolar UP-M245PT-B | Upsolar UP-Z245M | Upsolar UP-Z245M-B | Upsolar UP-Z245MS | Upsolar UP-Z245MS-B | Upsolar UP-Z245MT | Upsolar UP-Z245MT-B | Upsolar UP-Z245P | Upsolar UP-Z245P-B | Upsolar UP-Z245PS | Upsolar UP-Z245PS-B | Upsolar UP-Z245PT | Upsolar UP-Z245PT-B | Upsolar UP-M250M | Upsolar UP-M250M-B | Upsolar UP-M250MS | Upsolar UP-M250MS-B | Upsolar UP-M250MT | Upsolar UP-M250MT-B | Upsolar UP-M250P | Upsolar UP-M250P-B | Upsolar UP-M250PS | Upsolar UP-M250PS-B | Upsolar UP-M250PT | Upsolar UP-M250PT-B | Upsolar UP-Z250M | Upsolar UP-Z250M-B | Upsolar UP-Z250MS | Upsolar UP-Z250MS-B | Upsolar UP-Z250MT | Upsolar UP-Z250MT-B | Upsolar UP-Z250P | Upsolar UP-Z250P-B | Upsolar UP-Z250PS | Upsolar UP-Z250PS-B | Upsolar UP-Z250PT | Upsolar UP-Z250PT-B | Upsolar UP-M255M | Upsolar UP-M255M-B | Upsolar UP-M255MS | Upsolar UP-M255MS-B | Upsolar UP-M255MT | Upsolar UP-M255MT-B | Upsolar UP-M255P | Upsolar UP-M255P-B | Upsolar UP-M255PS | Upsolar UP-M255PS-B | Upsolar UP-M255PT | Upsolar UP-M255PT-B | Upsolar UP-Z255M | Upsolar UP-Z255M-B | Upsolar UP-Z255MS | Upsolar UP-Z255MS-B | Upsolar UP-Z255MT | Upsolar UP-Z255MT-B | Upsolar UP-Z255P | Upsolar UP-Z255P-B | Upsolar UP-Z255PS | Upsolar UP-Z255PS-B | Upsolar UP-Z255PT | Upsolar UP-Z255PT-B | Upsolar UP-M260M | Upsolar UP-M260M-B | Upsolar UP-M260MS | Upsolar UP-M260MS-B | Upsolar UP-M260MT | Upsolar UP-M260MT-B | Upsolar UP-M260P | Upsolar UP-M260P-B | Upsolar UP-M260PS | Upsolar UP-M260PS-B | Upsolar UP-M260PT | Upsolar UP-M260PT-B | Upsolar UP-Z260M | Upsolar UP-Z260M-B | Upsolar UP-Z260MS | Upsolar UP-Z260MS-B | Upsolar UP-Z260MT | Upsolar UP-Z260MT-B | Upsolar UP-Z260P | Upsolar UP-Z260P-B | Upsolar UP-Z260PS | Upsolar UP-Z260PS-B | Upsolar UP-Z260PT | Upsolar UP-Z260PT-B | Upsolar UP-M265M | Upsolar UP-M265M-B | Upsolar UP-M265MS | Upsolar UP-M265MS-B | Upsolar UP-M265MT | Upsolar UP-M265MT-B | Upsolar UP-M265P | Upsolar UP-Z265M | Upsolar UP-Z265M-B | Upsolar UP-Z265MS | Upsolar UP-Z265MS-B | Upsolar UP-Z265MT | Upsolar UP-Z265MT-B | Upsolar UP-M270M | Upsolar UP-M270M-B | Upsolar UP-M270MS | Upsolar UP-M270MS-B | Upsolar UP-M270MT | Upsolar UP-M270MT-B | Upsolar UP-M270P | Upsolar UP-M270P-B | Upsolar UP-Z270M | Upsolar UP-Z270M-B | Upsolar UP-Z270MS | Upsolar UP-Z270MS-B | Upsolar UP-Z270MT | Upsolar UP-Z270MT-B | Upsolar UP-Z270P | Upsolar UP-Z270P-B | Upsolar UP-M275M | Upsolar UP-M275M-B | Upsolar UP-M275P | Upsolar UP-M275P-B | Upsolar UP-Z275P | Upsolar UP-Z275P-B | Upsolar UP-M280M | Upsolar UP-M280P | Upsolar UP-M280P-B | Upsolar UP-M280PS | Upsolar UP-M280PT | Upsolar UP-M280PT-B | Upsolar UP-Z280P | Upsolar UP-Z280P-B | Upsolar UP-M285M | Upsolar UP-M285P | Upsolar UP-M285PS | Upsolar UP-M285PT | Upsolar UP-Z285P | Upsolar UP-M290M | Upsolar UP-M290P | Upsolar UP-M290PS | Upsolar UP-M290PT | Upsolar UP-Z290P | Upsolar UP-M295M | Upsolar UP-M295P | Upsolar UP-M295PS | Upsolar UP-M295PT | Upsolar UP-Z295P | Upsolar UP-M300M | Upsolar UP-M300MS | Upsolar UP-M300P | Upsolar UP-M300PS | Upsolar UP-M300PT | Upsolar UP-Z300P | Upsolar UP-M305M | Upsolar UP-M305MS | Upsolar UP-M305P | Upsolar UP-M305PS | Upsolar UP-M305PT | Upsolar UP-M310M | Upsolar UP-M310MS | Upsolar UP-M310P | Upsolar UP-M310PS | Upsolar UP-M310PT | Upsolar UP-M315M | Upsolar UP-M315MS | Upsolar UP-M315P | Upsolar UP-M315PS | Upsolar UP-M315PT | Upsolar UP-M320M | Upsolar UP-M320MS | Upsolar UP-M320P | Upsolar UP-M325M | Upsolar UP-M325MS | Upsolar UP-M325P | Upsolar UP-M330P | Upsolar UP-M350M | Upsolar UP-M360M | Upsolar UP-M365M | US Topco Energy TOPCO-170S5 | US Topco Energy TOPCO-180P6 | US Topco Energy TOPCO-180S5 | US Topco Energy TOPCO-190P6 | US Topco Energy TOPCO-195P6 | US Topco Energy TOPCO-200P6 | US Topco Energy TOPCO-205P6 | US Topco Energy TOPCO-210P6 | US Topco Energy TOPCO-215P6 | US Topco Energy TOPCO-220P6 | US Topco Energy TOPCO-225P6 | US Topco Energy TOPCO-230P6 | US Topco Energy TOPCO-235P6 | US Topco Energy TOPCO-240P6 | US Topco Energy TOPCO-245P6 | US Topco Energy TOPCO-250P6 | US Topco Energy TOPCO-255P6 | US Topco Energy TOPCO-260P6 | US Topco Energy TOPCO-265P6 | US Topco Energy TOPCO-270P6 | US Topco Energy TOPCO-275P6 | US Topco Energy TOPCO-280P6 | US Topco Energy TOPCO-285P6 | USOL Energy USOL-245-60P | USOL Energy USOL-250-60P | USOL Energy USOL-255-60P | USOL Energy USOL-260-60P | USOL Energy USOL-265-60P | Vikram Solar Eldora VSP.60.240.03 | Vikram Solar Eldora VSP.60.245.03 | Vikram Solar Eldora VSPB.60.245.03 | Vikram Solar Eldora VSP.60.250.03 | Vikram Solar Eldora VSPB.60.250.03 | Vikram Solar Eldora VSP.60.255.03 | Vikram Solar ELDORA VSP.60.255.03.04 | Vikram Solar ELDORA VSP.60.255.05 | Vikram Solar Eldora VSPB.60.255.03 | Vikram Solar Eldora VSP.60.260.03 | Vikram Solar ELDORA VSP.60.260.03.04 | Vikram Solar ELDORA VSP.60.260.05 | Vikram Solar Eldora VSPB.60.260.03 | Vikram Solar Eldora VSP.60.265.03 | Vikram Solar ELDORA VSP.60.265.03.04 | Vikram Solar ELDORA VSP.60.265.05 | Vikram Solar Eldora VSPB.60.265.03 | Vikram Solar ELDORA 270 | Vikram Solar Eldora VSP.60.270.03 | Vikram Solar ELDORA VSP.60.270.03.04 | Vikram Solar ELDORA VSP.60.270.05 | Vikram Solar SOMERA VSM.60.270.05 | Vikram Solar ELDORA VSP.60.275.03.04 | Vikram Solar ELDORA VSP.60.275.05 | Vikram Solar SOMERA VSM.60.275.05 | Vikram Solar ELDORA VSP.60.280.03.04 | Vikram Solar SOMERA VSM.60.280.05 | Vikram Solar SOMERA VSM.60.285.05 | Vikram Solar SOMERA VSM.60.290.05 | Vikram Solar Eldora VSP.72.295.03 | Vikram Solar SOMERA VSM.60.295.05 | Vikram Solar Eldora VSP.72.300.03 | Vikram Solar SOMERA VSM.60.300.05 | Vikram Solar Eldora VSP.72.305.03 | Vikram Solar ELDORA VSP.72.305.05 | Vikram Solar SOMERA VSM.60.305.05 | Vikram Solar Eldora VSP.72.310.03 | Vikram Solar ELDORA VSP.72.310.03.04 | Vikram Solar ELDORA VSP.72.310.05 | Vikram Solar Eldora VSP.72.315.03 | Vikram Solar ELDORA VSP.72.315.03.04 | Vikram Solar ELDORA VSP.72.315.05 | Vikram Solar Eldora VSP.72.320.03 | Vikram Solar ELDORA VSP.72.320.03.04 | Vikram Solar ELDORA VSP.72.320.05 | Vikram Solar Eldora VSP.72.325.03 | Vikram Solar ELDORA VSP.72.325.03.04 | Vikram Solar ELDORA VSP.72.325.05 | Vikram Solar ELDORA VSP.72.330.03.04 | Vikram Solar SOMERA VSM.72.330.05 | Vikram Solar ELDORA VSP.72.335.03.04 | Vikram Solar SOMERA VSM.72.335.05 | Vikram Solar SOMERA VSM.72.340.05 | Vikram Solar SOMERA VSM.72.345.05 | Vikram Solar SOMERA VSM.72.350.05 | Vikram Solar SOMERA VSM.72.355.05 | Vikram Solar SOMERA VSM.72.360.05 | Vikram Solar SOMERA VSM.72.365.05 | VINA SOLAR TECHNOLOGY CO LTD VNS-60M1-5-280W-1.0 | VINA SOLAR TECHNOLOGY CO LTD VNS-60M1-5-280W-1.5 | VINA SOLAR TECHNOLOGY CO LTD VNS-60M1-5-285W-1.0 | VINA SOLAR TECHNOLOGY CO LTD VNS-60M1-5-285W-1.5 | VINA SOLAR TECHNOLOGY CO LTD VNS-60M1-5-290W-1.0 | VINA SOLAR TECHNOLOGY CO LTD VNS-60M1-5-290W-1.5 | VINA SOLAR TECHNOLOGY CO LTD VNS-60M1-5-295W-1.0 | VINA SOLAR TECHNOLOGY CO LTD VNS-60M1-5-295W-1.5 | VINA SOLAR TECHNOLOGY CO LTD VNS-60M1-5-300W-1.0 | VINA SOLAR TECHNOLOGY CO LTD VNS-60M1-5-300W-1.5 | VINA SOLAR TECHNOLOGY CO LTD VNS-72PX-7-320W-1.0 | VINA SOLAR TECHNOLOGY CO LTD VNS-72PX-7-320W-1.5 | VINA SOLAR TECHNOLOGY CO LTD VNS-72PX-7-325W-1.0 | VINA SOLAR TECHNOLOGY CO LTD VNS-72PX-7-325W-1.5 | VINA SOLAR TECHNOLOGY CO LTD VNS-72PX-7-330W-1.0 | VINA SOLAR TECHNOLOGY CO LTD VNS-72PX-7-330W-1.5 | VINA SOLAR TECHNOLOGY CO LTD VNS-72MX-5-335W-1.0 | VINA SOLAR TECHNOLOGY CO LTD VNS-72MX-5-335W-1.5 | VINA SOLAR TECHNOLOGY CO LTD VNS-72PX-7-335W-1.0 | VINA SOLAR TECHNOLOGY CO LTD VNS-72PX-7-335W-1.5 | VINA SOLAR TECHNOLOGY CO LTD VNS-72MX-5-340W-1.0 | VINA SOLAR TECHNOLOGY CO LTD VNS-72MX-5-340W-1.5 | VINA SOLAR TECHNOLOGY CO LTD VNS-72PX-7-340W-1.0 | VINA SOLAR TECHNOLOGY CO LTD VNS-72PX-7-340W-1.5 | VINA SOLAR TECHNOLOGY CO LTD VNS-72MX-5-345W-1.0 | VINA SOLAR TECHNOLOGY CO LTD VNS-72MX-5-345W-1.5 | VINA SOLAR TECHNOLOGY CO LTD VNS-72PX-7-345W-1.0 | VINA SOLAR TECHNOLOGY CO LTD VNS-72PX-7-345W-1.5 | VINA SOLAR TECHNOLOGY CO LTD VNS-72MX-5-350W-1.0 | VINA SOLAR TECHNOLOGY CO LTD VNS-72MX-5-350W-1.5 | VINA SOLAR TECHNOLOGY CO LTD VNS-72MX-5-355W-1.0 | VINA SOLAR TECHNOLOGY CO LTD VNS-72MX-5-355W-1.5 | VINA SOLAR TECHNOLOGY CO LTD VNS-72MX-5-360W-1.0 | VINA SOLAR TECHNOLOGY CO LTD VNS-72MX-5-360W-1.5 | VINA SOLAR TECHNOLOGY CO LTD VNS-72MX-5-365W-1.0 | VINA SOLAR TECHNOLOGY CO LTD VNS-72MX-5-365W-1.5 | Waaree Energies WU-120 | Waaree Energies WU-125 | Waaree Energies WU-130 | Waaree Energies WSM-135 | Waaree Energies WSM-140 | Waaree Energies WU-140 | Waaree Energies WSM-145 | Waaree Energies WU-175 | Waaree Energies WU-180 | Waaree Energies WU-190 | Waaree Energies WU-200 | Waaree Energies WU-210 | Waaree Energies WS-220 | Waaree Energies WU-220 | Waaree Energies WS-225 | Waaree Energies WS-230 | Waaree Energies WU-230 | Waaree Energies WS-235 | Waaree Energies WS-240 | Waaree Energies WU-240 | Waaree Energies WS-255 | Waaree Energies WS-260 | Waaree Energies WS-265 | Waaree Energies WS-270 | Waaree Energies WS-275 | Waaree Energies WSM-275 | Waaree Energies WS-280 | Waaree Energies WSM-280 | Waaree Energies WS-285 | Waaree Energies WSM-285 | Waaree Energies WS-290 | Waaree Energies WSM-290 | Waaree Energies WSM-295 | Waaree Energies WSM-300 | Waaree Energies WSM-305 | Waaree Energies WSM-310 | Waaree Energies WSM-315 | Wanxiang New Energy WXS175S-US | Wanxiang New Energy WXS180P-US | Wanxiang New Energy WXS180S-US | Wanxiang New Energy WXS185P-US | Wanxiang New Energy WXS185S-US | Wanxiang New Energy WXS190P-US | Wanxiang New Energy WXS200P-US | Wanxiang New Energy WXS205P-US | Wanxiang New Energy WXS210P-US | Wanxiang New Energy WXS215P-US | Wanxiang New Energy WXS220P-US | Wanxiang New Energy WXS225P-US | Wanxiang New Energy WXS230P-US | Wanxiang New Energy WXS235P-US | Wanxiang New Energy WXS240P-US | Wanxiang New Energy WXS245P-US | Wanxiang New Energy WXS250P-US | Wanxiang New Energy WXS255P-US | Wanxiang New Energy WXS260P-US | Wanxiang New Energy WXS265P-US | Wanxiang New Energy WXS270P-US | Wanxiang New Energy WXS275P-US | Wanxiang New Energy WXS280P-US | Wanxiang New Energy WXS285P-US | Watton Solar WTM160M | Watton Solar WTM165M | Watton Solar WTM170M | Watton Solar WTM175M | Watton Solar WTM180M | Watton Solar WTM185M | Watton Solar WTM200P | Watton Solar WTM205P | Watton Solar WTM210P | Watton Solar WTM215P | Watton Solar WTM220P | Watton Solar WTM225P | Watton Solar WTM230P | Watton Solar WTM235P | Watton Solar WTM240P | Webel SL Energy Systems W 1750-170 Wp | Webel SL Energy Systems W 1750-175 Wp | Webel SL Energy Systems W 1750-180 Wp | Webel SL Energy Systems W 2100-210 Wp | Webel SL Energy Systems W 2100-215 Wp | Webel SL Energy Systems W 2100-220 Wp | Webel SL Energy Systems W 2300-230 | Webel SL Energy Systems W 2300-235 Wp | Webel SL Energy Systems W 2300-240 Wp | Websol Energy Systems W2500-250 | Websol Energy Systems W2800-275 | Websol Energy Systems W2800-280 | Websol Energy Systems W2800-285 | Wenzhou Jingri Photovoltaic Technology JRM160M | Wenzhou Jingri Photovoltaic Technology JRM165M | Wenzhou Jingri Photovoltaic Technology JRM170M | Wenzhou Jingri Photovoltaic Technology JRM175M | Wenzhou Jingri Photovoltaic Technology JRM180M | Wenzhou Jingri Photovoltaic Technology JRM185M | Wenzhou Jingri Photovoltaic Technology JRM200P | Wenzhou Jingri Photovoltaic Technology JRM205P | Wenzhou Jingri Photovoltaic Technology JRM210P | Wenzhou Jingri Photovoltaic Technology JRM215P | Wenzhou Jingri Photovoltaic Technology JRM220P | Wenzhou Jingri Photovoltaic Technology JRM225P | Wenzhou Jingri Photovoltaic Technology JRM230P | Wenzhou Jingri Photovoltaic Technology JRM235P | Wenzhou Jingri Photovoltaic Technology JRM240P | Westinghouse Solar ST-165-1 | Westinghouse Solar WS_165_1_DC0_0_B | Westinghouse Solar WS-165-1-DC0-0-A | Westinghouse Solar ST-170-1 | Westinghouse Solar WS_170_1_DC0_0_B | Westinghouse Solar WS-170-1-DC0-0-A | Westinghouse Solar ST-175-1 | Westinghouse Solar WS_175_1_DC0_0_B | Westinghouse Solar WS-175-1AC1-A-A | Westinghouse Solar WS-175-1AC3-B-A | Westinghouse Solar WS-175-1-DC0-0-A | Westinghouse Solar ST-180-1 | Westinghouse Solar WS_180_1_DC0_0_B | Westinghouse Solar WS-180-1-DC0-0-A | Westinghouse Solar ST-185-1 | Westinghouse Solar WS_185_1_DC0_0_A | Westinghouse Solar WS_185_1_DC0_0_B | Westinghouse Solar WS-185-1AC1-A-A | Westinghouse Solar WS-185-1AC1-A-B | Westinghouse Solar WS-185-1AC3-B-A | Westinghouse Solar WS-185-1AC3-B-B | Westinghouse Solar WS_190_1_DC0_0_B | Westinghouse Solar WS-190-1AC1-A-B | Westinghouse Solar WS-190-1AC3-B-B | Westinghouse Solar WS_195_1_DC0_0_B | Westinghouse Solar WS-195-1AC1-A-B | Westinghouse Solar WS-195-1AC3-B-B | Westinghouse Solar WLW-230-1-AC0-D-B | Westinghouse Solar WLW-230-1-AC1-A-B | Westinghouse Solar WLW-230-1-AC2-D-B | Westinghouse Solar WLW-230-1-AC3-B-B | Westinghouse Solar WLW-230-1-DC0-0-B | Westinghouse Solar WLW-230-1-DC0-0-BL | Westinghouse Solar WLW-230-1-DC1-0-B | Westinghouse Solar WLW-235-1-AC0-D-B | Westinghouse Solar WLW-235-1-AC1-A-B | Westinghouse Solar WLW-235-1-AC2-D-B | Westinghouse Solar WLW-235-1-AC3-B-B | Westinghouse Solar WLW-235-1-DC0-0-B | Westinghouse Solar WLW-235-1-DC0-0-BL | Westinghouse Solar WLW-235-1-DC1-0-B | Westinghouse Solar WLW-240-1-AC0-D-B | Westinghouse Solar WLW-240-1-AC1-A-B | Westinghouse Solar WLW-240-1-AC2-D-B | Westinghouse Solar WLW-240-1-AC3-B-B | Westinghouse Solar WLW-240-1-DC0-0-B | Westinghouse Solar WLW-240-1-DC0-0-BL | Westinghouse Solar WLW-240-1-DC1-0-B | Westinghouse Solar WTW-240-1-AC2-D-B | Westinghouse Solar WTW-240-1-DC4-0-B | Westinghouse Solar WTW-245-1-AC2-D-B | Westinghouse Solar WTW-245-1-DC4-0-B | Westinghouse Solar WTW-250-1-AC2-D-B | Westinghouse Solar WTW-250-1-DC4-0-B | Westinghouse Solar WS_260_1_DC0_0_B | Westinghouse Solar WS_270_1_DC0_0_B | Westinghouse Solar WS_280_1_DC0_0_B | Westinghouse Solar WS_290_1_DC0_0_B | WINAICO WSP-230P6 | WINAICO WSP-235P6 | WINAICO WSx-240P6 | WINAICO WSx-245P6 | WINAICO WSx-250P6 | WINAICO WSx-255P6 | WINAICO WSP-260M6 | WINAICO WSx-260P6 | WINAICO WSP-265M6 | WINAICO WSP-265P6 | WINAICO WST-265P6 | WINAICO WSP-270M6 | WINAICO WSP-270P6 | WINAICO WST-270P6 | WINAICO WSP-275M6 | WINAICO WSP-275P6 | WINAICO WST-275P6 | WINAICO WSP-280M6 | WINAICO WSP-280P6 | WINAICO WST-280P6 | WINAICO WSP-285M6 | WINAICO WSP-285P6 | WINAICO WST-285M6 | WINAICO WST-285P6 | WINAICO WSP-290M6 | WINAICO WST-290M6 | WINAICO WSP-295M6 | WINAICO WSP-300M6 | WINAICO WSP-305M6 | WINAICO WSP-310M6 | WINAICO WSP-315M6 | Wuxi Shangpin Solar Energy Science & Technology SPSM-165D | Wuxi Shangpin Solar Energy Science & Technology SPSM-170D | Wuxi Shangpin Solar Energy Science & Technology SPSM-175D | Wuxi Shangpin Solar Energy Science & Technology SPSM-180D | Wuxi Shangpin Solar Energy Science & Technology SPSM-250P | Wuxi Shangpin Solar Energy Science & Technology SPSM-260P | Wuxi Shangpin Solar Energy Science & Technology SPSM-270P | Xian Huanghe Photovoltaic Technology HH180(36)M | Xian Huanghe Photovoltaic Technology HH185(36)M | Xian Huanghe Photovoltaic Technology HH225(30)P | Xian Huanghe Photovoltaic Technology HH230(30)P | Xian Huanghe Photovoltaic Technology HH235(30)P | Xian Huanghe Photovoltaic Technology HH275(36)P | Xian Huanghe Photovoltaic Technology HH280(36)P | Xian Huanghe Photovoltaic Technology HH285(36)P | XL Telecom & Energy XL 30225 | Xunlight XRU10-71 | Xunlight XRU10-74 | Xunlight XR12-88 | Xunlight XRS18-146 | Xunlight XRS18-150 | Xunlight XRS18-158 | Xunlight XR 36-264 | Xunlight XR36-291 | Xunlight XR36-300 | Xunlight XR38-307 | Xunlight XR36-315 | Yes! Solar ES190W-NW | Yes! Solar ES190W-RW | Yes! Solar ES195W-NW | Yes! Solar ES195W-RW | Yes! Solar ES200W-NW | Yes! Solar ES200W-RW | Yes! Solar ES205W-NW | Yes! Solar ES205W-RW | Yingli Energy (China) YL170P-23b | Yingli Energy (China) YL175P-23b | Yingli Energy (China) YL180P-23b | Yingli Energy (China) YL185P-23b | Yingli Energy (China) YL195P-26b | Yingli Energy (China) YL200P-26b | Yingli Energy (China) YL205P-26b | Yingli Energy (China) YL210P-26b | Yingli Energy (China) YL220P-29b | Yingli Energy (China) YL225P-29b | Yingli Energy (China) YL230P-29b | Yingli Energy (China) YL235P-29b | Yingli Energy (China) YL240P-29b | Yingli Energy (China) YL240P-32b | Yingli Energy (China) YL245P-29b | Yingli Energy (China) YL245P-32b | Yingli Energy (China) YL250C-30b | Yingli Energy (China) YL250P-29b | Yingli Energy (China) YL250P-32b | Yingli Energy (China) YL255C-30b | Yingli Energy (China) YL255P-29b | Yingli Energy (China) YL255P-32b | Yingli Energy (China) YL260C-30b | Yingli Energy (China) YL260P-29b | Yingli Energy (China) YL260P-35b | Yingli Energy (China) YL265C-30b | Yingli Energy (China) YL265P-29b | Yingli Energy (China) YL265P-35b | Yingli Energy (China) YL270C-30b | Yingli Energy (China) YL270D-30b | Yingli Energy (China) YL270P-35b | Yingli Energy (China) YL275D-30b | Yingli Energy (China) YL275P-35b | Yingli Energy (China) YL280D-30b | Yingli Energy (China) YL280P-35b | Yingli Energy (China) YL285D-30b | Yingli Energy (China) YL285P-35b | Yingli Energy (China) YL290D-30b | Yingli Energy (China) YL290P-35b | Yingli Energy (China) YL295D-30b | Yingli Energy (China) YL295P-35b | Yingli Energy (China) YL300D-30b | Yingli Energy (China) YL300P-35b | Yingli Energy (China) YL305P-35b | Yingli Energy (China) YL310P-35b | Yingli Energy (China) YL315P-35b | Yingli Energy (China) YL320P-35b | Yingli Energy (China) YL325D-36b | Yingli Energy (China) YL325P-35b | Yingli Energy (China) YL330D-36b | Yingli Energy (China) YL330P-35b | Yingli Energy (China) YL335D-36b | Yingli Energy (China) YL335P-35b | 